simulink model "H175_V3_walk"  (R2025b)
(part 2 of 13)

  ct_L_elbow : nesl_utility/Simulink-PS Converter  PhysicalDomain=network_engine_domain  SubClassName=ps_input  LeftPortType=input  RightPortType=output  PseudoPeriodic=off  Frequencies=[]  NoiseDistribution=none  NoiseParameters=[]  Unit=N*m  AffineConversion=off  FilteringAndDerivatives=provide  SimscapeFilterOrder=1  InputFilterTimeConstant=0.001  UdotUserProvided=0
  ct_L_forearm_twist : nesl_utility/Simulink-PS Converter  PhysicalDomain=network_engine_domain  SubClassName=ps_input  LeftPortType=input  RightPortType=output  PseudoPeriodic=off  Frequencies=[]  NoiseDistribution=none  NoiseParameters=[]  Unit=N*m  AffineConversion=off  FilteringAndDerivatives=provide  SimscapeFilterOrder=1  InputFilterTimeConstant=0.001  UdotUserProvided=0
  ct_L_hip_pitch : nesl_utility/Simulink-PS Converter  PhysicalDomain=network_engine_domain  SubClassName=ps_input  LeftPortType=input  RightPortType=output  PseudoPeriodic=off  Frequencies=[]  NoiseDistribution=none  NoiseParameters=[]  Unit=N*m  AffineConversion=off  FilteringAndDerivatives=provide  SimscapeFilterOrder=1  InputFilterTimeConstant=0.001  UdotUserProvided=0
  ct_L_hip_roll : nesl_utility/Simulink-PS Converter  PhysicalDomain=network_engine_domain  SubClassName=ps_input  LeftPortType=input  RightPortType=output  PseudoPeriodic=off  Frequencies=[]  NoiseDistribution=none  NoiseParameters=[]  Unit=N*m  AffineConversion=off  FilteringAndDerivatives=provide  SimscapeFilterOrder=1  InputFilterTimeConstant=0.001  UdotUserProvided=0
  ct_L_hip_yaw : nesl_utility/Simulink-PS Converter  PhysicalDomain=network_engine_domain  SubClassName=ps_input  LeftPortType=input  RightPortType=output  PseudoPeriodic=off  Frequencies=[]  NoiseDistribution=none  NoiseParameters=[]  Unit=N*m  AffineConversion=off  FilteringAndDerivatives=provide  SimscapeFilterOrder=1  InputFilterTimeConstant=0.001  UdotUserProvided=0
  ct_L_index1 : nesl_utility/Simulink-PS Converter  PhysicalDomain=network_engine_domain  SubClassName=ps_input  LeftPortType=input  RightPortType=output  PseudoPeriodic=off  Frequencies=[]  NoiseDistribution=none  NoiseParameters=[]  Unit=N*m  AffineConversion=off  FilteringAndDerivatives=provide  SimscapeFilterOrder=1  InputFilterTimeConstant=0.001  UdotUserProvided=0
  ct_L_index2 : nesl_utility/Simulink-PS Converter  PhysicalDomain=network_engine_domain  SubClassName=ps_input  LeftPortType=input  RightPortType=output  PseudoPeriodic=off  Frequencies=[]  NoiseDistribution=none  NoiseParameters=[]  Unit=N*m  AffineConversion=off  FilteringAndDerivatives=provide  SimscapeFilterOrder=1  InputFilterTimeConstant=0.001  UdotUserProvided=0
  ct_L_index3 : nesl_utility/Simulink-PS Converter  PhysicalDomain=network_engine_domain  SubClassName=ps_input  LeftPortType=input  RightPortType=output  PseudoPeriodic=off  Frequencies=[]  NoiseDistribution=none  NoiseParameters=[]  Unit=N*m  AffineConversion=off  FilteringAndDerivatives=provide  SimscapeFilterOrder=1  InputFilterTimeConstant=0.001  UdotUserProvided=0
  ct_L_knee : nesl_utility/Simulink-PS Converter  PhysicalDomain=network_engine_domain  SubClassName=ps_input  LeftPortType=input  RightPortType=output  PseudoPeriodic=off  Frequencies=[]  NoiseDistribution=none  NoiseParameters=[]  Unit=N*m  AffineConversion=off  FilteringAndDerivatives=provide  SimscapeFilterOrder=1  InputFilterTimeConstant=0.001  UdotUserProvided=0
  ct_L_little1 : nesl_utility/Simulink-PS Converter  PhysicalDomain=network_engine_domain  SubClassName=ps_input  LeftPortType=input  RightPortType=output  PseudoPeriodic=off  Frequencies=[]  NoiseDistribution=none  NoiseParameters=[]  Unit=N*m  AffineConversion=off  FilteringAndDerivatives=provide  SimscapeFilterOrder=1  InputFilterTimeConstant=0.001  UdotUserProvided=0
  ct_L_little2 : nesl_utility/Simulink-PS Converter  PhysicalDomain=network_engine_domain  SubClassName=ps_input  LeftPortType=input  RightPortType=output  PseudoPeriodic=off  Frequencies=[]  NoiseDistribution=none  NoiseParameters=[]  Unit=N*m  AffineConversion=off  FilteringAndDerivatives=provide  SimscapeFilterOrder=1  InputFilterTimeConstant=0.001  UdotUserProvided=0
  ct_L_little3 : nesl_utility/Simulink-PS Converter  PhysicalDomain=network_engine_domain  SubClassName=ps_input  LeftPortType=input  RightPortType=output  PseudoPeriodic=off  Frequencies=[]  NoiseDistribution=none  NoiseParameters=[]  Unit=N*m  AffineConversion=off  FilteringAndDerivatives=provide  SimscapeFilterOrder=1  InputFilterTimeConstant=0.001  UdotUserProvided=0
  ct_L_middle1 : nesl_utility/Simulink-PS Converter  PhysicalDomain=network_engine_domain  SubClassName=ps_input  LeftPortType=input  RightPortType=output  PseudoPeriodic=off  Frequencies=[]  NoiseDistribution=none  NoiseParameters=[]  Unit=N*m  AffineConversion=off  FilteringAndDerivatives=provide  SimscapeFilterOrder=1  InputFilterTimeConstant=0.001  UdotUserProvided=0
  ct_L_middle2 : nesl_utility/Simulink-PS Converter  PhysicalDomain=network_engine_domain  SubClassName=ps_input  LeftPortType=input  RightPortType=output  PseudoPeriodic=off  Frequencies=[]  NoiseDistribution=none  NoiseParameters=[]  Unit=N*m  AffineConversion=off  FilteringAndDerivatives=provide  SimscapeFilterOrder=1  InputFilterTimeConstant=0.001  UdotUserProvided=0
  ct_L_middle3 : nesl_utility/Simulink-PS Converter  PhysicalDomain=network_engine_domain  SubClassName=ps_input  LeftPortType=input  RightPortType=output  PseudoPeriodic=off  Frequencies=[]  NoiseDistribution=none  NoiseParameters=[]  Unit=N*m  AffineConversion=off  FilteringAndDerivatives=provide  SimscapeFilterOrder=1  InputFilterTimeConstant=0.001  UdotUserProvided=0
  ct_L_ring1 : nesl_utility/Simulink-PS Converter  PhysicalDomain=network_engine_domain  SubClassName=ps_input  LeftPortType=input  RightPortType=output  PseudoPeriodic=off  Frequencies=[]  NoiseDistribution=none  NoiseParameters=[]  Unit=N*m  AffineConversion=off  FilteringAndDerivatives=provide  SimscapeFilterOrder=1  InputFilterTimeConstant=0.001  UdotUserProvided=0
  ct_L_ring2 : nesl_utility/Simulink-PS Converter  PhysicalDomain=network_engine_domain  SubClassName=ps_input  LeftPortType=input  RightPortType=output  PseudoPeriodic=off  Frequencies=[]  NoiseDistribution=none  NoiseParameters=[]  Unit=N*m  AffineConversion=off  FilteringAndDerivatives=provide  SimscapeFilterOrder=1  InputFilterTimeConstant=0.001  UdotUserProvided=0
  ct_L_ring3 : nesl_utility/Simulink-PS Converter  PhysicalDomain=network_engine_domain  SubClassName=ps_input  LeftPortType=input  RightPortType=output  PseudoPeriodic=off  Frequencies=[]  NoiseDistribution=none  NoiseParameters=[]  Unit=N*m  AffineConversion=off  FilteringAndDerivatives=provide  SimscapeFilterOrder=1  InputFilterTimeConstant=0.001  UdotUserProvided=0
  ct_L_scapula : nesl_utility/Simulink-PS Converter  PhysicalDomain=network_engine_domain  SubClassName=ps_input  LeftPortType=input  RightPortType=output  PseudoPeriodic=off  Frequencies=[]  NoiseDistribution=none  NoiseParameters=[]  Unit=N*m  AffineConversion=off  FilteringAndDerivatives=provide  SimscapeFilterOrder=1  InputFilterTimeConstant=0.001  UdotUserProvided=0
  ct_L_shoulder_pitch : nesl_utility/Simulink-PS Converter  PhysicalDomain=network_engine_domain  SubClassName=ps_input  LeftPortType=input  RightPortType=output  PseudoPeriodic=off  Frequencies=[]  NoiseDistribution=none  NoiseParameters=[]  Unit=N*m  AffineConversion=off  FilteringAndDerivatives=provide  SimscapeFilterOrder=1  InputFilterTimeConstant=0.001  UdotUserProvided=0
  ct_L_shoulder_roll : nesl_utility/Simulink-PS Converter  PhysicalDomain=network_engine_domain  SubClassName=ps_input  LeftPortType=input  RightPortType=output  PseudoPeriodic=off  Frequencies=[]  NoiseDistribution=none  NoiseParameters=[]  Unit=N*m  AffineConversion=off  FilteringAndDerivatives=provide  SimscapeFilterOrder=1  InputFilterTimeConstant=0.001  UdotUserProvided=0
  ct_L_shoulder_yaw : nesl_utility/Simulink-PS Converter  PhysicalDomain=network_engine_domain  SubClassName=ps_input  LeftPortType=input  RightPortType=output  PseudoPeriodic=off  Frequencies=[]  NoiseDistribution=none  NoiseParameters=[]  Unit=N*m  AffineConversion=off  FilteringAndDerivatives=provide  SimscapeFilterOrder=1  InputFilterTimeConstant=0.001  UdotUserProvided=0
  ct_L_thumb1 : nesl_utility/Simulink-PS Converter  PhysicalDomain=network_engine_domain  SubClassName=ps_input  LeftPortType=input  RightPortType=output  PseudoPeriodic=off  Frequencies=[]  NoiseDistribution=none  NoiseParameters=[]  Unit=N*m  AffineConversion=off  FilteringAndDerivatives=provide  SimscapeFilterOrder=1  InputFilterTimeConstant=0.001  UdotUserProvided=0
  ct_L_thumb2 : nesl_utility/Simulink-PS Converter  PhysicalDomain=network_engine_domain  SubClassName=ps_input  LeftPortType=input  RightPortType=output  PseudoPeriodic=off  Frequencies=[]  NoiseDistribution=none  NoiseParameters=[]  Unit=N*m  AffineConversion=off  FilteringAndDerivatives=provide  SimscapeFilterOrder=1  InputFilterTimeConstant=0.001  UdotUserProvided=0
  ct_L_thumb3 : nesl_utility/Simulink-PS Converter  PhysicalDomain=network_engine_domain  SubClassName=ps_input  LeftPortType=input  RightPortType=output  PseudoPeriodic=off  Frequencies=[]  NoiseDistribution=none  NoiseParameters=[]  Unit=N*m  AffineConversion=off  FilteringAndDerivatives=provide  SimscapeFilterOrder=1  InputFilterTimeConstant=0.001  UdotUserProvided=0
  ct_L_toe : nesl_utility/Simulink-PS Converter  PhysicalDomain=network_engine_domain  SubClassName=ps_input  LeftPortType=input  RightPortType=output  PseudoPeriodic=off  Frequencies=[]  NoiseDistribution=none  NoiseParameters=[]  Unit=N*m  AffineConversion=off  FilteringAndDerivatives=provide  SimscapeFilterOrder=1  InputFilterTimeConstant=0.001  UdotUserProvided=0
  ct_L_wrist_pitch : nesl_utility/Simulink-PS Converter  PhysicalDomain=network_engine_domain  SubClassName=ps_input  LeftPortType=input  RightPortType=output  PseudoPeriodic=off  Frequencies=[]  NoiseDistribution=none  NoiseParameters=[]  Unit=N*m  AffineConversion=off  FilteringAndDerivatives=provide  SimscapeFilterOrder=1  InputFilterTimeConstant=0.001  UdotUserProvided=0
  ct_L_wrist_roll : nesl_utility/Simulink-PS Converter  PhysicalDomain=network_engine_domain  SubClassName=ps_input  LeftPortType=input  RightPortType=output  PseudoPeriodic=off  Frequencies=[]  NoiseDistribution=none  NoiseParameters=[]  Unit=N*m  AffineConversion=off  FilteringAndDerivatives=provide  SimscapeFilterOrder=1  InputFilterTimeConstant=0.001  UdotUserProvided=0
  ct_L_wrist_yaw : nesl_utility/Simulink-PS Converter  PhysicalDomain=network_engine_domain  SubClassName=ps_input  LeftPortType=input  RightPortType=output  PseudoPeriodic=off  Frequencies=[]  NoiseDistribution=none  NoiseParameters=[]  Unit=N*m  AffineConversion=off  FilteringAndDerivatives=provide  SimscapeFilterOrder=1  InputFilterTimeConstant=0.001  UdotUserProvided=0
  ct_R_ankle_pitch : nesl_utility/Simulink-PS Converter  PhysicalDomain=network_engine_domain  SubClassName=ps_input  LeftPortType=input  RightPortType=output  PseudoPeriodic=off  Frequencies=[]  NoiseDistribution=none  NoiseParameters=[]  Unit=N*m  AffineConversion=off  FilteringAndDerivatives=provide  SimscapeFilterOrder=1  InputFilterTimeConstant=0.001  UdotUserProvided=0
  ct_R_ankle_roll : nesl_utility/Simulink-PS Converter  PhysicalDomain=network_engine_domain  SubClassName=ps_input  LeftPortType=input  RightPortType=output  PseudoPeriodic=off  Frequencies=[]  NoiseDistribution=none  NoiseParameters=[]  Unit=N*m  AffineConversion=off  FilteringAndDerivatives=provide  SimscapeFilterOrder=1  InputFilterTimeConstant=0.001  UdotUserProvided=0
  ct_R_clavicle : nesl_utility/Simulink-PS Converter  PhysicalDomain=network_engine_domain  SubClassName=ps_input  LeftPortType=input  RightPortType=output  PseudoPeriodic=off  Frequencies=[]  NoiseDistribution=none  NoiseParameters=[]  Unit=N*m  AffineConversion=off  FilteringAndDerivatives=provide  SimscapeFilterOrder=1  InputFilterTimeConstant=0.001  UdotUserProvided=0
  ct_R_elbow : nesl_utility/Simulink-PS Converter  PhysicalDomain=network_engine_domain  SubClassName=ps_input  LeftPortType=input  RightPortType=output  PseudoPeriodic=off  Frequencies=[]  NoiseDistribution=none  NoiseParameters=[]  Unit=N*m  AffineConversion=off  FilteringAndDerivatives=provide  SimscapeFilterOrder=1  InputFilterTimeConstant=0.001  UdotUserProvided=0
  ct_R_forearm_twist : nesl_utility/Simulink-PS Converter  PhysicalDomain=network_engine_domain  SubClassName=ps_input  LeftPortType=input  RightPortType=output  PseudoPeriodic=off  Frequencies=[]  NoiseDistribution=none  NoiseParameters=[]  Unit=N*m  AffineConversion=off  FilteringAndDerivatives=provide  SimscapeFilterOrder=1  InputFilterTimeConstant=0.001  UdotUserProvided=0
  ct_R_hip_pitch : nesl_utility/Simulink-PS Converter  PhysicalDomain=network_engine_domain  SubClassName=ps_input  LeftPortType=input  RightPortType=output  PseudoPeriodic=off  Frequencies=[]  NoiseDistribution=none  NoiseParameters=[]  Unit=N*m  AffineConversion=off  FilteringAndDerivatives=provide  SimscapeFilterOrder=1  InputFilterTimeConstant=0.001  UdotUserProvided=0
  ct_R_hip_roll : nesl_utility/Simulink-PS Converter  PhysicalDomain=network_engine_domain  SubClassName=ps_input  LeftPortType=input  RightPortType=output  PseudoPeriodic=off  Frequencies=[]  NoiseDistribution=none  NoiseParameters=[]  Unit=N*m  AffineConversion=off  FilteringAndDerivatives=provide  SimscapeFilterOrder=1  InputFilterTimeConstant=0.001  UdotUserProvided=0
  ct_R_hip_yaw : nesl_utility/Simulink-PS Converter  PhysicalDomain=network_engine_domain  SubClassName=ps_input  LeftPortType=input  RightPortType=output  PseudoPeriodic=off  Frequencies=[]  NoiseDistribution=none  NoiseParameters=[]  Unit=N*m  AffineConversion=off  FilteringAndDerivatives=provide  SimscapeFilterOrder=1  InputFilterTimeConstant=0.001  UdotUserProvided=0
  ct_R_index1 : nesl_utility/Simulink-PS Converter  PhysicalDomain=network_engine_domain  SubClassName=ps_input  LeftPortType=input  RightPortType=output  PseudoPeriodic=off  Frequencies=[]  NoiseDistribution=none  NoiseParameters=[]  Unit=N*m  AffineConversion=off  FilteringAndDerivatives=provide  SimscapeFilterOrder=1  InputFilterTimeConstant=0.001  UdotUserProvided=0
  ct_R_index2 : nesl_utility/Simulink-PS Converter  PhysicalDomain=network_engine_domain  SubClassName=ps_input  LeftPortType=input  RightPortType=output  PseudoPeriodic=off  Frequencies=[]  NoiseDistribution=none  NoiseParameters=[]  Unit=N*m  AffineConversion=off  FilteringAndDerivatives=provide  SimscapeFilterOrder=1  InputFilterTimeConstant=0.001  UdotUserProvided=0
  ct_R_index3 : nesl_utility/Simulink-PS Converter  PhysicalDomain=network_engine_domain  SubClassName=ps_input  LeftPortType=input  RightPortType=output  PseudoPeriodic=off  Frequencies=[]  NoiseDistribution=none  NoiseParameters=[]  Unit=N*m  AffineConversion=off  FilteringAndDerivatives=provide  SimscapeFilterOrder=1  InputFilterTimeConstant=0.001  UdotUserProvided=0
  ct_R_knee : nesl_utility/Simulink-PS Converter  PhysicalDomain=network_engine_domain  SubClassName=ps_input  LeftPortType=input  RightPortType=output  PseudoPeriodic=off  Frequencies=[]  NoiseDistribution=none  NoiseParameters=[]  Unit=N*m  AffineConversion=off  FilteringAndDerivatives=provide  SimscapeFilterOrder=1  InputFilterTimeConstant=0.001  UdotUserProvided=0
  ct_R_little1 : nesl_utility/Simulink-PS Converter  PhysicalDomain=network_engine_domain  SubClassName=ps_input  LeftPortType=input  RightPortType=output  PseudoPeriodic=off  Frequencies=[]  NoiseDistribution=none  NoiseParameters=[]  Unit=N*m  AffineConversion=off  FilteringAndDerivatives=provide  SimscapeFilterOrder=1  InputFilterTimeConstant=0.001  UdotUserProvided=0
  ct_R_little2 : nesl_utility/Simulink-PS Converter  PhysicalDomain=network_engine_domain  SubClassName=ps_input  LeftPortType=input  RightPortType=output  PseudoPeriodic=off  Frequencies=[]  NoiseDistribution=none  NoiseParameters=[]  Unit=N*m  AffineConversion=off  FilteringAndDerivatives=provide  SimscapeFilterOrder=1  InputFilterTimeConstant=0.001  UdotUserProvided=0
  ct_R_little3 : nesl_utility/Simulink-PS Converter  PhysicalDomain=network_engine_domain  SubClassName=ps_input  LeftPortType=input  RightPortType=output  PseudoPeriodic=off  Frequencies=[]  NoiseDistribution=none  NoiseParameters=[]  Unit=N*m  AffineConversion=off  FilteringAndDerivatives=provide  SimscapeFilterOrder=1  InputFilterTimeConstant=0.001  UdotUserProvided=0
  ct_R_middle1 : nesl_utility/Simulink-PS Converter  PhysicalDomain=network_engine_domain  SubClassName=ps_input  LeftPortType=input  RightPortType=output  PseudoPeriodic=off  Frequencies=[]  NoiseDistribution=none  NoiseParameters=[]  Unit=N*m  AffineConversion=off  FilteringAndDerivatives=provide  SimscapeFilterOrder=1  InputFilterTimeConstant=0.001  UdotUserProvided=0
  ct_R_middle2 : nesl_utility/Simulink-PS Converter  PhysicalDomain=network_engine_domain  SubClassName=ps_input  LeftPortType=input  RightPortType=output  PseudoPeriodic=off  Frequencies=[]  NoiseDistribution=none  NoiseParameters=[]  Unit=N*m  AffineConversion=off  FilteringAndDerivatives=provide  SimscapeFilterOrder=1  InputFilterTimeConstant=0.001  UdotUserProvided=0
  ct_R_middle3 : nesl_utility/Simulink-PS Converter  PhysicalDomain=network_engine_domain  SubClassName=ps_input  LeftPortType=input  RightPortType=output  PseudoPeriodic=off  Frequencies=[]  NoiseDistribution=none  NoiseParameters=[]  Unit=N*m  AffineConversion=off  FilteringAndDerivatives=provide  SimscapeFilterOrder=1  InputFilterTimeConstant=0.001  UdotUserProvided=0
  ct_R_ring1 : nesl_utility/Simulink-PS Converter  PhysicalDomain=network_engine_domain  SubClassName=ps_input  LeftPortType=input  RightPortType=output  PseudoPeriodic=off  Frequencies=[]  NoiseDistribution=none  NoiseParameters=[]  Unit=N*m  AffineConversion=off  FilteringAndDerivatives=provide  SimscapeFilterOrder=1  InputFilterTimeConstant=0.001  UdotUserProvided=0
  ct_R_ring2 : nesl_utility/Simulink-PS Converter  PhysicalDomain=network_engine_domain  SubClassName=ps_input  LeftPortType=input  RightPortType=output  PseudoPeriodic=off  Frequencies=[]  NoiseDistribution=none  NoiseParameters=[]  Unit=N*m  AffineConversion=off  FilteringAndDerivatives=provide  SimscapeFilterOrder=1  InputFilterTimeConstant=0.001  UdotUserProvided=0
  ct_R_ring3 : nesl_utility/Simulink-PS Converter  PhysicalDomain=network_engine_domain  SubClassName=ps_input  LeftPortType=input  RightPortType=output  PseudoPeriodic=off  Frequencies=[]  NoiseDistribution=none  NoiseParameters=[]  Unit=N*m  AffineConversion=off  FilteringAndDerivatives=provide  SimscapeFilterOrder=1  InputFilterTimeConstant=0.001  UdotUserProvided=0
  ct_R_scapula : nesl_utility/Simulink-PS Converter  PhysicalDomain=network_engine_domain  SubClassName=ps_input  LeftPortType=input  RightPortType=output  PseudoPeriodic=off  Frequencies=[]  NoiseDistribution=none  NoiseParameters=[]  Unit=N*m  AffineConversion=off  FilteringAndDerivatives=provide  SimscapeFilterOrder=1  InputFilterTimeConstant=0.001  UdotUserProvided=0
  ct_R_shoulder_pitch : nesl_utility/Simulink-PS Converter  PhysicalDomain=network_engine_domain  SubClassName=ps_input  LeftPortType=input  RightPortType=output  PseudoPeriodic=off  Frequencies=[]  NoiseDistribution=none  NoiseParameters=[]  Unit=N*m  AffineConversion=off  FilteringAndDerivatives=provide  SimscapeFilterOrder=1  InputFilterTimeConstant=0.001  UdotUserProvided=0
  ct_R_shoulder_roll : nesl_utility/Simulink-PS Converter  PhysicalDomain=network_engine_domain  SubClassName=ps_input  LeftPortType=input  RightPortType=output  PseudoPeriodic=off  Frequencies=[]  NoiseDistribution=none  NoiseParameters=[]  Unit=N*m  AffineConversion=off  FilteringAndDerivatives=provide  SimscapeFilterOrder=1  InputFilterTimeConstant=0.001  UdotUserProvided=0
  ct_R_shoulder_yaw : nesl_utility/Simulink-PS Converter  PhysicalDomain=network_engine_domain  SubClassName=ps_input  LeftPortType=input  RightPortType=output  PseudoPeriodic=off  Frequencies=[]  NoiseDistribution=none  NoiseParameters=[]  Unit=N*m  AffineConversion=off  FilteringAndDerivatives=provide  SimscapeFilterOrder=1  InputFilterTimeConstant=0.001  UdotUserProvided=0
  ct_R_thumb1 : nesl_utility/Simulink-PS Converter  PhysicalDomain=network_engine_domain  SubClassName=ps_input  LeftPortType=input  RightPortType=output  PseudoPeriodic=off  Frequencies=[]  NoiseDistribution=none  NoiseParameters=[]  Unit=N*m  AffineConversion=off  FilteringAndDerivatives=provide  SimscapeFilterOrder=1  InputFilterTimeConstant=0.001  UdotUserProvided=0
  ct_R_thumb2 : nesl_utility/Simulink-PS Converter  PhysicalDomain=network_engine_domain  SubClassName=ps_input  LeftPortType=input  RightPortType=output  PseudoPeriodic=off  Frequencies=[]  NoiseDistribution=none  NoiseParameters=[]  Unit=N*m  AffineConversion=off  FilteringAndDerivatives=provide  SimscapeFilterOrder=1  InputFilterTimeConstant=0.001  UdotUserProvided=0
  ct_R_thumb3 : nesl_utility/Simulink-PS Converter  PhysicalDomain=network_engine_domain  SubClassName=ps_input  LeftPortType=input  RightPortType=output  PseudoPeriodic=off  Frequencies=[]  NoiseDistribution=none  NoiseParameters=[]  Unit=N*m  AffineConversion=off  FilteringAndDerivatives=provide  SimscapeFilterOrder=1  InputFilterTimeConstant=0.001  UdotUserProvided=0
  ct_R_toe : nesl_utility/Simulink-PS Converter  PhysicalDomain=network_engine_domain  SubClassName=ps_input  LeftPortType=input  RightPortType=output  PseudoPeriodic=off  Frequencies=[]  NoiseDistribution=none  NoiseParameters=[]  Unit=N*m  AffineConversion=off  FilteringAndDerivatives=provide  SimscapeFilterOrder=1  InputFilterTimeConstant=0.001  UdotUserProvided=0
  ct_R_wrist_pitch : nesl_utility/Simulink-PS Converter  PhysicalDomain=network_engine_domain  SubClassName=ps_input  LeftPortType=input  RightPortType=output  PseudoPeriodic=off  Frequencies=[]  NoiseDistribution=none  NoiseParameters=[]  Unit=N*m  AffineConversion=off  FilteringAndDerivatives=provide  SimscapeFilterOrder=1  InputFilterTimeConstant=0.001  UdotUserProvided=0
  ct_R_wrist_roll : nesl_utility/Simulink-PS Converter  PhysicalDomain=network_engine_domain  SubClassName=ps_input  LeftPortType=input  RightPortType=output  PseudoPeriodic=off  Frequencies=[]  NoiseDistribution=none  NoiseParameters=[]  Unit=N*m  AffineConversion=off  FilteringAndDerivatives=provide  SimscapeFilterOrder=1  InputFilterTimeConstant=0.001  UdotUserProvided=0
  ct_R_wrist_yaw : nesl_utility/Simulink-PS Converter  PhysicalDomain=network_engine_domain  SubClassName=ps_input  LeftPortType=input  RightPortType=output  PseudoPeriodic=off  Frequencies=[]  NoiseDistribution=none  NoiseParameters=[]  Unit=N*m  AffineConversion=off  FilteringAndDerivatives=provide  SimscapeFilterOrder=1  InputFilterTimeConstant=0.001  UdotUserProvided=0
  ct_neck_pitch : nesl_utility/Simulink-PS Converter  PhysicalDomain=network_engine_domain  SubClassName=ps_input  LeftPortType=input  RightPortType=output  PseudoPeriodic=off  Frequencies=[]  NoiseDistribution=none  NoiseParameters=[]  Unit=N*m  AffineConversion=off  FilteringAndDerivatives=provide  SimscapeFilterOrder=1  InputFilterTimeConstant=0.001  UdotUserProvided=0
  ct_neck_roll : nesl_utility/Simulink-PS Converter  PhysicalDomain=network_engine_domain  SubClassName=ps_input  LeftPortType=input  RightPortType=output  PseudoPeriodic=off  Frequencies=[]  NoiseDistribution=none  NoiseParameters=[]  Unit=N*m  AffineConversion=off  FilteringAndDerivatives=provide  SimscapeFilterOrder=1  InputFilterTimeConstant=0.001  UdotUserProvided=0
  ct_neck_yaw : nesl_utility/Simulink-PS Converter  PhysicalDomain=network_engine_domain  SubClassName=ps_input  LeftPortType=input  RightPortType=output  PseudoPeriodic=off  Frequencies=[]  NoiseDistribution=none  NoiseParameters=[]  Unit=N*m  AffineConversion=off  FilteringAndDerivatives=provide  SimscapeFilterOrder=1  InputFilterTimeConstant=0.001  UdotUserProvided=0
  ct_rot_L{1..4} (4 alike) : sm_lib/Frames and Transforms/Rigid Transform  RotationMethod=ArbitraryAxis  FollAlignAxisA=+X  BaseAlignAxisA=+Y  FollAlignAxisB=+Y  BaseAlignAxisB=+Z  RotationStandardAxis=+Z  RotationAngle=-1.5708  RotationAngleUnits=rad  RotationArbitraryAxis=[-0, 1, 0]  RotationSequenceAxes=FollowerAxes  RotationSequence=XYX  RotationSequenceAngles=[0 0 0]  RotationSequenceAnglesUnits=deg  RotationMatrix=[1 0 0;0 1 0;0 0 1]  Quaternion=[1 0 0 0]  TranslationMethod=None  TranslationCartesianOffset=[0 0 0]  TranslationCartesianOffsetUnits=m  TranslationStandardAxis=+Z  TranslationStandardOffset=0  TranslationStandardOffsetUnits=m  TranslationROffset=0  TranslationROffsetUnits=m  TranslationThetaOffset=0  TranslationThetaOffsetUnits=deg  TranslationZOffset=0  TranslationZOffsetUnits=m
  ct_rot_R{1..4} (4 alike) : sm_lib/Frames and Transforms/Rigid Transform  RotationMethod=ArbitraryAxis  FollAlignAxisA=+X  BaseAlignAxisA=+Y  FollAlignAxisB=+Y  BaseAlignAxisB=+Z  RotationStandardAxis=+Z  RotationAngle=-1.5708  RotationAngleUnits=rad  RotationArbitraryAxis=[-0, 1, 0]  RotationSequenceAxes=FollowerAxes  RotationSequence=XYX  RotationSequenceAngles=[0 0 0]  RotationSequenceAnglesUnits=deg  RotationMatrix=[1 0 0;0 1 0;0 0 1]  Quaternion=[1 0 0 0]  TranslationMethod=None  TranslationCartesianOffset=[0 0 0]  TranslationCartesianOffsetUnits=m  TranslationStandardAxis=+Z  TranslationStandardOffset=0  TranslationStandardOffsetUnits=m  TranslationROffset=0  TranslationROffsetUnits=m  TranslationThetaOffset=0  TranslationThetaOffsetUnits=deg  TranslationZOffset=0  TranslationZOffsetUnits=m
  ct_sph_L{1..4} (4 alike) : sm_lib/Body Elements/Spherical Solid  SphereRadius=0.006  SphereRadiusUnits=m  ExportEntireGeometry=on  InertiaType=CalculateFromGeometry  BasedOnType=Density  Density=1000  DensityUnits=kg/m^3  Mass=1  MassUnits=kg  CenterOfMass=[0 0 0]  CenterOfMassUnits=m  MomentsOfInertia=[1 1 1]  MomentsOfInertiaUnits=kg*m^2  ProductsOfInertia=[0 0 0]  ProductsOfInertiaUnits=kg*m^2  GraphicType=FromGeometry  MarkerShape=Sphere  MarkerSize=10  GraphicVisPropType=SimpleVisualProperties  GraphicDiffuseColor=[0.9 0.2 0.2]  GraphicOpacity=1  GraphicSpecularColor=[0.5 0.5 0.5 1.0]  GraphicAmbientColor=[0.15 0.15 0.15 1.0]  GraphicEmissiveColor=[0.0 0.0 0.0 1.0]  GraphicShininess=75  DoExposeReferenceFrame=on  SerializedFrames=<Frames/>
  ct_sph_R{1..4} (4 alike) : sm_lib/Body Elements/Spherical Solid  SphereRadius=0.006  SphereRadiusUnits=m  ExportEntireGeometry=on  InertiaType=CalculateFromGeometry  BasedOnType=Density  Density=1000  DensityUnits=kg/m^3  Mass=1  MassUnits=kg  CenterOfMass=[0 0 0]  CenterOfMassUnits=m  MomentsOfInertia=[1 1 1]  MomentsOfInertiaUnits=kg*m^2  ProductsOfInertia=[0 0 0]  ProductsOfInertiaUnits=kg*m^2  GraphicType=FromGeometry  MarkerShape=Sphere  MarkerSize=10  GraphicVisPropType=SimpleVisualProperties  GraphicDiffuseColor=[0.9 0.2 0.2]  GraphicOpacity=1  GraphicSpecularColor=[0.5 0.5 0.5 1.0]  GraphicAmbientColor=[0.15 0.15 0.15 1.0]  GraphicEmissiveColor=[0.0 0.0 0.0 1.0]  GraphicShininess=75  DoExposeReferenceFrame=on  SerializedFrames=<Frames/>
  ct_tf_L1 : sm_lib/Frames and Transforms/Rigid Transform  RotationMethod=None  FollAlignAxisA=+X  BaseAlignAxisA=+Y  FollAlignAxisB=+Y  BaseAlignAxisB=+Z  RotationStandardAxis=+Z  RotationAngle=0  RotationAngleUnits=deg  RotationArbitraryAxis=[0 0 1]  RotationSequenceAxes=FollowerAxes  RotationSequence=XYX  RotationSequenceAngles=[0 0 0]  RotationSequenceAnglesUnits=deg  RotationMatrix=[1 0 0;0 1 0;0 0 1]  Quaternion=[1 0 0 0]  TranslationMethod=Cartesian  TranslationCartesianOffset=[-0.07 0.05 -0.074]  TranslationCartesianOffsetUnits=m  TranslationStandardAxis=+Z  TranslationStandardOffset=0  TranslationStandardOffsetUnits=m  TranslationROffset=0  TranslationROffsetUnits=m  TranslationThetaOffset=0  TranslationThetaOffsetUnits=deg  TranslationZOffset=0  TranslationZOffsetUnits=m
  ct_tf_L2 : sm_lib/Frames and Transforms/Rigid Transform  RotationMethod=None  FollAlignAxisA=+X  BaseAlignAxisA=+Y  FollAlignAxisB=+Y  BaseAlignAxisB=+Z  RotationStandardAxis=+Z  RotationAngle=0  RotationAngleUnits=deg  RotationArbitraryAxis=[0 0 1]  RotationSequenceAxes=FollowerAxes  RotationSequence=XYX  RotationSequenceAngles=[0 0 0]  RotationSequenceAnglesUnits=deg  RotationMatrix=[1 0 0;0 1 0;0 0 1]  Quaternion=[1 0 0 0]  TranslationMethod=Cartesian  TranslationCartesianOffset=[-0.07 -0.05 -0.074]  TranslationCartesianOffsetUnits=m  TranslationStandardAxis=+Z  TranslationStandardOffset=0  TranslationStandardOffsetUnits=m  TranslationROffset=0  TranslationROffsetUnits=m  TranslationThetaOffset=0  TranslationThetaOffsetUnits=deg  TranslationZOffset=0  TranslationZOffsetUnits=m
  ct_tf_L3 : sm_lib/Frames and Transforms/Rigid Transform  RotationMethod=None  FollAlignAxisA=+X  BaseAlignAxisA=+Y  FollAlignAxisB=+Y  BaseAlignAxisB=+Z  RotationStandardAxis=+Z  RotationAngle=0  RotationAngleUnits=deg  RotationArbitraryAxis=[0 0 1]  RotationSequenceAxes=FollowerAxes  RotationSequence=XYX  RotationSequenceAngles=[0 0 0]  RotationSequenceAnglesUnits=deg  RotationMatrix=[1 0 0;0 1 0;0 0 1]  Quaternion=[1 0 0 0]  TranslationMethod=Cartesian  TranslationCartesianOffset=[0.11 0.05 -0.074]  TranslationCartesianOffsetUnits=m  TranslationStandardAxis=+Z  TranslationStandardOffset=0  TranslationStandardOffsetUnits=m  TranslationROffset=0  TranslationROffsetUnits=m  TranslationThetaOffset=0  TranslationThetaOffsetUnits=deg  TranslationZOffset=0  TranslationZOffsetUnits=m
  ct_tf_L4 : sm_lib/Frames and Transforms/Rigid Transform  RotationMethod=None  FollAlignAxisA=+X  BaseAlignAxisA=+Y  FollAlignAxisB=+Y  BaseAlignAxisB=+Z  RotationStandardAxis=+Z  RotationAngle=0  RotationAngleUnits=deg  RotationArbitraryAxis=[0 0 1]  RotationSequenceAxes=FollowerAxes  RotationSequence=XYX  RotationSequenceAngles=[0 0 0]  RotationSequenceAnglesUnits=deg  RotationMatrix=[1 0 0;0 1 0;0 0 1]  Quaternion=[1 0 0 0]  TranslationMethod=Cartesian  TranslationCartesianOffset=[0.11 -0.05 -0.074]  TranslationCartesianOffsetUnits=m  TranslationStandardAxis=+Z  TranslationStandardOffset=0  TranslationStandardOffsetUnits=m  TranslationROffset=0  TranslationROffsetUnits=m  TranslationThetaOffset=0  TranslationThetaOffsetUnits=deg  TranslationZOffset=0  TranslationZOffsetUnits=m
  ct_tf_R1 : sm_lib/Frames and Transforms/Rigid Transform  RotationMethod=None  FollAlignAxisA=+X  BaseAlignAxisA=+Y  FollAlignAxisB=+Y  BaseAlignAxisB=+Z  RotationStandardAxis=+Z  RotationAngle=0  RotationAngleUnits=deg  RotationArbitraryAxis=[0 0 1]  RotationSequenceAxes=FollowerAxes  RotationSequence=XYX  RotationSequenceAngles=[0 0 0]  RotationSequenceAnglesUnits=deg  RotationMatrix=[1 0 0;0 1 0;0 0 1]  Quaternion=[1 0 0 0]  TranslationMethod=Cartesian  TranslationCartesianOffset=[-0.07 0.05 -0.074]  TranslationCartesianOffsetUnits=m  TranslationStandardAxis=+Z  TranslationStandardOffset=0  TranslationStandardOffsetUnits=m  TranslationROffset=0  TranslationROffsetUnits=m  TranslationThetaOffset=0  TranslationThetaOffsetUnits=deg  TranslationZOffset=0  TranslationZOffsetUnits=m
  ct_tf_R2 : sm_lib/Frames and Transforms/Rigid Transform  RotationMethod=None  FollAlignAxisA=+X  BaseAlignAxisA=+Y  FollAlignAxisB=+Y  BaseAlignAxisB=+Z  RotationStandardAxis=+Z  RotationAngle=0  RotationAngleUnits=deg  RotationArbitraryAxis=[0 0 1]  RotationSequenceAxes=FollowerAxes  RotationSequence=XYX  RotationSequenceAngles=[0 0 0]  RotationSequenceAnglesUnits=deg  RotationMatrix=[1 0 0;0 1 0;0 0 1]  Quaternion=[1 0 0 0]  TranslationMethod=Cartesian  TranslationCartesianOffset=[-0.07 -0.05 -0.074]  TranslationCartesianOffsetUnits=m  TranslationStandardAxis=+Z  TranslationStandardOffset=0  TranslationStandardOffsetUnits=m  TranslationROffset=0  TranslationROffsetUnits=m  TranslationThetaOffset=0  TranslationThetaOffsetUnits=deg  TranslationZOffset=0  TranslationZOffsetUnits=m
  ct_tf_R3 : sm_lib/Frames and Transforms/Rigid Transform  RotationMethod=None  FollAlignAxisA=+X  BaseAlignAxisA=+Y  FollAlignAxisB=+Y  BaseAlignAxisB=+Z  RotationStandardAxis=+Z  RotationAngle=0  RotationAngleUnits=deg  RotationArbitraryAxis=[0 0 1]  RotationSequenceAxes=FollowerAxes  RotationSequence=XYX  RotationSequenceAngles=[0 0 0]  RotationSequenceAnglesUnits=deg  RotationMatrix=[1 0 0;0 1 0;0 0 1]  Quaternion=[1 0 0 0]  TranslationMethod=Cartesian  TranslationCartesianOffset=[0.11 0.05 -0.074]  TranslationCartesianOffsetUnits=m  TranslationStandardAxis=+Z  TranslationStandardOffset=0  TranslationStandardOffsetUnits=m  TranslationROffset=0  TranslationROffsetUnits=m  TranslationThetaOffset=0  TranslationThetaOffsetUnits=deg  TranslationZOffset=0  TranslationZOffsetUnits=m
  ct_tf_R4 : sm_lib/Frames and Transforms/Rigid Transform  RotationMethod=None  FollAlignAxisA=+X  BaseAlignAxisA=+Y  FollAlignAxisB=+Y  BaseAlignAxisB=+Z  RotationStandardAxis=+Z  RotationAngle=0  RotationAngleUnits=deg  RotationArbitraryAxis=[0 0 1]  RotationSequenceAxes=FollowerAxes  RotationSequence=XYX  RotationSequenceAngles=[0 0 0]  RotationSequenceAnglesUnits=deg  RotationMatrix=[1 0 0;0 1 0;0 0 1]  Quaternion=[1 0 0 0]  TranslationMethod=Cartesian  TranslationCartesianOffset=[0.11 -0.05 -0.074]  TranslationCartesianOffsetUnits=m  TranslationStandardAxis=+Z  TranslationStandardOffset=0  TranslationStandardOffsetUnits=m  TranslationROffset=0  TranslationROffsetUnits=m  TranslationThetaOffset=0  TranslationThetaOffsetUnits=deg  TranslationZOffset=0  TranslationZOffsetUnits=m
  ct_waist_pitch : nesl_utility/Simulink-PS Converter  PhysicalDomain=network_engine_domain  SubClassName=ps_input  LeftPortType=input  RightPortType=output  PseudoPeriodic=off  Frequencies=[]  NoiseDistribution=none  NoiseParameters=[]  Unit=N*m  AffineConversion=off  FilteringAndDerivatives=provide  SimscapeFilterOrder=1  InputFilterTimeConstant=0.001  UdotUserProvided=0
  ct_waist_roll : nesl_utility/Simulink-PS Converter  PhysicalDomain=network_engine_domain  SubClassName=ps_input  LeftPortType=input  RightPortType=output  PseudoPeriodic=off  Frequencies=[]  NoiseDistribution=none  NoiseParameters=[]  Unit=N*m  AffineConversion=off  FilteringAndDerivatives=provide  SimscapeFilterOrder=1  InputFilterTimeConstant=0.001  UdotUserProvided=0
  ct_waist_yaw : nesl_utility/Simulink-PS Converter  PhysicalDomain=network_engine_domain  SubClassName=ps_input  LeftPortType=input  RightPortType=output  PseudoPeriodic=off  Frequencies=[]  NoiseDistribution=none  NoiseParameters=[]  Unit=N*m  AffineConversion=off  FilteringAndDerivatives=provide  SimscapeFilterOrder=1  InputFilterTimeConstant=0.001  UdotUserProvided=0
  cw_L_ankle_pitch : nesl_utility/PS-Simulink Converter  PhysicalDomain=network_engine_domain  SubClassName=ps_output  LeftPortType=input  RightPortType=output  PseudoPeriodic=off  Frequencies=[]  VectorFormat=inherit  Unit=rad/s  AffineConversion=off
  cw_L_ankle_roll : nesl_utility/PS-Simulink Converter  PhysicalDomain=network_engine_domain  SubClassName=ps_output  LeftPortType=input  RightPortType=output  PseudoPeriodic=off  Frequencies=[]  VectorFormat=inherit  Unit=rad/s  AffineConversion=off
  cw_L_clavicle : nesl_utility/PS-Simulink Converter  PhysicalDomain=network_engine_domain  SubClassName=ps_output  LeftPortType=input  RightPortType=output  PseudoPeriodic=off  Frequencies=[]  VectorFormat=inherit  Unit=rad/s  AffineConversion=off
  cw_L_elbow : nesl_utility/PS-Simulink Converter  PhysicalDomain=network_engine_domain  SubClassName=ps_output  LeftPortType=input  RightPortType=output  PseudoPeriodic=off  Frequencies=[]  VectorFormat=inherit  Unit=rad/s  AffineConversion=off
  cw_L_forearm_twist : nesl_utility/PS-Simulink Converter  PhysicalDomain=network_engine_domain  SubClassName=ps_output  LeftPortType=input  RightPortType=output  PseudoPeriodic=off  Frequencies=[]  VectorFormat=inherit  Unit=rad/s  AffineConversion=off
  cw_L_hip_pitch : nesl_utility/PS-Simulink Converter  PhysicalDomain=network_engine_domain  SubClassName=ps_output  LeftPortType=input  RightPortType=output  PseudoPeriodic=off  Frequencies=[]  VectorFormat=inherit  Unit=rad/s  AffineConversion=off
  cw_L_hip_roll : nesl_utility/PS-Simulink Converter  PhysicalDomain=network_engine_domain  SubClassName=ps_output  LeftPortType=input  RightPortType=output  PseudoPeriodic=off  Frequencies=[]  VectorFormat=inherit  Unit=rad/s  AffineConversion=off
  cw_L_hip_yaw : nesl_utility/PS-Simulink Converter  PhysicalDomain=network_engine_domain  SubClassName=ps_output  LeftPortType=input  RightPortType=output  PseudoPeriodic=off  Frequencies=[]  VectorFormat=inherit  Unit=rad/s  AffineConversion=off
  cw_L_index1 : nesl_utility/PS-Simulink Converter  PhysicalDomain=network_engine_domain  SubClassName=ps_output  LeftPortType=input  RightPortType=output  PseudoPeriodic=off  Frequencies=[]  VectorFormat=inherit  Unit=rad/s  AffineConversion=off
  cw_L_index2 : nesl_utility/PS-Simulink Converter  PhysicalDomain=network_engine_domain  SubClassName=ps_output  LeftPortType=input  RightPortType=output  PseudoPeriodic=off  Frequencies=[]  VectorFormat=inherit  Unit=rad/s  AffineConversion=off
  cw_L_index3 : nesl_utility/PS-Simulink Converter  PhysicalDomain=network_engine_domain  SubClassName=ps_output  LeftPortType=input  RightPortType=output  PseudoPeriodic=off  Frequencies=[]  VectorFormat=inherit  Unit=rad/s  AffineConversion=off
  cw_L_knee : nesl_utility/PS-Simulink Converter  PhysicalDomain=network_engine_domain  SubClassName=ps_output  LeftPortType=input  RightPortType=output  PseudoPeriodic=off  Frequencies=[]  VectorFormat=inherit  Unit=rad/s  AffineConversion=off
  cw_L_little1 : nesl_utility/PS-Simulink Converter  PhysicalDomain=network_engine_domain  SubClassName=ps_output  LeftPortType=input  RightPortType=output  PseudoPeriodic=off  Frequencies=[]  VectorFormat=inherit  Unit=rad/s  AffineConversion=off
  cw_L_little2 : nesl_utility/PS-Simulink Converter  PhysicalDomain=network_engine_domain  SubClassName=ps_output  LeftPortType=input  RightPortType=output  PseudoPeriodic=off  Frequencies=[]  VectorFormat=inherit  Unit=rad/s  AffineConversion=off
  cw_L_little3 : nesl_utility/PS-Simulink Converter  PhysicalDomain=network_engine_domain  SubClassName=ps_output  LeftPortType=input  RightPortType=output  PseudoPeriodic=off  Frequencies=[]  VectorFormat=inherit  Unit=rad/s  AffineConversion=off
  cw_L_middle1 : nesl_utility/PS-Simulink Converter  PhysicalDomain=network_engine_domain  SubClassName=ps_output  LeftPortType=input  RightPortType=output  PseudoPeriodic=off  Frequencies=[]  VectorFormat=inherit  Unit=rad/s  AffineConversion=off
  cw_L_middle2 : nesl_utility/PS-Simulink Converter  PhysicalDomain=network_engine_domain  SubClassName=ps_output  LeftPortType=input  RightPortType=output  PseudoPeriodic=off  Frequencies=[]  VectorFormat=inherit  Unit=rad/s  AffineConversion=off
  cw_L_middle3 : nesl_utility/PS-Simulink Converter  PhysicalDomain=network_engine_domain  SubClassName=ps_output  LeftPortType=input  RightPortType=output  PseudoPeriodic=off  Frequencies=[]  VectorFormat=inherit  Unit=rad/s  AffineConversion=off
  cw_L_ring1 : nesl_utility/PS-Simulink Converter  PhysicalDomain=network_engine_domain  SubClassName=ps_output  LeftPortType=input  RightPortType=output  PseudoPeriodic=off  Frequencies=[]  VectorFormat=inherit  Unit=rad/s  AffineConversion=off
  cw_L_ring2 : nesl_utility/PS-Simulink Converter  PhysicalDomain=network_engine_domain  SubClassName=ps_output  LeftPortType=input  RightPortType=output  PseudoPeriodic=off  Frequencies=[]  VectorFormat=inherit  Unit=rad/s  AffineConversion=off
  cw_L_ring3 : nesl_utility/PS-Simulink Converter  PhysicalDomain=network_engine_domain  SubClassName=ps_output  LeftPortType=input  RightPortType=output  PseudoPeriodic=off  Frequencies=[]  VectorFormat=inherit  Unit=rad/s  AffineConversion=off
  cw_L_scapula : nesl_utility/PS-Simulink Converter  PhysicalDomain=network_engine_domain  SubClassName=ps_output  LeftPortType=input  RightPortType=output  PseudoPeriodic=off  Frequencies=[]  VectorFormat=inherit  Unit=rad/s  AffineConversion=off
  cw_L_shoulder_pitch : nesl_utility/PS-Simulink Converter  PhysicalDomain=network_engine_domain  SubClassName=ps_output  LeftPortType=input  RightPortType=output  PseudoPeriodic=off  Frequencies=[]  VectorFormat=inherit  Unit=rad/s  AffineConversion=off
  cw_L_shoulder_roll : nesl_utility/PS-Simulink Converter  PhysicalDomain=network_engine_domain  SubClassName=ps_output  LeftPortType=input  RightPortType=output  PseudoPeriodic=off  Frequencies=[]  VectorFormat=inherit  Unit=rad/s  AffineConversion=off
  cw_L_shoulder_yaw : nesl_utility/PS-Simulink Converter  PhysicalDomain=network_engine_domain  SubClassName=ps_output  LeftPortType=input  RightPortType=output  PseudoPeriodic=off  Frequencies=[]  VectorFormat=inherit  Unit=rad/s  AffineConversion=off
  cw_L_thumb1 : nesl_utility/PS-Simulink Converter  PhysicalDomain=network_engine_domain  SubClassName=ps_output  LeftPortType=input  RightPortType=output  PseudoPeriodic=off  Frequencies=[]  VectorFormat=inherit  Unit=rad/s  AffineConversion=off
  cw_L_thumb2 : nesl_utility/PS-Simulink Converter  PhysicalDomain=network_engine_domain  SubClassName=ps_output  LeftPortType=input  RightPortType=output  PseudoPeriodic=off  Frequencies=[]  VectorFormat=inherit  Unit=rad/s  AffineConversion=off
  cw_L_thumb3 : nesl_utility/PS-Simulink Converter  PhysicalDomain=network_engine_domain  SubClassName=ps_output  LeftPortType=input  RightPortType=output  PseudoPeriodic=off  Frequencies=[]  VectorFormat=inherit  Unit=rad/s  AffineConversion=off
  cw_L_toe : nesl_utility/PS-Simulink Converter  PhysicalDomain=network_engine_domain  SubClassName=ps_output  LeftPortType=input  RightPortType=output  PseudoPeriodic=off  Frequencies=[]  VectorFormat=inherit  Unit=rad/s  AffineConversion=off
  cw_L_wrist_pitch : nesl_utility/PS-Simulink Converter  PhysicalDomain=network_engine_domain  SubClassName=ps_output  LeftPortType=input  RightPortType=output  PseudoPeriodic=off  Frequencies=[]  VectorFormat=inherit  Unit=rad/s  AffineConversion=off
  cw_L_wrist_roll : nesl_utility/PS-Simulink Converter  PhysicalDomain=network_engine_domain  SubClassName=ps_output  LeftPortType=input  RightPortType=output  PseudoPeriodic=off  Frequencies=[]  VectorFormat=inherit  Unit=rad/s  AffineConversion=off
  cw_L_wrist_yaw : nesl_utility/PS-Simulink Converter  PhysicalDomain=network_engine_domain  SubClassName=ps_output  LeftPortType=input  RightPortType=output  PseudoPeriodic=off  Frequencies=[]  VectorFormat=inherit  Unit=rad/s  AffineConversion=off
  cw_R_ankle_pitch : nesl_utility/PS-Simulink Converter  PhysicalDomain=network_engine_domain  SubClassName=ps_output  LeftPortType=input  RightPortType=output  PseudoPeriodic=off  Frequencies=[]  VectorFormat=inherit  Unit=rad/s  AffineConversion=off
  cw_R_ankle_roll : nesl_utility/PS-Simulink Converter  PhysicalDomain=network_engine_domain  SubClassName=ps_output  LeftPortType=input  RightPortType=output  PseudoPeriodic=off  Frequencies=[]  VectorFormat=inherit  Unit=rad/s  AffineConversion=off
  cw_R_clavicle : nesl_utility/PS-Simulink Converter  PhysicalDomain=network_engine_domain  SubClassName=ps_output  LeftPortType=input  RightPortType=output  PseudoPeriodic=off  Frequencies=[]  VectorFormat=inherit  Unit=rad/s  AffineConversion=off
  cw_R_elbow : nesl_utility/PS-Simulink Converter  PhysicalDomain=network_engine_domain  SubClassName=ps_output  LeftPortType=input  RightPortType=output  PseudoPeriodic=off  Frequencies=[]  VectorFormat=inherit  Unit=rad/s  AffineConversion=off
  cw_R_forearm_twist : nesl_utility/PS-Simulink Converter  PhysicalDomain=network_engine_domain  SubClassName=ps_output  LeftPortType=input  RightPortType=output  PseudoPeriodic=off  Frequencies=[]  VectorFormat=inherit  Unit=rad/s  AffineConversion=off
  cw_R_hip_pitch : nesl_utility/PS-Simulink Converter  PhysicalDomain=network_engine_domain  SubClassName=ps_output  LeftPortType=input  RightPortType=output  PseudoPeriodic=off  Frequencies=[]  VectorFormat=inherit  Unit=rad/s  AffineConversion=off
  cw_R_hip_roll : nesl_utility/PS-Simulink Converter  PhysicalDomain=network_engine_domain  SubClassName=ps_output  LeftPortType=input  RightPortType=output  PseudoPeriodic=off  Frequencies=[]  VectorFormat=inherit  Unit=rad/s  AffineConversion=off
  cw_R_hip_yaw : nesl_utility/PS-Simulink Converter  PhysicalDomain=network_engine_domain  SubClassName=ps_output  LeftPortType=input  RightPortType=output  PseudoPeriodic=off  Frequencies=[]  VectorFormat=inherit  Unit=rad/s  AffineConversion=off
  cw_R_index1 : nesl_utility/PS-Simulink Converter  PhysicalDomain=network_engine_domain  SubClassName=ps_output  LeftPortType=input  RightPortType=output  PseudoPeriodic=off  Frequencies=[]  VectorFormat=inherit  Unit=rad/s  AffineConversion=off
  cw_R_index2 : nesl_utility/PS-Simulink Converter  PhysicalDomain=network_engine_domain  SubClassName=ps_output  LeftPortType=input  RightPortType=output  PseudoPeriodic=off  Frequencies=[]  VectorFormat=inherit  Unit=rad/s  AffineConversion=off
  cw_R_index3 : nesl_utility/PS-Simulink Converter  PhysicalDomain=network_engine_domain  SubClassName=ps_output  LeftPortType=input  RightPortType=output  PseudoPeriodic=off  Frequencies=[]  VectorFormat=inherit  Unit=rad/s  AffineConversion=off
  cw_R_knee : nesl_utility/PS-Simulink Converter  PhysicalDomain=network_engine_domain  SubClassName=ps_output  LeftPortType=input  RightPortType=output  PseudoPeriodic=off  Frequencies=[]  VectorFormat=inherit  Unit=rad/s  AffineConversion=off
  cw_R_little1 : nesl_utility/PS-Simulink Converter  PhysicalDomain=network_engine_domain  SubClassName=ps_output  LeftPortType=input  RightPortType=output  PseudoPeriodic=off  Frequencies=[]  VectorFormat=inherit  Unit=rad/s  AffineConversion=off
  cw_R_little2 : nesl_utility/PS-Simulink Converter  PhysicalDomain=network_engine_domain  SubClassName=ps_output  LeftPortType=input  RightPortType=output  PseudoPeriodic=off  Frequencies=[]  VectorFormat=inherit  Unit=rad/s  AffineConversion=off
  cw_R_little3 : nesl_utility/PS-Simulink Converter  PhysicalDomain=network_engine_domain  SubClassName=ps_output  LeftPortType=input  RightPortType=output  PseudoPeriodic=off  Frequencies=[]  VectorFormat=inherit  Unit=rad/s  AffineConversion=off
  cw_R_middle1 : nesl_utility/PS-Simulink Converter  PhysicalDomain=network_engine_domain  SubClassName=ps_output  LeftPortType=input  RightPortType=output  PseudoPeriodic=off  Frequencies=[]  VectorFormat=inherit  Unit=rad/s  AffineConversion=off
  cw_R_middle2 : nesl_utility/PS-Simulink Converter  PhysicalDomain=network_engine_domain  SubClassName=ps_output  LeftPortType=input  RightPortType=output  PseudoPeriodic=off  Frequencies=[]  VectorFormat=inherit  Unit=rad/s  AffineConversion=off
  cw_R_middle3 : nesl_utility/PS-Simulink Converter  PhysicalDomain=network_engine_domain  SubClassName=ps_output  LeftPortType=input  RightPortType=output  PseudoPeriodic=off  Frequencies=[]  VectorFormat=inherit  Unit=rad/s  AffineConversion=off
  cw_R_ring1 : nesl_utility/PS-Simulink Converter  PhysicalDomain=network_engine_domain  SubClassName=ps_output  LeftPortType=input  RightPortType=output  PseudoPeriodic=off  Frequencies=[]  VectorFormat=inherit  Unit=rad/s  AffineConversion=off
  cw_R_ring2 : nesl_utility/PS-Simulink Converter  PhysicalDomain=network_engine_domain  SubClassName=ps_output  LeftPortType=input  RightPortType=output  PseudoPeriodic=off  Frequencies=[]  VectorFormat=inherit  Unit=rad/s  AffineConversion=off
  cw_R_ring3 : nesl_utility/PS-Simulink Converter  PhysicalDomain=network_engine_domain  SubClassName=ps_output  LeftPortType=input  RightPortType=output  PseudoPeriodic=off  Frequencies=[]  VectorFormat=inherit  Unit=rad/s  AffineConversion=off
  cw_R_scapula : nesl_utility/PS-Simulink Converter  PhysicalDomain=network_engine_domain  SubClassName=ps_output  LeftPortType=input  RightPortType=output  PseudoPeriodic=off  Frequencies=[]  VectorFormat=inherit  Unit=rad/s  AffineConversion=off
  cw_R_shoulder_pitch : nesl_utility/PS-Simulink Converter  PhysicalDomain=network_engine_domain  SubClassName=ps_output  LeftPortType=input  RightPortType=output  PseudoPeriodic=off  Frequencies=[]  VectorFormat=inherit  Unit=rad/s  AffineConversion=off
  cw_R_shoulder_roll : nesl_utility/PS-Simulink Converter  PhysicalDomain=network_engine_domain  SubClassName=ps_output  LeftPortType=input  RightPortType=output  PseudoPeriodic=off  Frequencies=[]  VectorFormat=inherit  Unit=rad/s  AffineConversion=off
  cw_R_shoulder_yaw : nesl_utility/PS-Simulink Converter  PhysicalDomain=network_engine_domain  SubClassName=ps_output  LeftPortType=input  RightPortType=output  PseudoPeriodic=off  Frequencies=[]  VectorFormat=inherit  Unit=rad/s  AffineConversion=off
  cw_R_thumb1 : nesl_utility/PS-Simulink Converter  PhysicalDomain=network_engine_domain  SubClassName=ps_output  LeftPortType=input  RightPortType=output  PseudoPeriodic=off  Frequencies=[]  VectorFormat=inherit  Unit=rad/s  AffineConversion=off
  cw_R_thumb2 : nesl_utility/PS-Simulink Converter  PhysicalDomain=network_engine_domain  SubClassName=ps_output  LeftPortType=input  RightPortType=output  PseudoPeriodic=off  Frequencies=[]  VectorFormat=inherit  Unit=rad/s  AffineConversion=off
  cw_R_thumb3 : nesl_utility/PS-Simulink Converter  PhysicalDomain=network_engine_domain  SubClassName=ps_output  LeftPortType=input  RightPortType=output  PseudoPeriodic=off  Frequencies=[]  VectorFormat=inherit  Unit=rad/s  AffineConversion=off
  cw_R_toe : nesl_utility/PS-Simulink Converter  PhysicalDomain=network_engine_domain  SubClassName=ps_output  LeftPortType=input  RightPortType=output  PseudoPeriodic=off  Frequencies=[]  VectorFormat=inherit  Unit=rad/s  AffineConversion=off
  cw_R_wrist_pitch : nesl_utility/PS-Simulink Converter  PhysicalDomain=network_engine_domain  SubClassName=ps_output  LeftPortType=input  RightPortType=output  PseudoPeriodic=off  Frequencies=[]  VectorFormat=inherit  Unit=rad/s  AffineConversion=off
  cw_R_wrist_roll : nesl_utility/PS-Simulink Converter  PhysicalDomain=network_engine_domain  SubClassName=ps_output  LeftPortType=input  RightPortType=output  PseudoPeriodic=off  Frequencies=[]  VectorFormat=inherit  Unit=rad/s  AffineConversion=off
  cw_R_wrist_yaw : nesl_utility/PS-Simulink Converter  PhysicalDomain=network_engine_domain  SubClassName=ps_output  LeftPortType=input  RightPortType=output  PseudoPeriodic=off  Frequencies=[]  VectorFormat=inherit  Unit=rad/s  AffineConversion=off
  cw_neck_pitch : nesl_utility/PS-Simulink Converter  PhysicalDomain=network_engine_domain  SubClassName=ps_output  LeftPortType=input  RightPortType=output  PseudoPeriodic=off  Frequencies=[]  VectorFormat=inherit  Unit=rad/s  AffineConversion=off
  cw_neck_roll : nesl_utility/PS-Simulink Converter  PhysicalDomain=network_engine_domain  SubClassName=ps_output  LeftPortType=input  RightPortType=output  PseudoPeriodic=off  Frequencies=[]  VectorFormat=inherit  Unit=rad/s  AffineConversion=off
  cw_neck_yaw : nesl_utility/PS-Simulink Converter  PhysicalDomain=network_engine_domain  SubClassName=ps_output  LeftPortType=input  RightPortType=output  PseudoPeriodic=off  Frequencies=[]  VectorFormat=inherit  Unit=rad/s  AffineConversion=off
  cw_waist_pitch : nesl_utility/PS-Simulink Converter  PhysicalDomain=network_engine_domain  SubClassName=ps_output  LeftPortType=input  RightPortType=output  PseudoPeriodic=off  Frequencies=[]  VectorFormat=inherit  Unit=rad/s  AffineConversion=off
  cw_waist_roll : nesl_utility/PS-Simulink Converter  PhysicalDomain=network_engine_domain  SubClassName=ps_output  LeftPortType=input  RightPortType=output  PseudoPeriodic=off  Frequencies=[]  VectorFormat=inherit  Unit=rad/s  AffineConversion=off
  cw_waist_yaw : nesl_utility/PS-Simulink Converter  PhysicalDomain=network_engine_domain  SubClassName=ps_output  LeftPortType=input  RightPortType=output  PseudoPeriodic=off  Frequencies=[]  VectorFormat=inherit  Unit=rad/s  AffineConversion=off
  err_X : Sum  Inputs=+-
  err_XDot : Sum  Inputs=+-
  err_Y : Sum  Inputs=+-
  err_YDot : Sum  Inputs=+-
  fb_gxd : Gain  Gain=Mtot*9.81*1.1
  fb_gxp : Gain  Gain=Mtot*9.81*3.0
  fb_gyd : Gain  Gain=-Mtot*9.81*0.6
  fb_gyp : Gain  Gain=-Mtot*9.81*2.0
  fb_pm_L1 : Product
  fb_pm_L2 : Product
  fb_pm_R1 : Product
  fb_pm_R2 : Product
  fb_satx : Saturate  UpperLimit=Mtot*9.81*0.08  LowerLimit=-Mtot*9.81*0.08
  fb_saty : Saturate  UpperLimit=Mtot*9.81*0.05  LowerLimit=-Mtot*9.81*0.05
  fb_sx : Sum
  fb_sy : Sum
  gT_L_ankle_pitch : Gain  Gain=Tpk(1)
  gT_L_ankle_roll : Gain  Gain=Tpk(2)
  gT_L_clavicle : Gain  Gain=Tpk(3)
  gT_L_elbow : Gain  Gain=Tpk(4)
  gT_L_forearm_twist : Gain  Gain=Tpk(5)
  gT_L_hip_pitch : Gain  Gain=Tpk(6)
  gT_L_hip_roll : Gain  Gain=Tpk(7)
  gT_L_hip_yaw : Gain  Gain=Tpk(8)
  gT_L_index1 : Gain  Gain=Tpk(9)
  gT_L_index2 : Gain  Gain=Tpk(10)
  gT_L_index3 : Gain  Gain=Tpk(11)
  gT_L_knee : Gain  Gain=Tpk(12)
  gT_L_little1 : Gain  Gain=Tpk(13)
  gT_L_little2 : Gain  Gain=Tpk(14)
  gT_L_little3 : Gain  Gain=Tpk(15)
  gT_L_middle1 : Gain  Gain=Tpk(16)
  gT_L_middle2 : Gain  Gain=Tpk(17)
  gT_L_middle3 : Gain  Gain=Tpk(18)
  gT_L_ring1 : Gain  Gain=Tpk(19)
  gT_L_ring2 : Gain  Gain=Tpk(20)
  gT_L_ring3 : Gain  Gain=Tpk(21)
  gT_L_scapula : Gain  Gain=Tpk(22)
  gT_L_shoulder_pitch : Gain  Gain=Tpk(23)
  gT_L_shoulder_roll : Gain  Gain=Tpk(24)
  gT_L_shoulder_yaw : Gain  Gain=Tpk(25)
  gT_L_thumb1 : Gain  Gain=Tpk(26)
  gT_L_thumb2 : Gain  Gain=Tpk(27)
  gT_L_thumb3 : Gain  Gain=Tpk(28)
  gT_L_toe : Gain  Gain=Tpk(29)
  gT_L_wrist_pitch : Gain  Gain=Tpk(30)
  gT_L_wrist_roll : Gain  Gain=Tpk(31)
  gT_L_wrist_yaw : Gain  Gain=Tpk(32)
  gT_R_ankle_pitch : Gain  Gain=Tpk(33)
  gT_R_ankle_roll : Gain  Gain=Tpk(34)
  gT_R_clavicle : Gain  Gain=Tpk(35)
  gT_R_elbow : Gain  Gain=Tpk(36)
  gT_R_forearm_twist : Gain  Gain=Tpk(37)
  gT_R_hip_pitch : Gain  Gain=Tpk(38)
  gT_R_hip_roll : Gain  Gain=Tpk(39)
  gT_R_hip_yaw : Gain  Gain=Tpk(40)
  gT_R_index1 : Gain  Gain=Tpk(41)
  gT_R_index2 : Gain  Gain=Tpk(42)
  gT_R_index3 : Gain  Gain=Tpk(43)
  gT_R_knee : Gain  Gain=Tpk(44)
  gT_R_little1 : Gain  Gain=Tpk(45)
  gT_R_little2 : Gain  Gain=Tpk(46)
  gT_R_little3 : Gain  Gain=Tpk(47)
  gT_R_middle1 : Gain  Gain=Tpk(48)
  gT_R_middle2 : Gain  Gain=Tpk(49)
  gT_R_middle3 : Gain  Gain=Tpk(50)
  gT_R_ring1 : Gain  Gain=Tpk(51)
  gT_R_ring2 : Gain  Gain=Tpk(52)
  gT_R_ring3 : Gain  Gain=Tpk(53)
  gT_R_scapula : Gain  Gain=Tpk(54)
  gT_R_shoulder_pitch : Gain  Gain=Tpk(55)
  gT_R_shoulder_roll : Gain  Gain=Tpk(56)
  gT_R_shoulder_yaw : Gain  Gain=Tpk(57)
  gT_R_thumb1 : Gain  Gain=Tpk(58)
  gT_R_thumb2 : Gain  Gain=Tpk(59)
  gT_R_thumb3 : Gain  Gain=Tpk(60)
  gT_R_toe : Gain  Gain=Tpk(61)
  gT_R_wrist_pitch : Gain  Gain=Tpk(62)
  gT_R_wrist_roll : Gain  Gain=Tpk(63)
  gT_R_wrist_yaw : Gain  Gain=Tpk(64)
  gT_neck_pitch : Gain  Gain=Tpk(65)
  gT_neck_roll : Gain  Gain=Tpk(66)
  gT_neck_yaw : Gain  Gain=Tpk(67)
  gT_waist_pitch : Gain  Gain=Tpk(68)
  gT_waist_roll : Gain  Gain=Tpk(69)
  gT_waist_yaw : Gain  Gain=Tpk(70)
  gn_L_ankle_pitch : Gain  Gain=-1
  gn_L_ankle_roll : Gain  Gain=-1
  gn_L_clavicle : Gain  Gain=-1
  gn_L_elbow : Gain  Gain=-1
  gn_L_forearm_twist : Gain  Gain=-1
  gn_L_hip_pitch : Gain  Gain=-1
  gn_L_hip_roll : Gain  Gain=-1
  gn_L_hip_yaw : Gain  Gain=-1
  gn_L_index1 : Gain  Gain=-1
  gn_L_index2 : Gain  Gain=-1
  gn_L_index3 : Gain  Gain=-1
  gn_L_knee : Gain  Gain=-1
  gn_L_little1 : Gain  Gain=-1
  gn_L_little2 : Gain  Gain=-1
  gn_L_little3 : Gain  Gain=-1
  gn_L_middle1 : Gain  Gain=-1
  gn_L_middle2 : Gain  Gain=-1
  gn_L_middle3 : Gain  Gain=-1
  gn_L_ring1 : Gain  Gain=-1
  gn_L_ring2 : Gain  Gain=-1
  gn_L_ring3 : Gain  Gain=-1
  gn_L_scapula : Gain  Gain=-1
  gn_L_shoulder_pitch : Gain  Gain=-1
  gn_L_shoulder_roll : Gain  Gain=-1
  gn_L_shoulder_yaw : Gain  Gain=-1
  gn_L_thumb1 : Gain  Gain=-1
  gn_L_thumb2 : Gain  Gain=-1
  gn_L_thumb3 : Gain  Gain=-1
  gn_L_toe : Gain  Gain=-1
  gn_L_wrist_pitch : Gain  Gain=-1
  gn_L_wrist_roll : Gain  Gain=-1
  gn_L_wrist_yaw : Gain  Gain=-1
  gn_R_ankle_pitch : Gain  Gain=-1
  gn_R_ankle_roll : Gain  Gain=-1
  gn_R_clavicle : Gain  Gain=-1
  gn_R_elbow : Gain  Gain=-1
  gn_R_forearm_twist : Gain  Gain=-1
  gn_R_hip_pitch : Gain  Gain=-1
  gn_R_hip_roll : Gain  Gain=-1
  gn_R_hip_yaw : Gain  Gain=-1
  gn_R_index1 : Gain  Gain=-1
  gn_R_index2 : Gain  Gain=-1
  gn_R_index3 : Gain  Gain=-1
  gn_R_knee : Gain  Gain=-1
  gn_R_little1 : Gain  Gain=-1
  gn_R_little2 : Gain  Gain=-1
  gn_R_little3 : Gain  Gain=-1
  gn_R_middle1 : Gain  Gain=-1
  gn_R_middle2 : Gain  Gain=-1
  gn_R_middle3 : Gain  Gain=-1
  gn_R_ring1 : Gain  Gain=-1
  gn_R_ring2 : Gain  Gain=-1
  gn_R_ring3 : Gain  Gain=-1
  gn_R_scapula : Gain  Gain=-1
  gn_R_shoulder_pitch : Gain  Gain=-1
  gn_R_shoulder_roll : Gain  Gain=-1
  gn_R_shoulder_yaw : Gain  Gain=-1
  gn_R_thumb1 : Gain  Gain=-1
  gn_R_thumb2 : Gain  Gain=-1
  gn_R_thumb3 : Gain  Gain=-1
  gn_R_toe : Gain  Gain=-1
  gn_R_wrist_pitch : Gain  Gain=-1
  gn_R_wrist_roll : Gain  Gain=-1
  gn_R_wrist_yaw : Gain  Gain=-1
  gn_neck_pitch : Gain  Gain=-1
  gn_neck_roll : Gain  Gain=-1
  gn_neck_yaw : Gain  Gain=-1
  gn_waist_pitch : Gain  Gain=-1
  gn_waist_roll : Gain  Gain=-1
  gn_waist_yaw : Gain  Gain=-1
  gnd_L{1..4} (4 alike) : sm_lib/Body Elements/Brick Solid  BrickDimensions=[30 6 0.2]  BrickDimensionsUnits=m  ExportEntireGeometry=on  InertiaType=CalculateFromGeometry  BasedOnType=Density  Density=1000  DensityUnits=kg/m^3  Mass=1  MassUnits=kg  CenterOfMass=[0 0 0]  CenterOfMassUnits=m  MomentsOfInertia=[1 1 1]  MomentsOfInertiaUnits=kg*m^2  ProductsOfInertia=[0 0 0]  ProductsOfInertiaUnits=kg*m^2  GraphicType=None  MarkerShape=Sphere  MarkerSize=10  GraphicVisPropType=SimpleVisualProperties  GraphicDiffuseColor=[0.5 0.5 0.5]  GraphicOpacity=1  GraphicSpecularColor=[0.5 0.5 0.5 1.0]  GraphicAmbientColor=[0.15 0.15 0.15 1.0]  GraphicEmissiveColor=[0.0 0.0 0.0 1.0]  GraphicShininess=75  DoExposeReferenceFrame=on  SerializedFrames=<Frames/>
  gnd_R{1..4} (4 alike) : sm_lib/Body Elements/Brick Solid  BrickDimensions=[30 6 0.2]  BrickDimensionsUnits=m  ExportEntireGeometry=on  InertiaType=CalculateFromGeometry  BasedOnType=Density  Density=1000  DensityUnits=kg/m^3  Mass=1  MassUnits=kg  CenterOfMass=[0 0 0]  CenterOfMassUnits=m  MomentsOfInertia=[1 1 1]  MomentsOfInertiaUnits=kg*m^2  ProductsOfInertia=[0 0 0]  ProductsOfInertiaUnits=kg*m^2  GraphicType=None  MarkerShape=Sphere  MarkerSize=10  GraphicVisPropType=SimpleVisualProperties  GraphicDiffuseColor=[0.5 0.5 0.5]  GraphicOpacity=1  GraphicSpecularColor=[0.5 0.5 0.5 1.0]  GraphicAmbientColor=[0.15 0.15 0.15 1.0]  GraphicEmissiveColor=[0.0 0.0 0.0 1.0]  GraphicShininess=75  DoExposeReferenceFrame=on  SerializedFrames=<Frames/>
  gw_L_ankle_pitch : Gain  Gain=-1/Wnl(1)
  gw_L_ankle_roll : Gain  Gain=-1/Wnl(2)
  gw_L_clavicle : Gain  Gain=-1/Wnl(3)
  gw_L_elbow : Gain  Gain=-1/Wnl(4)
  gw_L_forearm_twist : Gain  Gain=-1/Wnl(5)
  gw_L_hip_pitch : Gain  Gain=-1/Wnl(6)
  gw_L_hip_roll : Gain  Gain=-1/Wnl(7)
  gw_L_hip_yaw : Gain  Gain=-1/Wnl(8)
  gw_L_index1 : Gain  Gain=-1/Wnl(9)
  gw_L_index2 : Gain  Gain=-1/Wnl(10)
  gw_L_index3 : Gain  Gain=-1/Wnl(11)
  gw_L_knee : Gain  Gain=-1/Wnl(12)
  gw_L_little1 : Gain  Gain=-1/Wnl(13)
  gw_L_little2 : Gain  Gain=-1/Wnl(14)
  gw_L_little3 : Gain  Gain=-1/Wnl(15)
  gw_L_middle1 : Gain  Gain=-1/Wnl(16)
  gw_L_middle2 : Gain  Gain=-1/Wnl(17)
  gw_L_middle3 : Gain  Gain=-1/Wnl(18)
  gw_L_ring1 : Gain  Gain=-1/Wnl(19)
  gw_L_ring2 : Gain  Gain=-1/Wnl(20)
  gw_L_ring3 : Gain  Gain=-1/Wnl(21)
  gw_L_scapula : Gain  Gain=-1/Wnl(22)
  gw_L_shoulder_pitch : Gain  Gain=-1/Wnl(23)
  gw_L_shoulder_roll : Gain  Gain=-1/Wnl(24)
  gw_L_shoulder_yaw : Gain  Gain=-1/Wnl(25)
  gw_L_thumb1 : Gain  Gain=-1/Wnl(26)
  gw_L_thumb2 : Gain  Gain=-1/Wnl(27)
  gw_L_thumb3 : Gain  Gain=-1/Wnl(28)
  gw_L_toe : Gain  Gain=-1/Wnl(29)
  gw_L_wrist_pitch : Gain  Gain=-1/Wnl(30)
  gw_L_wrist_roll : Gain  Gain=-1/Wnl(31)
  gw_L_wrist_yaw : Gain  Gain=-1/Wnl(32)
  gw_R_ankle_pitch : Gain  Gain=-1/Wnl(33)
  gw_R_ankle_roll : Gain  Gain=-1/Wnl(34)
  gw_R_clavicle : Gain  Gain=-1/Wnl(35)
  gw_R_elbow : Gain  Gain=-1/Wnl(36)
  gw_R_forearm_twist : Gain  Gain=-1/Wnl(37)
  gw_R_hip_pitch : Gain  Gain=-1/Wnl(38)
  gw_R_hip_roll : Gain  Gain=-1/Wnl(39)
  gw_R_hip_yaw : Gain  Gain=-1/Wnl(40)
  gw_R_index1 : Gain  Gain=-1/Wnl(41)
  gw_R_index2 : Gain  Gain=-1/Wnl(42)
  gw_R_index3 : Gain  Gain=-1/Wnl(43)
  gw_R_knee : Gain  Gain=-1/Wnl(44)
  gw_R_little1 : Gain  Gain=-1/Wnl(45)
  gw_R_little2 : Gain  Gain=-1/Wnl(46)
  gw_R_little3 : Gain  Gain=-1/Wnl(47)
  gw_R_middle1 : Gain  Gain=-1/Wnl(48)
  gw_R_middle2 : Gain  Gain=-1/Wnl(49)
  gw_R_middle3 : Gain  Gain=-1/Wnl(50)
  gw_R_ring1 : Gain  Gain=-1/Wnl(51)
  gw_R_ring2 : Gain  Gain=-1/Wnl(52)
  gw_R_ring3 : Gain  Gain=-1/Wnl(53)
  gw_R_scapula : Gain  Gain=-1/Wnl(54)
  gw_R_shoulder_pitch : Gain  Gain=-1/Wnl(55)
  gw_R_shoulder_roll : Gain  Gain=-1/Wnl(56)
  gw_R_shoulder_yaw : Gain  Gain=-1/Wnl(57)
  gw_R_thumb1 : Gain  Gain=-1/Wnl(58)
  gw_R_thumb2 : Gain  Gain=-1/Wnl(59)
  gw_R_thumb3 : Gain  Gain=-1/Wnl(60)
  gw_R_toe : Gain  Gain=-1/Wnl(61)
  gw_R_wrist_pitch : Gain  Gain=-1/Wnl(62)
  gw_R_wrist_roll : Gain  Gain=-1/Wnl(63)
  gw_R_wrist_yaw : Gain  Gain=-1/Wnl(64)
  gw_neck_pitch : Gain  Gain=-1/Wnl(65)
  gw_neck_roll : Gain  Gain=-1/Wnl(66)
  gw_neck_yaw : Gain  Gain=-1/Wnl(67)
  gw_waist_pitch : Gain  Gain=-1/Wnl(68)
  gw_waist_roll : Gain  Gain=-1/Wnl(69)
  gw_waist_yaw : Gain  Gain=-1/Wnl(70)
  head : Subsystem
  lam : FromWorkspace  VariableName=lam  OutputAfterFinalValue=Holding final value
  lam_demux : Demux  Outputs=2
  mn_L_ankle_pitch : MinMax  Inputs=2
  mn_L_ankle_roll : MinMax  Inputs=2
  mn_L_clavicle : MinMax  Inputs=2
  mn_L_elbow : MinMax  Inputs=2
  mn_L_forearm_twist : MinMax  Inputs=2
  mn_L_hip_pitch : MinMax  Inputs=2
  mn_L_hip_roll : MinMax  Inputs=2
  mn_L_hip_yaw : MinMax  Inputs=2
  mn_L_index1 : MinMax  Inputs=2
  mn_L_index2 : MinMax  Inputs=2
  mn_L_index3 : MinMax  Inputs=2
  mn_L_knee : MinMax  Inputs=2
  mn_L_little1 : MinMax  Inputs=2
  mn_L_little2 : MinMax  Inputs=2
  mn_L_little3 : MinMax  Inputs=2
  mn_L_middle1 : MinMax  Inputs=2
  mn_L_middle2 : MinMax  Inputs=2
  mn_L_middle3 : MinMax  Inputs=2
  mn_L_ring1 : MinMax  Inputs=2
  mn_L_ring2 : MinMax  Inputs=2
  mn_L_ring3 : MinMax  Inputs=2
  mn_L_scapula : MinMax  Inputs=2
  mn_L_shoulder_pitch : MinMax  Inputs=2
  mn_L_shoulder_roll : MinMax  Inputs=2
  mn_L_shoulder_yaw : MinMax  Inputs=2
  mn_L_thumb1 : MinMax  Inputs=2
  mn_L_thumb2 : MinMax  Inputs=2
  mn_L_thumb3 : MinMax  Inputs=2
  mn_L_toe : MinMax  Inputs=2
  mn_L_wrist_pitch : MinMax  Inputs=2
  mn_L_wrist_roll : MinMax  Inputs=2
  mn_L_wrist_yaw : MinMax  Inputs=2
  mn_R_ankle_pitch : MinMax  Inputs=2
  mn_R_ankle_roll : MinMax  Inputs=2
  mn_R_clavicle : MinMax  Inputs=2
  mn_R_elbow : MinMax  Inputs=2
  mn_R_forearm_twist : MinMax  Inputs=2
  mn_R_hip_pitch : MinMax  Inputs=2
  mn_R_hip_roll : MinMax  Inputs=2
  mn_R_hip_yaw : MinMax  Inputs=2
  mn_R_index1 : MinMax  Inputs=2
  mn_R_index2 : MinMax  Inputs=2
  mn_R_index3 : MinMax  Inputs=2
  mn_R_knee : MinMax  Inputs=2
  mn_R_little1 : MinMax  Inputs=2
  mn_R_little2 : MinMax  Inputs=2
  mn_R_little3 : MinMax  Inputs=2
  mn_R_middle1 : MinMax  Inputs=2
  mn_R_middle2 : MinMax  Inputs=2
  mn_R_middle3 : MinMax  Inputs=2
  mn_R_ring1 : MinMax  Inputs=2
  mn_R_ring2 : MinMax  Inputs=2
  mn_R_ring3 : MinMax  Inputs=2
  mn_R_scapula : MinMax  Inputs=2
  mn_R_shoulder_pitch : MinMax  Inputs=2
  mn_R_shoulder_roll : MinMax  Inputs=2
  mn_R_shoulder_yaw : MinMax  Inputs=2
  mn_R_thumb1 : MinMax  Inputs=2
  mn_R_thumb2 : MinMax  Inputs=2
  mn_R_thumb3 : MinMax  Inputs=2
  mn_R_toe : MinMax  Inputs=2
  mn_R_wrist_pitch : MinMax  Inputs=2
  mn_R_wrist_roll : MinMax  Inputs=2
  mn_R_wrist_yaw : MinMax  Inputs=2
  mn_neck_pitch : MinMax  Inputs=2
  mn_neck_roll : MinMax  Inputs=2
  mn_neck_yaw : MinMax  Inputs=2
  mn_waist_pitch : MinMax  Inputs=2
  mn_waist_roll : MinMax  Inputs=2
  mn_waist_yaw : MinMax  Inputs=2
  mx_L_ankle_pitch : MinMax  Function=max  Inputs=2
  mx_L_ankle_roll : MinMax  Function=max  Inputs=2
  mx_L_clavicle : MinMax  Function=max  Inputs=2
  mx_L_elbow : MinMax  Function=max  Inputs=2
  mx_L_forearm_twist : MinMax  Function=max  Inputs=2
  mx_L_hip_pitch : MinMax  Function=max  Inputs=2
  mx_L_hip_roll : MinMax  Function=max  Inputs=2
  mx_L_hip_yaw : MinMax  Function=max  Inputs=2
  mx_L_index1 : MinMax  Function=max  Inputs=2
  mx_L_index2 : MinMax  Function=max  Inputs=2
  mx_L_index3 : MinMax  Function=max  Inputs=2
  mx_L_knee : MinMax  Function=max  Inputs=2
  mx_L_little1 : MinMax  Function=max  Inputs=2
  mx_L_little2 : MinMax  Function=max  Inputs=2
  mx_L_little3 : MinMax  Function=max  Inputs=2
  mx_L_middle1 : MinMax  Function=max  Inputs=2
  mx_L_middle2 : MinMax  Function=max  Inputs=2
  mx_L_middle3 : MinMax  Function=max  Inputs=2
  mx_L_ring1 : MinMax  Function=max  Inputs=2
  mx_L_ring2 : MinMax  Function=max  Inputs=2
  mx_L_ring3 : MinMax  Function=max  Inputs=2
  mx_L_scapula : MinMax  Function=max  Inputs=2
  mx_L_shoulder_pitch : MinMax  Function=max  Inputs=2
  mx_L_shoulder_roll : MinMax  Function=max  Inputs=2
  mx_L_shoulder_yaw : MinMax  Function=max  Inputs=2
  mx_L_thumb1 : MinMax  Function=max  Inputs=2
  mx_L_thumb2 : MinMax  Function=max  Inputs=2
  mx_L_thumb3 : MinMax  Function=max  Inputs=2
  mx_L_toe : MinMax  Function=max  Inputs=2
  mx_L_wrist_pitch : MinMax  Function=max  Inputs=2
  mx_L_wrist_roll : MinMax  Function=max  Inputs=2
  mx_L_wrist_yaw : MinMax  Function=max  Inputs=2
  mx_R_ankle_pitch : MinMax  Function=max  Inputs=2
  mx_R_ankle_roll : MinMax  Function=max  Inputs=2
  mx_R_clavicle : MinMax  Function=max  Inputs=2
  mx_R_elbow : MinMax  Function=max  Inputs=2
  mx_R_forearm_twist : MinMax  Function=max  Inputs=2
  mx_R_hip_pitch : MinMax  Function=max  Inputs=2
  mx_R_hip_roll : MinMax  Function=max  Inputs=2
  mx_R_hip_yaw : MinMax  Function=max  Inputs=2
  mx_R_index1 : MinMax  Function=max  Inputs=2
  mx_R_index2 : MinMax  Function=max  Inputs=2
  mx_R_index3 : MinMax  Function=max  Inputs=2
  mx_R_knee : MinMax  Function=max  Inputs=2
  mx_R_little1 : MinMax  Function=max  Inputs=2
  mx_R_little2 : MinMax  Function=max  Inputs=2
  mx_R_little3 : MinMax  Function=max  Inputs=2
  mx_R_middle1 : MinMax  Function=max  Inputs=2
  mx_R_middle2 : MinMax  Function=max  Inputs=2
  mx_R_middle3 : MinMax  Function=max  Inputs=2
  mx_R_ring1 : MinMax  Function=max  Inputs=2
  mx_R_ring2 : MinMax  Function=max  Inputs=2
  mx_R_ring3 : MinMax  Function=max  Inputs=2
  mx_R_scapula : MinMax  Function=max  Inputs=2
  mx_R_shoulder_pitch : MinMax  Function=max  Inputs=2
  mx_R_shoulder_roll : MinMax  Function=max  Inputs=2
  mx_R_shoulder_yaw : MinMax  Function=max  Inputs=2
  mx_R_thumb1 : MinMax  Function=max  Inputs=2
  mx_R_thumb2 : MinMax  Function=max  Inputs=2
  mx_R_thumb3 : MinMax  Function=max  Inputs=2
  mx_R_toe : MinMax  Function=max  Inputs=2
  mx_R_wrist_pitch : MinMax  Function=max  Inputs=2
  mx_R_wrist_roll : MinMax  Function=max  Inputs=2
  mx_R_wrist_yaw : MinMax  Function=max  Inputs=2
  mx_neck_pitch : MinMax  Function=max  Inputs=2
  mx_neck_roll : MinMax  Function=max  Inputs=2
  mx_neck_yaw : MinMax  Function=max  Inputs=2
  mx_waist_pitch : MinMax  Function=max  Inputs=2
  mx_waist_roll : MinMax  Function=max  Inputs=2
  mx_waist_yaw : MinMax  Function=max  Inputs=2
  neck_pitch : sm_lib/Joints/Revolute Joint  JointMode=Normal  CompositeWrenchDir=FollowerOnBase  CompositeWrenchFrame=BaseFrame  SenseConstraintForce=off  SenseConstraintTorque=off  SenseTotalForce=off  SenseTotalTorque=off  PositionTargetSpecify=on  PositionTargetPriority=High  PositionTargetValue=0  PositionTargetValueUnits=rad  VelocityTargetSpecify=off  VelocityTargetPriority=High  VelocityTargetValue=0  VelocityTargetValueUnits=deg/s  EquilibriumPosition=0  EquilibriumPositionUnits=deg  SpringStiffness=0  SpringStiffnessUnits=N*m/deg  DampingCoefficient=0.3  DampingCoefficientUnits=kg*m^2/(rad*s)  LowerLimitSpecify=on  LowerLimitBound=-0.6108652381980153  LowerLimitBoundUnits=rad  LowerLimitStiffness=1e4  LowerLimitStiffnessUnits=N*m/deg  LowerLimitDamping=10  LowerLimitDampingUnits=N*m/(deg/s)  LowerLimitTransitionRegionWidth=0.1  LowerLimitTransitionRegionWidthUnits=deg  UpperLimitSpecify=on  UpperLimitBound=0.6108652381980153  UpperLimitBoundUnits=rad  UpperLimitStiffness=1e4  UpperLimitStiffnessUnits=N*m/deg  UpperLimitDamping=10  UpperLimitDampingUnits=N*m/(deg/s)  UpperLimitTransitionRegionWidth=0.1  UpperLimitTransitionRegionWidthUnits=deg  TorqueActuationMode=InputTorque  MotionActuationMode=ComputedMotion  SensePosition=on  SenseVelocity=on  SenseAcceleration=off  SenseTorqueForce=off  SenseLowerLimitTorqueForce=off  SenseUpperLimitTorqueForce=off
  neck_roll : sm_lib/Joints/Revolute Joint  JointMode=Normal  CompositeWrenchDir=FollowerOnBase  CompositeWrenchFrame=BaseFrame  SenseConstraintForce=off  SenseConstraintTorque=off  SenseTotalForce=off  SenseTotalTorque=off  PositionTargetSpecify=on  PositionTargetPriority=High  PositionTargetValue=0  PositionTargetValueUnits=rad  VelocityTargetSpecify=off  VelocityTargetPriority=High  VelocityTargetValue=0  VelocityTargetValueUnits=deg/s  EquilibriumPosition=0  EquilibriumPositionUnits=deg  SpringStiffness=0  SpringStiffnessUnits=N*m/deg  DampingCoefficient=0.3  DampingCoefficientUnits=kg*m^2/(rad*s)  LowerLimitSpecify=on  LowerLimitBound=-0.3490658503988659  LowerLimitBoundUnits=rad  LowerLimitStiffness=1e4  LowerLimitStiffnessUnits=N*m/deg  LowerLimitDamping=10  LowerLimitDampingUnits=N*m/(deg/s)  LowerLimitTransitionRegionWidth=0.1  LowerLimitTransitionRegionWidthUnits=deg  UpperLimitSpecify=on  UpperLimitBound=0.3490658503988659  UpperLimitBoundUnits=rad  UpperLimitStiffness=1e4  UpperLimitStiffnessUnits=N*m/deg  UpperLimitDamping=10  UpperLimitDampingUnits=N*m/(deg/s)  UpperLimitTransitionRegionWidth=0.1  UpperLimitTransitionRegionWidthUnits=deg  TorqueActuationMode=InputTorque  MotionActuationMode=ComputedMotion  SensePosition=on  SenseVelocity=on  SenseAcceleration=off  SenseTorqueForce=off  SenseLowerLimitTorqueForce=off  SenseUpperLimitTorqueForce=off
  neck_roll1 : Subsystem
  neck_yaw : sm_lib/Joints/Revolute Joint  JointMode=Normal  CompositeWrenchDir=FollowerOnBase  CompositeWrenchFrame=BaseFrame  SenseConstraintForce=off  SenseConstraintTorque=off  SenseTotalForce=off  SenseTotalTorque=off  PositionTargetSpecify=on  PositionTargetPriority=High  PositionTargetValue=0  PositionTargetValueUnits=rad  VelocityTargetSpecify=off  VelocityTargetPriority=High  VelocityTargetValue=0  VelocityTargetValueUnits=deg/s  EquilibriumPosition=0  EquilibriumPositionUnits=deg  SpringStiffness=0  SpringStiffnessUnits=N*m/deg  DampingCoefficient=0.3  DampingCoefficientUnits=kg*m^2/(rad*s)  LowerLimitSpecify=on  LowerLimitBound=-1.48352986419518  LowerLimitBoundUnits=rad  LowerLimitStiffness=1e4  LowerLimitStiffnessUnits=N*m/deg  LowerLimitDamping=10  LowerLimitDampingUnits=N*m/(deg/s)  LowerLimitTransitionRegionWidth=0.1  LowerLimitTransitionRegionWidthUnits=deg  UpperLimitSpecify=on  UpperLimitBound=1.48352986419518  UpperLimitBoundUnits=rad  UpperLimitStiffness=1e4  UpperLimitStiffnessUnits=N*m/deg  UpperLimitDamping=10  UpperLimitDampingUnits=N*m/(deg/s)  UpperLimitTransitionRegionWidth=0.1  UpperLimitTransitionRegionWidthUnits=deg  TorqueActuationMode=InputTorque  MotionActuationMode=ComputedMotion  SensePosition=on  SenseVelocity=on  SenseAcceleration=off  SenseTorqueForce=off  SenseLowerLimitTorqueForce=off  SenseUpperLimitTorqueForce=off
  neck_yaw1 : Subsystem
  pb_L_ankle_pitch : Product
  pb_L_hip_pitch : Product
  pb_L_knee : Product
  pb_R_ankle_pitch : Product
  pb_R_hip_pitch : Product
  pb_R_knee : Product
  pc_X : nesl_utility/PS-Simulink Converter  PhysicalDomain=network_engine_domain  SubClassName=ps_output  LeftPortType=input  RightPortType=output  PseudoPeriodic=off  Frequencies=[]  VectorFormat=inherit  Unit=m  AffineConversion=off
  pc_XDot : nesl_utility/PS-Simulink Converter  PhysicalDomain=network_engine_domain  SubClassName=ps_output  LeftPortType=input  RightPortType=output  PseudoPeriodic=off  Frequencies=[]  VectorFormat=inherit  Unit=m/s  AffineConversion=off
  pc_Y : nesl_utility/PS-Simulink Converter  PhysicalDomain=network_engine_domain  SubClassName=ps_output  LeftPortType=input  RightPortType=output  PseudoPeriodic=off  Frequencies=[]  VectorFormat=inherit  Unit=m  AffineConversion=off
  pc_YDot : nesl_utility/PS-Simulink Converter  PhysicalDomain=network_engine_domain  SubClassName=ps_output  LeftPortType=input  RightPortType=output  PseudoPeriodic=off  Frequencies=[]  VectorFormat=inherit  Unit=m/s  AffineConversion=off
  pelvis : Subsystem
  pk_L_ankle_pitch : Product
  pk_L_hip_pitch : Product
  pk_L_knee : Product
  pk_R_ankle_pitch : Product
  pk_R_hip_pitch : Product
  pk_R_knee : Product
  pref : FromWorkspace  VariableName=pref  OutputAfterFinalValue=Holding final value
  pref_demux : Demux
  ps_X : sm_lib/Frames and Transforms/Transform Sensor  MeasurementFrame=World  RotationSequence=XYX  SenseAngle=off  SenseAxis=off  SenseQ=off  SenseR=off  SenseRotationSequence=off  SenseOmegaX=off  SenseOmegaY=off  SenseOmegaZ=off  SenseOmega=off  SenseQDot=off  SenseRDot=off  SenseRotationSequenceDot=off  SenseAlphaX=off  SenseAlphaY=off  SenseAlphaZ=off  SenseAlpha=off  SenseQDDot=off  SenseRDDot=off  SenseX=on  SenseY=off  SenseZ=off  SenseXYZ=off  SenseRad=off  SenseAzim=off  SenseDist=off  SenseInc=off  SenseXDot=off  SenseYDot=off  SenseZDot=off  SenseXYZDot=off  SenseRadDot=off  SenseAzimDot=off  SenseDistDot=off  SenseIncDot=off  SenseXDDot=off  SenseYDDot=off  SenseZDDot=off  SenseXYZDDot=off  SenseRadDDot=off  SenseAzimDDot=off  SenseDistDDot=off  SenseIncDDot=off
  ps_XDot : sm_lib/Frames and Transforms/Transform Sensor  MeasurementFrame=World  RotationSequence=XYX  SenseAngle=off  SenseAxis=off  SenseQ=off  SenseR=off  SenseRotationSequence=off  SenseOmegaX=off  SenseOmegaY=off  SenseOmegaZ=off  SenseOmega=off  SenseQDot=off  SenseRDot=off  SenseRotationSequenceDot=off  SenseAlphaX=off  SenseAlphaY=off  SenseAlphaZ=off  SenseAlpha=off  SenseQDDot=off  SenseRDDot=off  SenseX=off  SenseY=off  SenseZ=off  SenseXYZ=off  SenseRad=off  SenseAzim=off  SenseDist=off  SenseInc=off  SenseXDot=on  SenseYDot=off  SenseZDot=off  SenseXYZDot=off  SenseRadDot=off  SenseAzimDot=off  SenseDistDot=off  SenseIncDot=off  SenseXDDot=off  SenseYDDot=off  SenseZDDot=off  SenseXYZDDot=off  SenseRadDDot=off  SenseAzimDDot=off  SenseDistDDot=off  SenseIncDDot=off
  ps_Y : sm_lib/Frames and Transforms/Transform Sensor  MeasurementFrame=World  RotationSequence=XYX  SenseAngle=off  SenseAxis=off  SenseQ=off  SenseR=off  SenseRotationSequence=off  SenseOmegaX=off  SenseOmegaY=off  SenseOmegaZ=off  SenseOmega=off  SenseQDot=off  SenseRDot=off  SenseRotationSequenceDot=off  SenseAlphaX=off  SenseAlphaY=off  SenseAlphaZ=off  SenseAlpha=off  SenseQDDot=off  SenseRDDot=off  SenseX=off  SenseY=on  SenseZ=off  SenseXYZ=off  SenseRad=off  SenseAzim=off  SenseDist=off  SenseInc=off  SenseXDot=off  SenseYDot=off  SenseZDot=off  SenseXYZDot=off  SenseRadDot=off  SenseAzimDot=off  SenseDistDot=off  SenseIncDot=off  SenseXDDot=off  SenseYDDot=off  SenseZDDot=off  SenseXYZDDot=off  SenseRadDDot=off  SenseAzimDDot=off  SenseDistDDot=off  SenseIncDDot=off
  ps_YDot : sm_lib/Frames and Transforms/Transform Sensor  MeasurementFrame=World  RotationSequence=XYX  SenseAngle=off  SenseAxis=off  SenseQ=off  SenseR=off  SenseRotationSequence=off  SenseOmegaX=off  SenseOmegaY=off  SenseOmegaZ=off  SenseOmega=off  SenseQDot=off  SenseRDot=off  SenseRotationSequenceDot=off  SenseAlphaX=off  SenseAlphaY=off  SenseAlphaZ=off  SenseAlpha=off  SenseQDDot=off  SenseRDDot=off  SenseX=off  SenseY=off  SenseZ=off  SenseXYZ=off  SenseRad=off  SenseAzim=off  SenseDist=off  SenseInc=off  SenseXDot=off  SenseYDot=on  SenseZDot=off  SenseXYZDot=off  SenseRadDot=off  SenseAzimDot=off  SenseDistDot=off  SenseIncDot=off  SenseXDDot=off  SenseYDDot=off  SenseZDDot=off  SenseXYZDDot=off  SenseRadDDot=off  SenseAzimDDot=off  SenseDistDDot=off  SenseIncDDot=off
  qref : FromWorkspace  VariableName=qref  OutputAfterFinalValue=Holding final value
  qref_demux : Demux  Outputs=70
  sat_L_ankle_pitch : Saturate  UpperLimit=1  LowerLimit=0
  sat_L_ankle_roll : Saturate  UpperLimit=1  LowerLimit=0
  sat_L_clavicle : Saturate  UpperLimit=1  LowerLimit=0
  sat_L_elbow : Saturate  UpperLimit=1  LowerLimit=0
  sat_L_forearm_twist : Saturate  UpperLimit=1  LowerLimit=0
  sat_L_hip_pitch : Saturate  UpperLimit=1  LowerLimit=0
  sat_L_hip_roll : Saturate  UpperLimit=1  LowerLimit=0
  sat_L_hip_yaw : Saturate  UpperLimit=1  LowerLimit=0
  sat_L_index1 : Saturate  UpperLimit=1  LowerLimit=0
  sat_L_index2 : Saturate  UpperLimit=1  LowerLimit=0
  sat_L_index3 : Saturate  UpperLimit=1  LowerLimit=0
  sat_L_knee : Saturate  UpperLimit=1  LowerLimit=0
  sat_L_little1 : Saturate  UpperLimit=1  LowerLimit=0
  sat_L_little2 : Saturate  UpperLimit=1  LowerLimit=0
  sat_L_little3 : Saturate  UpperLimit=1  LowerLimit=0
  sat_L_middle1 : Saturate  UpperLimit=1  LowerLimit=0
  sat_L_middle2 : Saturate  UpperLimit=1  LowerLimit=0
  sat_L_middle3 : Saturate  UpperLimit=1  LowerLimit=0
  sat_L_ring1 : Saturate  UpperLimit=1  LowerLimit=0
  sat_L_ring2 : Saturate  UpperLimit=1  LowerLimit=0
  sat_L_ring3 : Saturate  UpperLimit=1  LowerLimit=0
  sat_L_scapula : Saturate  UpperLimit=1  LowerLimit=0
  sat_L_shoulder_pitch : Saturate  UpperLimit=1  LowerLimit=0
  sat_L_shoulder_roll : Saturate  UpperLimit=1  LowerLimit=0
  sat_L_shoulder_yaw : Saturate  UpperLimit=1  LowerLimit=0
  sat_L_thumb1 : Saturate  UpperLimit=1  LowerLimit=0
  sat_L_thumb2 : Saturate  UpperLimit=1  LowerLimit=0
  sat_L_thumb3 : Saturate  UpperLimit=1  LowerLimit=0
  sat_L_toe : Saturate  UpperLimit=1  LowerLimit=0
  sat_L_wrist_pitch : Saturate  UpperLimit=1  LowerLimit=0
  sat_L_wrist_roll : Saturate  UpperLimit=1  LowerLimit=0
  sat_L_wrist_yaw : Saturate  UpperLimit=1  LowerLimit=0
  sat_R_ankle_pitch : Saturate  UpperLimit=1  LowerLimit=0
  sat_R_ankle_roll : Saturate  UpperLimit=1  LowerLimit=0
  sat_R_clavicle : Saturate  UpperLimit=1  LowerLimit=0
  sat_R_elbow : Saturate  UpperLimit=1  LowerLimit=0
  sat_R_forearm_twist : Saturate  UpperLimit=1  LowerLimit=0
  sat_R_hip_pitch : Saturate  UpperLimit=1  LowerLimit=0
  sat_R_hip_roll : Saturate  UpperLimit=1  LowerLimit=0
  sat_R_hip_yaw : Saturate  UpperLimit=1  LowerLimit=0
  sat_R_index1 : Saturate  UpperLimit=1  LowerLimit=0
  sat_R_index2 : Saturate  UpperLimit=1  LowerLimit=0
  sat_R_index3 : Saturate  UpperLimit=1  LowerLimit=0
  sat_R_knee : Saturate  UpperLimit=1  LowerLimit=0
  sat_R_little1 : Saturate  UpperLimit=1  LowerLimit=0
  sat_R_little2 : Saturate  UpperLimit=1  LowerLimit=0
  sat_R_little3 : Saturate  UpperLimit=1  LowerLimit=0
  sat_R_middle1 : Saturate  UpperLimit=1  LowerLimit=0
  sat_R_middle2 : Saturate  UpperLimit=1  LowerLimit=0
  sat_R_middle3 : Saturate  UpperLimit=1  LowerLimit=0
  sat_R_ring1 : Saturate  UpperLimit=1  LowerLimit=0
  sat_R_ring2 : Saturate  UpperLimit=1  LowerLimit=0
  sat_R_ring3 : Saturate  UpperLimit=1  LowerLimit=0
  sat_R_scapula : Saturate  UpperLimit=1  LowerLimit=0
  sat_R_shoulder_pitch : Saturate  UpperLimit=1  LowerLimit=0
  sat_R_shoulder_roll : Saturate  UpperLimit=1  LowerLimit=0
  sat_R_shoulder_yaw : Saturate  UpperLimit=1  LowerLimit=0
  sat_R_thumb1 : Saturate  UpperLimit=1  LowerLimit=0
  sat_R_thumb2 : Saturate  UpperLimit=1  LowerLimit=0
  sat_R_thumb3 : Saturate  UpperLimit=1  LowerLimit=0
  sat_R_toe : Saturate  UpperLimit=1  LowerLimit=0
  sat_R_wrist_pitch : Saturate  UpperLimit=1  LowerLimit=0
  sat_R_wrist_roll : Saturate  UpperLimit=1  LowerLimit=0
  sat_R_wrist_yaw : Saturate  UpperLimit=1  LowerLimit=0
  sat_neck_pitch : Saturate  UpperLimit=1  LowerLimit=0
  sat_neck_roll : Saturate  UpperLimit=1  LowerLimit=0
  sat_neck_yaw : Saturate  UpperLimit=1  LowerLimit=0
  sat_waist_pitch : Saturate  UpperLimit=1  LowerLimit=0
  sat_waist_roll : Saturate  UpperLimit=1  LowerLimit=0
  sat_waist_yaw : Saturate  UpperLimit=1  LowerLimit=0
  sch_b_L : Bias  Bias=1  SaturateOnIntegerOverflow=off
  sch_b_R : Bias  Bias=1  SaturateOnIntegerOverflow=off
  sch_g_L : Gain  Gain=Ksw-1
  sch_g_R : Gain  Gain=Ksw-1
  st_gv : Gain  Gain=0.3052
  st_k : Gain  Gain=-Kstep/0.72
  st_n_L : Gain  Gain=-1
  st_n_R : Gain  Gain=-1
  st_pm_L : Product
  st_pm_R : Product
  st_sat : Saturate  UpperLimit=0.25  LowerLimit=-0.25
  st_xi : Sum
  swing : FromWorkspace  VariableName=swing  OutputAfterFinalValue=Holding final value
  swing_demux : Demux  Outputs=2
  tau_log : ToWorkspace  VariableName=tau_log  SampleTime=-1
  tau_mux : Mux  Inputs=70
  tauff : FromWorkspace  VariableName=tauff  OutputAfterFinalValue=Holding final value
  tauff_demux : Demux  Outputs=70
  torso : Subsystem
  waist_pitch : sm_lib/Joints/Revolute Joint  JointMode=Normal  CompositeWrenchDir=FollowerOnBase  CompositeWrenchFrame=BaseFrame  SenseConstraintForce=off  SenseConstraintTorque=off  SenseTotalForce=off  SenseTotalTorque=off  PositionTargetSpecify=on  PositionTargetPriority=High  PositionTargetValue=0  PositionTargetValueUnits=rad  VelocityTargetSpecify=off  VelocityTargetPriority=High  VelocityTargetValue=0  VelocityTargetValueUnits=deg/s  EquilibriumPosition=0  EquilibriumPositionUnits=deg  SpringStiffness=0  SpringStiffnessUnits=N*m/deg  DampingCoefficient=0.3  DampingCoefficientUnits=kg*m^2/(rad*s)  LowerLimitSpecify=on  LowerLimitBound=-0.5235987755982988  LowerLimitBoundUnits=rad  LowerLimitStiffness=1e4  LowerLimitStiffnessUnits=N*m/deg  LowerLimitDamping=10  LowerLimitDampingUnits=N*m/(deg/s)  LowerLimitTransitionRegionWidth=0.1  LowerLimitTransitionRegionWidthUnits=deg  UpperLimitSpecify=on  UpperLimitBound=0.7853981633974483  UpperLimitBoundUnits=rad  UpperLimitStiffness=1e4  UpperLimitStiffnessUnits=N*m/deg  UpperLimitDamping=10  UpperLimitDampingUnits=N*m/(deg/s)  UpperLimitTransitionRegionWidth=0.1  UpperLimitTransitionRegionWidthUnits=deg  TorqueActuationMode=InputTorque  MotionActuationMode=ComputedMotion  SensePosition=on  SenseVelocity=on  SenseAcceleration=off  SenseTorqueForce=off  SenseLowerLimitTorqueForce=off  SenseUpperLimitTorqueForce=off
  waist_roll : sm_lib/Joints/Revolute Joint  JointMode=Normal  CompositeWrenchDir=FollowerOnBase  CompositeWrenchFrame=BaseFrame  SenseConstraintForce=off  SenseConstraintTorque=off  SenseTotalForce=off  SenseTotalTorque=off  PositionTargetSpecify=on  PositionTargetPriority=High  PositionTargetValue=0  PositionTargetValueUnits=rad  VelocityTargetSpecify=off  VelocityTargetPriority=High  VelocityTargetValue=0  VelocityTargetValueUnits=deg/s  EquilibriumPosition=0  EquilibriumPositionUnits=deg  SpringStiffness=0  SpringStiffnessUnits=N*m/deg  DampingCoefficient=0.3  DampingCoefficientUnits=kg*m^2/(rad*s)  LowerLimitSpecify=on  LowerLimitBound=-0.3490658503988659  LowerLimitBoundUnits=rad  LowerLimitStiffness=1e4  LowerLimitStiffnessUnits=N*m/deg  LowerLimitDamping=10  LowerLimitDampingUnits=N*m/(deg/s)  LowerLimitTransitionRegionWidth=0.1  LowerLimitTransitionRegionWidthUnits=deg  UpperLimitSpecify=on  UpperLimitBound=0.3490658503988659  UpperLimitBoundUnits=rad  UpperLimitStiffness=1e4  UpperLimitStiffnessUnits=N*m/deg  UpperLimitDamping=10  UpperLimitDampingUnits=N*m/(deg/s)  UpperLimitTransitionRegionWidth=0.1  UpperLimitTransitionRegionWidthUnits=deg  TorqueActuationMode=InputTorque  MotionActuationMode=ComputedMotion  SensePosition=on  SenseVelocity=on  SenseAcceleration=off  SenseTorqueForce=off  SenseLowerLimitTorqueForce=off  SenseUpperLimitTorqueForce=off
  waist_roll1 : Subsystem
  waist_yaw : sm_lib/Joints/Revolute Joint  JointMode=Normal  CompositeWrenchDir=FollowerOnBase  CompositeWrenchFrame=BaseFrame  SenseConstraintForce=off  SenseConstraintTorque=off  SenseTotalForce=off  SenseTotalTorque=off  PositionTargetSpecify=on  PositionTargetPriority=High  PositionTargetValue=0  PositionTargetValueUnits=rad  VelocityTargetSpecify=off  VelocityTargetPriority=High  VelocityTargetValue=0  VelocityTargetValueUnits=deg/s  EquilibriumPosition=0  EquilibriumPositionUnits=deg  SpringStiffness=0  SpringStiffnessUnits=N*m/deg  DampingCoefficient=0.3  DampingCoefficientUnits=kg*m^2/(rad*s)  LowerLimitSpecify=on  LowerLimitBound=-1.047197551196598  LowerLimitBoundUnits=rad  LowerLimitStiffness=1e4  LowerLimitStiffnessUnits=N*m/deg  LowerLimitDamping=10  LowerLimitDampingUnits=N*m/(deg/s)  LowerLimitTransitionRegionWidth=0.1  LowerLimitTransitionRegionWidthUnits=deg  UpperLimitSpecify=on  UpperLimitBound=1.047197551196598  UpperLimitBoundUnits=rad  UpperLimitStiffness=1e4  UpperLimitStiffnessUnits=N*m/deg  UpperLimitDamping=10  UpperLimitDampingUnits=N*m/(deg/s)  UpperLimitTransitionRegionWidth=0.1  UpperLimitTransitionRegionWidthUnits=deg  TorqueActuationMode=InputTorque  MotionActuationMode=ComputedMotion  SensePosition=on  SenseVelocity=on  SenseAcceleration=off  SenseTorqueForce=off  SenseLowerLimitTorqueForce=off  SenseUpperLimitTorqueForce=off
  waist_yaw1 : Subsystem
  wires:
  [qr_L_ankle_pitch] -> S_L_ankle_pitch/1
  cq_L_ankle_pitch/1 -> S_L_ankle_pitch/2
  [dq_L_ankle_pitch] -> S_L_ankle_pitch/3
  S_L_ankle_pitch/1 -> K_L_ankle_pitch/1
  cw_L_ankle_pitch/1 -> B_L_ankle_pitch/1, abs_L_ankle_pitch/1
  K_L_ankle_pitch/1 -> pk_L_ankle_pitch/1
  [sch_L] -> pk_L_ankle_pitch/2
  pk_L_ankle_pitch/1 -> T_L_ankle_pitch/1
  B_L_ankle_pitch/1 -> pb_L_ankle_pitch/1
  [sch_L] -> pb_L_ankle_pitch/2
  pb_L_ankle_pitch/1 -> T_L_ankle_pitch/2
  [tf_L_ankle_pitch] -> T_L_ankle_pitch/3
  [fb_L_ankle_pitch] -> T_L_ankle_pitch/4
  abs_L_ankle_pitch/1 -> gw_L_ankle_pitch/1
  gw_L_ankle_pitch/1 -> bi_L_ankle_pitch/1
  bi_L_ankle_pitch/1 -> sat_L_ankle_pitch/1
  sat_L_ankle_pitch/1 -> gT_L_ankle_pitch/1
  gT_L_ankle_pitch/1 -> gn_L_ankle_pitch/1, mn_L_ankle_pitch/2
  T_L_ankle_pitch/1 -> mn_L_ankle_pitch/1
  mn_L_ankle_pitch/1 -> mx_L_ankle_pitch/1
  gn_L_ankle_pitch/1 -> mx_L_ankle_pitch/2
  mx_L_ankle_pitch/1 -> ct_L_ankle_pitch/1, tau_mux/1
  [qr_L_ankle_roll] -> S_L_ankle_roll/1
  cq_L_ankle_roll/1 -> S_L_ankle_roll/2
  S_L_ankle_roll/1 -> K_L_ankle_roll/1
  cw_L_ankle_roll/1 -> B_L_ankle_roll/1, abs_L_ankle_roll/1
  K_L_ankle_roll/1 -> T_L_ankle_roll/1
  B_L_ankle_roll/1 -> T_L_ankle_roll/2
  [tf_L_ankle_roll] -> T_L_ankle_roll/3
  [fb_L_ankle_roll] -> T_L_ankle_roll/4
  abs_L_ankle_roll/1 -> gw_L_ankle_roll/1
  gw_L_ankle_roll/1 -> bi_L_ankle_roll/1
  bi_L_ankle_roll/1 -> sat_L_ankle_roll/1
  sat_L_ankle_roll/1 -> gT_L_ankle_roll/1
  gT_L_ankle_roll/1 -> gn_L_ankle_roll/1, mn_L_ankle_roll/2
  T_L_ankle_roll/1 -> mn_L_ankle_roll/1
  mn_L_ankle_roll/1 -> mx_L_ankle_roll/1
  gn_L_ankle_roll/1 -> mx_L_ankle_roll/2
  mx_L_ankle_roll/1 -> ct_L_ankle_roll/1, tau_mux/2
  [qr_L_clavicle] -> S_L_clavicle/1
  cq_L_clavicle/1 -> S_L_clavicle/2
  S_L_clavicle/1 -> K_L_clavicle/1
  cw_L_clavicle/1 -> B_L_clavicle/1, abs_L_clavicle/1
  K_L_clavicle/1 -> T_L_clavicle/1
  B_L_clavicle/1 -> T_L_clavicle/2
  [tf_L_clavicle] -> T_L_clavicle/3
  abs_L_clavicle/1 -> gw_L_clavicle/1
  gw_L_clavicle/1 -> bi_L_clavicle/1
  bi_L_clavicle/1 -> sat_L_clavicle/1
  sat_L_clavicle/1 -> gT_L_clavicle/1
  gT_L_clavicle/1 -> gn_L_clavicle/1, mn_L_clavicle/2
  T_L_clavicle/1 -> mn_L_clavicle/1
  mn_L_clavicle/1 -> mx_L_clavicle/1
  gn_L_clavicle/1 -> mx_L_clavicle/2
  mx_L_clavicle/1 -> ct_L_clavicle/1, tau_mux/3
  [qr_L_elbow] -> S_L_elbow/1
  cq_L_elbow/1 -> S_L_elbow/2
  S_L_elbow/1 -> K_L_elbow/1
  cw_L_elbow/1 -> B_L_elbow/1, abs_L_elbow/1
  K_L_elbow/1 -> T_L_elbow/1
  B_L_elbow/1 -> T_L_elbow/2
  [tf_L_elbow] -> T_L_elbow/3
  abs_L_elbow/1 -> gw_L_elbow/1
  gw_L_elbow/1 -> bi_L_elbow/1
  bi_L_elbow/1 -> sat_L_elbow/1
  sat_L_elbow/1 -> gT_L_elbow/1
  gT_L_elbow/1 -> gn_L_elbow/1, mn_L_elbow/2
  T_L_elbow/1 -> mn_L_elbow/1
  mn_L_elbow/1 -> mx_L_elbow/1
  gn_L_elbow/1 -> mx_L_elbow/2
  mx_L_elbow/1 -> ct_L_elbow/1, tau_mux/4
  [qr_L_forearm_twist] -> S_L_forearm_twist/1
  cq_L_forearm_twist/1 -> S_L_forearm_twist/2
  S_L_forearm_twist/1 -> K_L_forearm_twist/1
  cw_L_forearm_twist/1 -> B_L_forearm_twist/1, abs_L_forearm_twist/1
  K_L_forearm_twist/1 -> T_L_forearm_twist/1
  B_L_forearm_twist/1 -> T_L_forearm_twist/2
  [tf_L_forearm_twist] -> T_L_forearm_twist/3
  abs_L_forearm_twist/1 -> gw_L_forearm_twist/1
  gw_L_forearm_twist/1 -> bi_L_forearm_twist/1
  bi_L_forearm_twist/1 -> sat_L_forearm_twist/1
  sat_L_forearm_twist/1 -> gT_L_forearm_twist/1
  gT_L_forearm_twist/1 -> gn_L_forearm_twist/1, mn_L_forearm_twist/2
  T_L_forearm_twist/1 -> mn_L_forearm_twist/1
  mn_L_forearm_twist/1 -> mx_L_forearm_twist/1
  gn_L_forearm_twist/1 -> mx_L_forearm_twist/2
  mx_L_forearm_twist/1 -> ct_L_forearm_twist/1, tau_mux/5
  [qr_L_hip_pitch] -> S_L_hip_pitch/1
  cq_L_hip_pitch/1 -> S_L_hip_pitch/2
  [dq_L_hip_pitch] -> S_L_hip_pitch/3
  S_L_hip_pitch/1 -> K_L_hip_pitch/1
  cw_L_hip_pitch/1 -> B_L_hip_pitch/1, abs_L_hip_pitch/1
  K_L_hip_pitch/1 -> pk_L_hip_pitch/1
  [sch_L] -> pk_L_hip_pitch/2
  pk_L_hip_pitch/1 -> T_L_hip_pitch/1
  B_L_hip_pitch/1 -> pb_L_hip_pitch/1
  [sch_L] -> pb_L_hip_pitch/2
  pb_L_hip_pitch/1 -> T_L_hip_pitch/2
  [tf_L_hip_pitch] -> T_L_hip_pitch/3
  abs_L_hip_pitch/1 -> gw_L_hip_pitch/1
  gw_L_hip_pitch/1 -> bi_L_hip_pitch/1
  bi_L_hip_pitch/1 -> sat_L_hip_pitch/1
  sat_L_hip_pitch/1 -> gT_L_hip_pitch/1
  gT_L_hip_pitch/1 -> gn_L_hip_pitch/1, mn_L_hip_pitch/2
  T_L_hip_pitch/1 -> mn_L_hip_pitch/1
  mn_L_hip_pitch/1 -> mx_L_hip_pitch/1
  gn_L_hip_pitch/1 -> mx_L_hip_pitch/2
  mx_L_hip_pitch/1 -> ct_L_hip_pitch/1, tau_mux/6
  [qr_L_hip_roll] -> S_L_hip_roll/1
  cq_L_hip_roll/1 -> S_L_hip_roll/2
  S_L_hip_roll/1 -> K_L_hip_roll/1
  cw_L_hip_roll/1 -> B_L_hip_roll/1, abs_L_hip_roll/1
  K_L_hip_roll/1 -> T_L_hip_roll/1
  B_L_hip_roll/1 -> T_L_hip_roll/2
  [tf_L_hip_roll] -> T_L_hip_roll/3
  abs_L_hip_roll/1 -> gw_L_hip_roll/1
  gw_L_hip_roll/1 -> bi_L_hip_roll/1
  bi_L_hip_roll/1 -> sat_L_hip_roll/1
  sat_L_hip_roll/1 -> gT_L_hip_roll/1
  gT_L_hip_roll/1 -> gn_L_hip_roll/1, mn_L_hip_roll/2
  T_L_hip_roll/1 -> mn_L_hip_roll/1
  mn_L_hip_roll/1 -> mx_L_hip_roll/1
  gn_L_hip_roll/1 -> mx_L_hip_roll/2
  mx_L_hip_roll/1 -> ct_L_hip_roll/1, tau_mux/7
  [qr_L_hip_yaw] -> S_L_hip_yaw/1
  cq_L_hip_yaw/1 -> S_L_hip_yaw/2
  S_L_hip_yaw/1 -> K_L_hip_yaw/1
  cw_L_hip_yaw/1 -> B_L_hip_yaw/1, abs_L_hip_yaw/1
  K_L_hip_yaw/1 -> T_L_hip_yaw/1
  B_L_hip_yaw/1 -> T_L_hip_yaw/2
  [tf_L_hip_yaw] -> T_L_hip_yaw/3
  abs_L_hip_yaw/1 -> gw_L_hip_yaw/1
  gw_L_hip_yaw/1 -> bi_L_hip_yaw/1
  bi_L_hip_yaw/1 -> sat_L_hip_yaw/1
  sat_L_hip_yaw/1 -> gT_L_hip_yaw/1
  gT_L_hip_yaw/1 -> gn_L_hip_yaw/1, mn_L_hip_yaw/2
  T_L_hip_yaw/1 -> mn_L_hip_yaw/1
  mn_L_hip_yaw/1 -> mx_L_hip_yaw/1
  gn_L_hip_yaw/1 -> mx_L_hip_yaw/2
  mx_L_hip_yaw/1 -> ct_L_hip_yaw/1, tau_mux/8
  [qr_L_index1] -> S_L_index1/1
  cq_L_index1/1 -> S_L_index1/2
  S_L_index1/1 -> K_L_index1/1
  cw_L_index1/1 -> B_L_index1/1, abs_L_index1/1
  K_L_index1/1 -> T_L_index1/1
  B_L_index1/1 -> T_L_index1/2
  [tf_L_index1] -> T_L_index1/3
  abs_L_index1/1 -> gw_L_index1/1
  gw_L_index1/1 -> bi_L_index1/1
  bi_L_index1/1 -> sat_L_index1/1
  sat_L_index1/1 -> gT_L_index1/1
  gT_L_index1/1 -> gn_L_index1/1, mn_L_index1/2
  T_L_index1/1 -> mn_L_index1/1
  mn_L_index1/1 -> mx_L_index1/1
  gn_L_index1/1 -> mx_L_index1/2
  mx_L_index1/1 -> ct_L_index1/1, tau_mux/9
  [qr_L_index2] -> S_L_index2/1
  cq_L_index2/1 -> S_L_index2/2
  S_L_index2/1 -> K_L_index2/1
  cw_L_index2/1 -> B_L_index2/1, abs_L_index2/1
  K_L_index2/1 -> T_L_index2/1
  B_L_index2/1 -> T_L_index2/2
  [tf_L_index2] -> T_L_index2/3
  abs_L_index2/1 -> gw_L_index2/1
  gw_L_index2/1 -> bi_L_index2/1
  bi_L_index2/1 -> sat_L_index2/1
  sat_L_index2/1 -> gT_L_index2/1
  gT_L_index2/1 -> gn_L_index2/1, mn_L_index2/2
  T_L_index2/1 -> mn_L_index2/1
  mn_L_index2/1 -> mx_L_index2/1
  gn_L_index2/1 -> mx_L_index2/2
  mx_L_index2/1 -> ct_L_index2/1, tau_mux/10
  [qr_L_index3] -> S_L_index3/1
  cq_L_index3/1 -> S_L_index3/2
  S_L_index3/1 -> K_L_index3/1
  cw_L_index3/1 -> B_L_index3/1, abs_L_index3/1
  K_L_index3/1 -> T_L_index3/1
  B_L_index3/1 -> T_L_index3/2
  [tf_L_index3] -> T_L_index3/3
  abs_L_index3/1 -> gw_L_index3/1
  gw_L_index3/1 -> bi_L_index3/1
  bi_L_index3/1 -> sat_L_index3/1
  sat_L_index3/1 -> gT_L_index3/1
  gT_L_index3/1 -> gn_L_index3/1, mn_L_index3/2
  T_L_index3/1 -> mn_L_index3/1
  mn_L_index3/1 -> mx_L_index3/1
  gn_L_index3/1 -> mx_L_index3/2
  mx_L_index3/1 -> ct_L_index3/1, tau_mux/11
  [qr_L_knee] -> S_L_knee/1
  cq_L_knee/1 -> S_L_knee/2
  S_L_knee/1 -> K_L_knee/1
  cw_L_knee/1 -> B_L_knee/1, abs_L_knee/1
  K_L_knee/1 -> pk_L_knee/1
  [sch_L] -> pk_L_knee/2
  pk_L_knee/1 -> T_L_knee/1
  B_L_knee/1 -> pb_L_knee/1
  [sch_L] -> pb_L_knee/2
  pb_L_knee/1 -> T_L_knee/2
  [tf_L_knee] -> T_L_knee/3
  abs_L_knee/1 -> gw_L_knee/1
  gw_L_knee/1 -> bi_L_knee/1
  bi_L_knee/1 -> sat_L_knee/1
  sat_L_knee/1 -> gT_L_knee/1
  gT_L_knee/1 -> gn_L_knee/1, mn_L_knee/2
  T_L_knee/1 -> mn_L_knee/1
  mn_L_knee/1 -> mx_L_knee/1
  gn_L_knee/1 -> mx_L_knee/2
  mx_L_knee/1 -> ct_L_knee/1, tau_mux/12
  [qr_L_little1] -> S_L_little1/1
  cq_L_little1/1 -> S_L_little1/2
  S_L_little1/1 -> K_L_little1/1
  cw_L_little1/1 -> B_L_little1/1, abs_L_little1/1
  K_L_little1/1 -> T_L_little1/1
  B_L_little1/1 -> T_L_little1/2
  [tf_L_little1] -> T_L_little1/3
  abs_L_little1/1 -> gw_L_little1/1
  gw_L_little1/1 -> bi_L_little1/1
  bi_L_little1/1 -> sat_L_little1/1
  sat_L_little1/1 -> gT_L_little1/1
  gT_L_little1/1 -> gn_L_little1/1, mn_L_little1/2
  T_L_little1/1 -> mn_L_little1/1
  mn_L_little1/1 -> mx_L_little1/1
  gn_L_little1/1 -> mx_L_little1/2
  mx_L_little1/1 -> ct_L_little1/1, tau_mux/13
  [qr_L_little2] -> S_L_little2/1
  cq_L_little2/1 -> S_L_little2/2
  S_L_little2/1 -> K_L_little2/1
  cw_L_little2/1 -> B_L_little2/1, abs_L_little2/1
  K_L_little2/1 -> T_L_little2/1
  B_L_little2/1 -> T_L_little2/2
  [tf_L_little2] -> T_L_little2/3
  abs_L_little2/1 -> gw_L_little2/1
  gw_L_little2/1 -> bi_L_little2/1
  bi_L_little2/1 -> sat_L_little2/1
  sat_L_little2/1 -> gT_L_little2/1
  gT_L_little2/1 -> gn_L_little2/1, mn_L_little2/2
  T_L_little2/1 -> mn_L_little2/1
  mn_L_little2/1 -> mx_L_little2/1
  gn_L_little2/1 -> mx_L_little2/2
  mx_L_little2/1 -> ct_L_little2/1, tau_mux/14
  [qr_L_little3] -> S_L_little3/1
  cq_L_little3/1 -> S_L_little3/2
  S_L_little3/1 -> K_L_little3/1
  cw_L_little3/1 -> B_L_little3/1, abs_L_little3/1
  K_L_little3/1 -> T_L_little3/1
  B_L_little3/1 -> T_L_little3/2
  [tf_L_little3] -> T_L_little3/3
  abs_L_little3/1 -> gw_L_little3/1
  gw_L_little3/1 -> bi_L_little3/1
  bi_L_little3/1 -> sat_L_little3/1
  sat_L_little3/1 -> gT_L_little3/1
  gT_L_little3/1 -> gn_L_little3/1, mn_L_little3/2
  T_L_little3/1 -> mn_L_little3/1
  mn_L_little3/1 -> mx_L_little3/1
  gn_L_little3/1 -> mx_L_little3/2
  mx_L_little3/1 -> ct_L_little3/1, tau_mux/15
  [qr_L_middle1] -> S_L_middle1/1
  cq_L_middle1/1 -> S_L_middle1/2
  S_L_middle1/1 -> K_L_middle1/1
  cw_L_middle1/1 -> B_L_middle1/1, abs_L_middle1/1
  K_L_middle1/1 -> T_L_middle1/1
  B_L_middle1/1 -> T_L_middle1/2
  [tf_L_middle1] -> T_L_middle1/3
  abs_L_middle1/1 -> gw_L_middle1/1
  gw_L_middle1/1 -> bi_L_middle1/1
  bi_L_middle1/1 -> sat_L_middle1/1
  sat_L_middle1/1 -> gT_L_middle1/1
  gT_L_middle1/1 -> gn_L_middle1/1, mn_L_middle1/2
  T_L_middle1/1 -> mn_L_middle1/1
  mn_L_middle1/1 -> mx_L_middle1/1
  gn_L_middle1/1 -> mx_L_middle1/2
  mx_L_middle1/1 -> ct_L_middle1/1, tau_mux/16
  [qr_L_middle2] -> S_L_middle2/1
  cq_L_middle2/1 -> S_L_middle2/2
  S_L_middle2/1 -> K_L_middle2/1
  cw_L_middle2/1 -> B_L_middle2/1, abs_L_middle2/1
  K_L_middle2/1 -> T_L_middle2/1
  B_L_middle2/1 -> T_L_middle2/2
  [tf_L_middle2] -> T_L_middle2/3
  abs_L_middle2/1 -> gw_L_middle2/1
  gw_L_middle2/1 -> bi_L_middle2/1
  bi_L_middle2/1 -> sat_L_middle2/1
  sat_L_middle2/1 -> gT_L_middle2/1
  gT_L_middle2/1 -> gn_L_middle2/1, mn_L_middle2/2
  T_L_middle2/1 -> mn_L_middle2/1
  mn_L_middle2/1 -> mx_L_middle2/1
  gn_L_middle2/1 -> mx_L_middle2/2
  mx_L_middle2/1 -> ct_L_middle2/1, tau_mux/17
  [qr_L_middle3] -> S_L_middle3/1
  cq_L_middle3/1 -> S_L_middle3/2
  S_L_middle3/1 -> K_L_middle3/1
  cw_L_middle3/1 -> B_L_middle3/1, abs_L_middle3/1
  K_L_middle3/1 -> T_L_middle3/1
  B_L_middle3/1 -> T_L_middle3/2
  [tf_L_middle3] -> T_L_middle3/3
  abs_L_middle3/1 -> gw_L_middle3/1
  gw_L_middle3/1 -> bi_L_middle3/1
  bi_L_middle3/1 -> sat_L_middle3/1
  sat_L_middle3/1 -> gT_L_middle3/1
  gT_L_middle3/1 -> gn_L_middle3/1, mn_L_middle3/2
  T_L_middle3/1 -> mn_L_middle3/1
  mn_L_middle3/1 -> mx_L_middle3/1
  gn_L_middle3/1 -> mx_L_middle3/2
  mx_L_middle3/1 -> ct_L_middle3/1, tau_mux/18
  [qr_L_ring1] -> S_L_ring1/1
  cq_L_ring1/1 -> S_L_ring1/2
  S_L_ring1/1 -> K_L_ring1/1
  cw_L_ring1/1 -> B_L_ring1/1, abs_L_ring1/1
  K_L_ring1/1 -> T_L_ring1/1
  B_L_ring1/1 -> T_L_ring1/2
  [tf_L_ring1] -> T_L_ring1/3
  abs_L_ring1/1 -> gw_L_ring1/1
  gw_L_ring1/1 -> bi_L_ring1/1
  bi_L_ring1/1 -> sat_L_ring1/1
  sat_L_ring1/1 -> gT_L_ring1/1
  gT_L_ring1/1 -> gn_L_ring1/1, mn_L_ring1/2
  T_L_ring1/1 -> mn_L_ring1/1
  mn_L_ring1/1 -> mx_L_ring1/1
  gn_L_ring1/1 -> mx_L_ring1/2
  mx_L_ring1/1 -> ct_L_ring1/1, tau_mux/19
  [qr_L_ring2] -> S_L_ring2/1
  cq_L_ring2/1 -> S_L_ring2/2
  S_L_ring2/1 -> K_L_ring2/1
  cw_L_ring2/1 -> B_L_ring2/1, abs_L_ring2/1
  K_L_ring2/1 -> T_L_ring2/1
  B_L_ring2/1 -> T_L_ring2/2
  [tf_L_ring2] -> T_L_ring2/3
  abs_L_ring2/1 -> gw_L_ring2/1
  gw_L_ring2/1 -> bi_L_ring2/1
  bi_L_ring2/1 -> sat_L_ring2/1
  sat_L_ring2/1 -> gT_L_ring2/1
  gT_L_ring2/1 -> gn_L_ring2/1, mn_L_ring2/2
  T_L_ring2/1 -> mn_L_ring2/1
  mn_L_ring2/1 -> mx_L_ring2/1
  gn_L_ring2/1 -> mx_L_ring2/2
  mx_L_ring2/1 -> ct_L_ring2/1, tau_mux/20
  [qr_L_ring3] -> S_L_ring3/1
  cq_L_ring3/1 -> S_L_ring3/2
  S_L_ring3/1 -> K_L_ring3/1
  cw_L_ring3/1 -> B_L_ring3/1, abs_L_ring3/1
  K_L_ring3/1 -> T_L_ring3/1
  B_L_ring3/1 -> T_L_ring3/2
  [tf_L_ring3] -> T_L_ring3/3
  abs_L_ring3/1 -> gw_L_ring3/1
  gw_L_ring3/1 -> bi_L_ring3/1
  bi_L_ring3/1 -> sat_L_ring3/1
  sat_L_ring3/1 -> gT_L_ring3/1
  gT_L_ring3/1 -> gn_L_ring3/1, mn_L_ring3/2
  T_L_ring3/1 -> mn_L_ring3/1
  mn_L_ring3/1 -> mx_L_ring3/1
  gn_L_ring3/1 -> mx_L_ring3/2
  mx_L_ring3/1 -> ct_L_ring3/1, tau_mux/21
  [qr_L_scapula] -> S_L_scapula/1
  cq_L_scapula/1 -> S_L_scapula/2
  S_L_scapula/1 -> K_L_scapula/1
  cw_L_scapula/1 -> B_L_scapula/1, abs_L_scapula/1
  K_L_scapula/1 -> T_L_scapula/1
  B_L_scapula/1 -> T_L_scapula/2
  [tf_L_scapula] -> T_L_scapula/3
  abs_L_scapula/1 -> gw_L_scapula/1
  gw_L_scapula/1 -> bi_L_scapula/1
  bi_L_scapula/1 -> sat_L_scapula/1
  sat_L_scapula/1 -> gT_L_scapula/1
  gT_L_scapula/1 -> gn_L_scapula/1, mn_L_scapula/2
  T_L_scapula/1 -> mn_L_scapula/1
  mn_L_scapula/1 -> mx_L_scapula/1
  gn_L_scapula/1 -> mx_L_scapula/2
  mx_L_scapula/1 -> ct_L_scapula/1, tau_mux/22
  [qr_L_shoulder_pitch] -> S_L_shoulder_pitch/1
  cq_L_shoulder_pitch/1 -> S_L_shoulder_pitch/2
  S_L_shoulder_pitch/1 -> K_L_shoulder_pitch/1
  cw_L_shoulder_pitch/1 -> B_L_shoulder_pitch/1, abs_L_shoulder_pitch/1
  K_L_shoulder_pitch/1 -> T_L_shoulder_pitch/1
  B_L_shoulder_pitch/1 -> T_L_shoulder_pitch/2
  [tf_L_shoulder_pitch] -> T_L_shoulder_pitch/3
  abs_L_shoulder_pitch/1 -> gw_L_shoulder_pitch/1
  gw_L_shoulder_pitch/1 -> bi_L_shoulder_pitch/1
  bi_L_shoulder_pitch/1 -> sat_L_shoulder_pitch/1
  sat_L_shoulder_pitch/1 -> gT_L_shoulder_pitch/1
  gT_L_shoulder_pitch/1 -> gn_L_shoulder_pitch/1, mn_L_shoulder_pitch/2
  T_L_shoulder_pitch/1 -> mn_L_shoulder_pitch/1
  mn_L_shoulder_pitch/1 -> mx_L_shoulder_pitch/1
  gn_L_shoulder_pitch/1 -> mx_L_shoulder_pitch/2
  mx_L_shoulder_pitch/1 -> ct_L_shoulder_pitch/1, tau_mux/23
  [qr_L_shoulder_roll] -> S_L_shoulder_roll/1
  cq_L_shoulder_roll/1 -> S_L_shoulder_roll/2
  S_L_shoulder_roll/1 -> K_L_shoulder_roll/1
  cw_L_shoulder_roll/1 -> B_L_shoulder_roll/1, abs_L_shoulder_roll/1
  K_L_shoulder_roll/1 -> T_L_shoulder_roll/1
  B_L_shoulder_roll/1 -> T_L_shoulder_roll/2
  [tf_L_shoulder_roll] -> T_L_shoulder_roll/3
  abs_L_shoulder_roll/1 -> gw_L_shoulder_roll/1
  gw_L_shoulder_roll/1 -> bi_L_shoulder_roll/1
  bi_L_shoulder_roll/1 -> sat_L_shoulder_roll/1
  sat_L_shoulder_roll/1 -> gT_L_shoulder_roll/1
  gT_L_shoulder_roll/1 -> gn_L_shoulder_roll/1, mn_L_shoulder_roll/2
  T_L_shoulder_roll/1 -> mn_L_shoulder_roll/1
  mn_L_shoulder_roll/1 -> mx_L_shoulder_roll/1
  gn_L_shoulder_roll/1 -> mx_L_shoulder_roll/2
  mx_L_shoulder_roll/1 -> ct_L_shoulder_roll/1, tau_mux/24
  [qr_L_shoulder_yaw] -> S_L_shoulder_yaw/1
  cq_L_shoulder_yaw/1 -> S_L_shoulder_yaw/2
  S_L_shoulder_yaw/1 -> K_L_shoulder_yaw/1
  cw_L_shoulder_yaw/1 -> B_L_shoulder_yaw/1, abs_L_shoulder_yaw/1
  K_L_shoulder_yaw/1 -> T_L_shoulder_yaw/1
  B_L_shoulder_yaw/1 -> T_L_shoulder_yaw/2
  [tf_L_shoulder_yaw] -> T_L_shoulder_yaw/3
  abs_L_shoulder_yaw/1 -> gw_L_shoulder_yaw/1
  gw_L_shoulder_yaw/1 -> bi_L_shoulder_yaw/1
  bi_L_shoulder_yaw/1 -> sat_L_shoulder_yaw/1
  sat_L_shoulder_yaw/1 -> gT_L_shoulder_yaw/1
  gT_L_shoulder_yaw/1 -> gn_L_shoulder_yaw/1, mn_L_shoulder_yaw/2
  T_L_shoulder_yaw/1 -> mn_L_shoulder_yaw/1
  mn_L_shoulder_yaw/1 -> mx_L_shoulder_yaw/1
  gn_L_shoulder_yaw/1 -> mx_L_shoulder_yaw/2
  mx_L_shoulder_yaw/1 -> ct_L_shoulder_yaw/1, tau_mux/25
  [qr_L_thumb1] -> S_L_thumb1/1
  cq_L_thumb1/1 -> S_L_thumb1/2
  S_L_thumb1/1 -> K_L_thumb1/1
  cw_L_thumb1/1 -> B_L_thumb1/1, abs_L_thumb1/1
  K_L_thumb1/1 -> T_L_thumb1/1
  B_L_thumb1/1 -> T_L_thumb1/2
  [tf_L_thumb1] -> T_L_thumb1/3
  abs_L_thumb1/1 -> gw_L_thumb1/1
  gw_L_thumb1/1 -> bi_L_thumb1/1
  bi_L_thumb1/1 -> sat_L_thumb1/1
  sat_L_thumb1/1 -> gT_L_thumb1/1
  gT_L_thumb1/1 -> gn_L_thumb1/1, mn_L_thumb1/2
  T_L_thumb1/1 -> mn_L_thumb1/1
  mn_L_thumb1/1 -> mx_L_thumb1/1
  gn_L_thumb1/1 -> mx_L_thumb1/2
  mx_L_thumb1/1 -> ct_L_thumb1/1, tau_mux/26
  [qr_L_thumb2] -> S_L_thumb2/1
  cq_L_thumb2/1 -> S_L_thumb2/2
  S_L_thumb2/1 -> K_L_thumb2/1
  cw_L_thumb2/1 -> B_L_thumb2/1, abs_L_thumb2/1
  K_L_thumb2/1 -> T_L_thumb2/1
  B_L_thumb2/1 -> T_L_thumb2/2
  [tf_L_thumb2] -> T_L_thumb2/3
  abs_L_thumb2/1 -> gw_L_thumb2/1
  gw_L_thumb2/1 -> bi_L_thumb2/1
  bi_L_thumb2/1 -> sat_L_thumb2/1
  sat_L_thumb2/1 -> gT_L_thumb2/1
  gT_L_thumb2/1 -> gn_L_thumb2/1, mn_L_thumb2/2
  T_L_thumb2/1 -> mn_L_thumb2/1
  mn_L_thumb2/1 -> mx_L_thumb2/1
  gn_L_thumb2/1 -> mx_L_thumb2/2
  mx_L_thumb2/1 -> ct_L_thumb2/1, tau_mux/27
  [qr_L_thumb3] -> S_L_thumb3/1
  cq_L_thumb3/1 -> S_L_thumb3/2
  S_L_thumb3/1 -> K_L_thumb3/1
  cw_L_thumb3/1 -> B_L_thumb3/1, abs_L_thumb3/1
  K_L_thumb3/1 -> T_L_thumb3/1
  B_L_thumb3/1 -> T_L_thumb3/2
  [tf_L_thumb3] -> T_L_thumb3/3
  abs_L_thumb3/1 -> gw_L_thumb3/1
  gw_L_thumb3/1 -> bi_L_thumb3/1
  bi_L_thumb3/1 -> sat_L_thumb3/1
  sat_L_thumb3/1 -> gT_L_thumb3/1
  gT_L_thumb3/1 -> gn_L_thumb3/1, mn_L_thumb3/2
  T_L_thumb3/1 -> mn_L_thumb3/1
  mn_L_thumb3/1 -> mx_L_thumb3/1
  gn_L_thumb3/1 -> mx_L_thumb3/2
  mx_L_thumb3/1 -> ct_L_thumb3/1, tau_mux/28
  [qr_L_toe] -> S_L_toe/1
  cq_L_toe/1 -> S_L_toe/2
  S_L_toe/1 -> K_L_toe/1
  cw_L_toe/1 -> B_L_toe/1, abs_L_toe/1
  K_L_toe/1 -> T_L_toe/1
  B_L_toe/1 -> T_L_toe/2
  [tf_L_toe] -> T_L_toe/3
  abs_L_toe/1 -> gw_L_toe/1
  gw_L_toe/1 -> bi_L_toe/1
  bi_L_toe/1 -> sat_L_toe/1
  sat_L_toe/1 -> gT_L_toe/1
  gT_L_toe/1 -> gn_L_toe/1, mn_L_toe/2
  T_L_toe/1 -> mn_L_toe/1
  mn_L_toe/1 -> mx_L_toe/1
  gn_L_toe/1 -> mx_L_toe/2
  mx_L_toe/1 -> ct_L_toe/1, tau_mux/29
  [qr_L_wrist_pitch] -> S_L_wrist_pitch/1
  cq_L_wrist_pitch/1 -> S_L_wrist_pitch/2
  S_L_wrist_pitch/1 -> K_L_wrist_pitch/1
  cw_L_wrist_pitch/1 -> B_L_wrist_pitch/1, abs_L_wrist_pitch/1
  K_L_wrist_pitch/1 -> T_L_wrist_pitch/1
  B_L_wrist_pitch/1 -> T_L_wrist_pitch/2
  [tf_L_wrist_pitch] -> T_L_wrist_pitch/3
  abs_L_wrist_pitch/1 -> gw_L_wrist_pitch/1
  gw_L_wrist_pitch/1 -> bi_L_wrist_pitch/1
  bi_L_wrist_pitch/1 -> sat_L_wrist_pitch/1
  sat_L_wrist_pitch/1 -> gT_L_wrist_pitch/1
  gT_L_wrist_pitch/1 -> gn_L_wrist_pitch/1, mn_L_wrist_pitch/2
  T_L_wrist_pitch/1 -> mn_L_wrist_pitch/1
  mn_L_wrist_pitch/1 -> mx_L_wrist_pitch/1
  gn_L_wrist_pitch/1 -> mx_L_wrist_pitch/2
  mx_L_wrist_pitch/1 -> ct_L_wrist_pitch/1, tau_mux/30
  [qr_L_wrist_roll] -> S_L_wrist_roll/1
  cq_L_wrist_roll/1 -> S_L_wrist_roll/2
  S_L_wrist_roll/1 -> K_L_wrist_roll/1
  cw_L_wrist_roll/1 -> B_L_wrist_roll/1, abs_L_wrist_roll/1
  K_L_wrist_roll/1 -> T_L_wrist_roll/1
  B_L_wrist_roll/1 -> T_L_wrist_roll/2
  [tf_L_wrist_roll] -> T_L_wrist_roll/3
  abs_L_wrist_roll/1 -> gw_L_wrist_roll/1
  gw_L_wrist_roll/1 -> bi_L_wrist_roll/1
  bi_L_wrist_roll/1 -> sat_L_wrist_roll/1
  sat_L_wrist_roll/1 -> gT_L_wrist_roll/1
  gT_L_wrist_roll/1 -> gn_L_wrist_roll/1, mn_L_wrist_roll/2
  T_L_wrist_roll/1 -> mn_L_wrist_roll/1
  mn_L_wrist_roll/1 -> mx_L_wrist_roll/1
  gn_L_wrist_roll/1 -> mx_L_wrist_roll/2
  mx_L_wrist_roll/1 -> ct_L_wrist_roll/1, tau_mux/31
  [qr_L_wrist_yaw] -> S_L_wrist_yaw/1
  cq_L_wrist_yaw/1 -> S_L_wrist_yaw/2
  S_L_wrist_yaw/1 -> K_L_wrist_yaw/1
  cw_L_wrist_yaw/1 -> B_L_wrist_yaw/1, abs_L_wrist_yaw/1
  K_L_wrist_yaw/1 -> T_L_wrist_yaw/1
  B_L_wrist_yaw/1 -> T_L_wrist_yaw/2
  [tf_L_wrist_yaw] -> T_L_wrist_yaw/3
  abs_L_wrist_yaw/1 -> gw_L_wrist_yaw/1
  gw_L_wrist_yaw/1 -> bi_L_wrist_yaw/1
  bi_L_wrist_yaw/1 -> sat_L_wrist_yaw/1
  sat_L_wrist_yaw/1 -> gT_L_wrist_yaw/1
  gT_L_wrist_yaw/1 -> gn_L_wrist_yaw/1, mn_L_wrist_yaw/2
  T_L_wrist_yaw/1 -> mn_L_wrist_yaw/1
  mn_L_wrist_yaw/1 -> mx_L_wrist_yaw/1
  gn_L_wrist_yaw/1 -> mx_L_wrist_yaw/2
  mx_L_wrist_yaw/1 -> ct_L_wrist_yaw/1, tau_mux/32
  [qr_R_ankle_pitch] -> S_R_ankle_pitch/1
  cq_R_ankle_pitch/1 -> S_R_ankle_pitch/2
  [dq_R_ankle_pitch] -> S_R_ankle_pitch/3
  S_R_ankle_pitch/1 -> K_R_ankle_pitch/1
  cw_R_ankle_pitch/1 -> B_R_ankle_pitch/1, abs_R_ankle_pitch/1
  K_R_ankle_pitch/1 -> pk_R_ankle_pitch/1
  [sch_R] -> pk_R_ankle_pitch/2
  pk_R_ankle_pitch/1 -> T_R_ankle_pitch/1
  B_R_ankle_pitch/1 -> pb_R_ankle_pitch/1
  [sch_R] -> pb_R_ankle_pitch/2
  pb_R_ankle_pitch/1 -> T_R_ankle_pitch/2
  [tf_R_ankle_pitch] -> T_R_ankle_pitch/3
  [fb_R_ankle_pitch] -> T_R_ankle_pitch/4
  abs_R_ankle_pitch/1 -> gw_R_ankle_pitch/1
  gw_R_ankle_pitch/1 -> bi_R_ankle_pitch/1
  bi_R_ankle_pitch/1 -> sat_R_ankle_pitch/1
  sat_R_ankle_pitch/1 -> gT_R_ankle_pitch/1
  gT_R_ankle_pitch/1 -> gn_R_ankle_pitch/1, mn_R_ankle_pitch/2
  T_R_ankle_pitch/1 -> mn_R_ankle_pitch/1
  mn_R_ankle_pitch/1 -> mx_R_ankle_pitch/1
  gn_R_ankle_pitch/1 -> mx_R_ankle_pitch/2
  mx_R_ankle_pitch/1 -> ct_R_ankle_pitch/1, tau_mux/33
  [qr_R_ankle_roll] -> S_R_ankle_roll/1
  cq_R_ankle_roll/1 -> S_R_ankle_roll/2
  S_R_ankle_roll/1 -> K_R_ankle_roll/1
  cw_R_ankle_roll/1 -> B_R_ankle_roll/1, abs_R_ankle_roll/1
  K_R_ankle_roll/1 -> T_R_ankle_roll/1
  B_R_ankle_roll/1 -> T_R_ankle_roll/2
  [tf_R_ankle_roll] -> T_R_ankle_roll/3
  [fb_R_ankle_roll] -> T_R_ankle_roll/4
  abs_R_ankle_roll/1 -> gw_R_ankle_roll/1
  gw_R_ankle_roll/1 -> bi_R_ankle_roll/1
  bi_R_ankle_roll/1 -> sat_R_ankle_roll/1
  sat_R_ankle_roll/1 -> gT_R_ankle_roll/1
  gT_R_ankle_roll/1 -> gn_R_ankle_roll/1, mn_R_ankle_roll/2
  T_R_ankle_roll/1 -> mn_R_ankle_roll/1
  mn_R_ankle_roll/1 -> mx_R_ankle_roll/1
  gn_R_ankle_roll/1 -> mx_R_ankle_roll/2
  mx_R_ankle_roll/1 -> ct_R_ankle_roll/1, tau_mux/34
  [qr_R_clavicle] -> S_R_clavicle/1
  cq_R_clavicle/1 -> S_R_clavicle/2
  S_R_clavicle/1 -> K_R_clavicle/1
  cw_R_clavicle/1 -> B_R_clavicle/1, abs_R_clavicle/1
  K_R_clavicle/1 -> T_R_clavicle/1
  B_R_clavicle/1 -> T_R_clavicle/2
  [tf_R_clavicle] -> T_R_clavicle/3
  abs_R_clavicle/1 -> gw_R_clavicle/1
  gw_R_clavicle/1 -> bi_R_clavicle/1
  bi_R_clavicle/1 -> sat_R_clavicle/1
  sat_R_clavicle/1 -> gT_R_clavicle/1
  gT_R_clavicle/1 -> gn_R_clavicle/1, mn_R_clavicle/2
  T_R_clavicle/1 -> mn_R_clavicle/1
  mn_R_clavicle/1 -> mx_R_clavicle/1
  gn_R_clavicle/1 -> mx_R_clavicle/2
  mx_R_clavicle/1 -> ct_R_clavicle/1, tau_mux/35
  [qr_R_elbow] -> S_R_elbow/1
  cq_R_elbow/1 -> S_R_elbow/2
  S_R_elbow/1 -> K_R_elbow/1
  cw_R_elbow/1 -> B_R_elbow/1, abs_R_elbow/1
  K_R_elbow/1 -> T_R_elbow/1
  B_R_elbow/1 -> T_R_elbow/2
  [tf_R_elbow] -> T_R_elbow/3
  abs_R_elbow/1 -> gw_R_elbow/1
  gw_R_elbow/1 -> bi_R_elbow/1
  bi_R_elbow/1 -> sat_R_elbow/1
  sat_R_elbow/1 -> gT_R_elbow/1
  gT_R_elbow/1 -> gn_R_elbow/1, mn_R_elbow/2
  T_R_elbow/1 -> mn_R_elbow/1
  mn_R_elbow/1 -> mx_R_elbow/1
  gn_R_elbow/1 -> mx_R_elbow/2
  mx_R_elbow/1 -> ct_R_elbow/1, tau_mux/36
  [qr_R_forearm_twist] -> S_R_forearm_twist/1
  cq_R_forearm_twist/1 -> S_R_forearm_twist/2
  S_R_forearm_twist/1 -> K_R_forearm_twist/1
  cw_R_forearm_twist/1 -> B_R_forearm_twist/1, abs_R_forearm_twist/1
  K_R_forearm_twist/1 -> T_R_forearm_twist/1
  B_R_forearm_twist/1 -> T_R_forearm_twist/2
  [tf_R_forearm_twist] -> T_R_forearm_twist/3
  abs_R_forearm_twist/1 -> gw_R_forearm_twist/1
  gw_R_forearm_twist/1 -> bi_R_forearm_twist/1
  bi_R_forearm_twist/1 -> sat_R_forearm_twist/1
  sat_R_forearm_twist/1 -> gT_R_forearm_twist/1
  gT_R_forearm_twist/1 -> gn_R_forearm_twist/1, mn_R_forearm_twist/2
  T_R_forearm_twist/1 -> mn_R_forearm_twist/1
  mn_R_forearm_twist/1 -> mx_R_forearm_twist/1
  gn_R_forearm_twist/1 -> mx_R_forearm_twist/2
  mx_R_forearm_twist/1 -> ct_R_forearm_twist/1, tau_mux/37
  [qr_R_hip_pitch] -> S_R_hip_pitch/1
  cq_R_hip_pitch/1 -> S_R_hip_pitch/2
  [dq_R_hip_pitch] -> S_R_hip_pitch/3
  S_R_hip_pitch/1 -> K_R_hip_pitch/1
  cw_R_hip_pitch/1 -> B_R_hip_pitch/1, abs_R_hip_pitch/1
  K_R_hip_pitch/1 -> pk_R_hip_pitch/1
  [sch_R] -> pk_R_hip_pitch/2
  pk_R_hip_pitch/1 -> T_R_hip_pitch/1
  B_R_hip_pitch/1 -> pb_R_hip_pitch/1
  [sch_R] -> pb_R_hip_pitch/2
  pb_R_hip_pitch/1 -> T_R_hip_pitch/2
  [tf_R_hip_pitch] -> T_R_hip_pitch/3
  abs_R_hip_pitch/1 -> gw_R_hip_pitch/1
  gw_R_hip_pitch/1 -> bi_R_hip_pitch/1
  bi_R_hip_pitch/1 -> sat_R_hip_pitch/1
  sat_R_hip_pitch/1 -> gT_R_hip_pitch/1
  gT_R_hip_pitch/1 -> gn_R_hip_pitch/1, mn_R_hip_pitch/2
  T_R_hip_pitch/1 -> mn_R_hip_pitch/1
  mn_R_hip_pitch/1 -> mx_R_hip_pitch/1
  gn_R_hip_pitch/1 -> mx_R_hip_pitch/2
  mx_R_hip_pitch/1 -> ct_R_hip_pitch/1, tau_mux/38
  [qr_R_hip_roll] -> S_R_hip_roll/1
  cq_R_hip_roll/1 -> S_R_hip_roll/2
  S_R_hip_roll/1 -> K_R_hip_roll/1
  cw_R_hip_roll/1 -> B_R_hip_roll/1, abs_R_hip_roll/1
  K_R_hip_roll/1 -> T_R_hip_roll/1
  B_R_hip_roll/1 -> T_R_hip_roll/2
  [tf_R_hip_roll] -> T_R_hip_roll/3
  abs_R_hip_roll/1 -> gw_R_hip_roll/1
  gw_R_hip_roll/1 -> bi_R_hip_roll/1
  bi_R_hip_roll/1 -> sat_R_hip_roll/1
  sat_R_hip_roll/1 -> gT_R_hip_roll/1
  gT_R_hip_roll/1 -> gn_R_hip_roll/1, mn_R_hip_roll/2
  T_R_hip_roll/1 -> mn_R_hip_roll/1
  mn_R_hip_roll/1 -> mx_R_hip_roll/1
  gn_R_hip_roll/1 -> mx_R_hip_roll/2
  mx_R_hip_roll/1 -> ct_R_hip_roll/1, tau_mux/39
  [qr_R_hip_yaw] -> S_R_hip_yaw/1
  cq_R_hip_yaw/1 -> S_R_hip_yaw/2
  S_R_hip_yaw/1 -> K_R_hip_yaw/1
  cw_R_hip_yaw/1 -> B_R_hip_yaw/1, abs_R_hip_yaw/1
  K_R_hip_yaw/1 -> T_R_hip_yaw/1
  B_R_hip_yaw/1 -> T_R_hip_yaw/2
  [tf_R_hip_yaw] -> T_R_hip_yaw/3
  abs_R_hip_yaw/1 -> gw_R_hip_yaw/1
  gw_R_hip_yaw/1 -> bi_R_hip_yaw/1
  bi_R_hip_yaw/1 -> sat_R_hip_yaw/1
  sat_R_hip_yaw/1 -> gT_R_hip_yaw/1
  gT_R_hip_yaw/1 -> gn_R_hip_yaw/1, mn_R_hip_yaw/2
  T_R_hip_yaw/1 -> mn_R_hip_yaw/1
  mn_R_hip_yaw/1 -> mx_R_hip_yaw/1
  gn_R_hip_yaw/1 -> mx_R_hip_yaw/2
  mx_R_hip_yaw/1 -> ct_R_hip_yaw/1, tau_mux/40
  [qr_R_index1] -> S_R_index1/1
  cq_R_index1/1 -> S_R_index1/2
  S_R_index1/1 -> K_R_index1/1
  cw_R_index1/1 -> B_R_index1/1, abs_R_index1/1
  K_R_index1/1 -> T_R_index1/1
  B_R_index1/1 -> T_R_index1/2
  [tf_R_index1] -> T_R_index1/3
  abs_R_index1/1 -> gw_R_index1/1
  gw_R_index1/1 -> bi_R_index1/1
  bi_R_index1/1 -> sat_R_index1/1
  sat_R_index1/1 -> gT_R_index1/1
  gT_R_index1/1 -> gn_R_index1/1, mn_R_index1/2
  T_R_index1/1 -> mn_R_index1/1
  mn_R_index1/1 -> mx_R_index1/1
  gn_R_index1/1 -> mx_R_index1/2
  mx_R_index1/1 -> ct_R_index1/1, tau_mux/41
  [qr_R_index2] -> S_R_index2/1
  cq_R_index2/1 -> S_R_index2/2
  S_R_index2/1 -> K_R_index2/1
  cw_R_index2/1 -> B_R_index2/1, abs_R_index2/1
  K_R_index2/1 -> T_R_index2/1
  B_R_index2/1 -> T_R_index2/2
  [tf_R_index2] -> T_R_index2/3
  abs_R_index2/1 -> gw_R_index2/1
  gw_R_index2/1 -> bi_R_index2/1
  bi_R_index2/1 -> sat_R_index2/1
  sat_R_index2/1 -> gT_R_index2/1
  gT_R_index2/1 -> gn_R_index2/1, mn_R_index2/2
  T_R_index2/1 -> mn_R_index2/1
  mn_R_index2/1 -> mx_R_index2/1
  gn_R_index2/1 -> mx_R_index2/2
  mx_R_index2/1 -> ct_R_index2/1, tau_mux/42
  [qr_R_index3] -> S_R_index3/1
  cq_R_index3/1 -> S_R_index3/2
  S_R_index3/1 -> K_R_index3/1
  cw_R_index3/1 -> B_R_index3/1, abs_R_index3/1
  K_R_index3/1 -> T_R_index3/1
  B_R_index3/1 -> T_R_index3/2
  [tf_R_index3] -> T_R_index3/3
  abs_R_index3/1 -> gw_R_index3/1
  gw_R_index3/1 -> bi_R_index3/1
  bi_R_index3/1 -> sat_R_index3/1
  sat_R_index3/1 -> gT_R_index3/1
  gT_R_index3/1 -> gn_R_index3/1, mn_R_index3/2
  T_R_index3/1 -> mn_R_index3/1
  mn_R_index3/1 -> mx_R_index3/1
  gn_R_index3/1 -> mx_R_index3/2
  mx_R_index3/1 -> ct_R_index3/1, tau_mux/43
  [qr_R_knee] -> S_R_knee/1
  cq_R_knee/1 -> S_R_knee/2
  S_R_knee/1 -> K_R_knee/1
  cw_R_knee/1 -> B_R_knee/1, abs_R_knee/1
  K_R_knee/1 -> pk_R_knee/1
  [sch_R] -> pk_R_knee/2
  pk_R_knee/1 -> T_R_knee/1
  B_R_knee/1 -> pb_R_knee/1
  [sch_R] -> pb_R_knee/2
  pb_R_knee/1 -> T_R_knee/2
  [tf_R_knee] -> T_R_knee/3
  abs_R_knee/1 -> gw_R_knee/1
  gw_R_knee/1 -> bi_R_knee/1
  bi_R_knee/1 -> sat_R_knee/1
  sat_R_knee/1 -> gT_R_knee/1
  gT_R_knee/1 -> gn_R_knee/1, mn_R_knee/2
  T_R_knee/1 -> mn_R_knee/1
  mn_R_knee/1 -> mx_R_knee/1
  gn_R_knee/1 -> mx_R_knee/2
  mx_R_knee/1 -> ct_R_knee/1, tau_mux/44
  [qr_R_little1] -> S_R_little1/1
  cq_R_little1/1 -> S_R_little1/2
  S_R_little1/1 -> K_R_little1/1
  cw_R_little1/1 -> B_R_little1/1, abs_R_little1/1
  K_R_little1/1 -> T_R_little1/1
  B_R_little1/1 -> T_R_little1/2
  [tf_R_little1] -> T_R_little1/3
  abs_R_little1/1 -> gw_R_little1/1
  gw_R_little1/1 -> bi_R_little1/1
  bi_R_little1/1 -> sat_R_little1/1
  sat_R_little1/1 -> gT_R_little1/1
  gT_R_little1/1 -> gn_R_little1/1, mn_R_little1/2
  T_R_little1/1 -> mn_R_little1/1
  mn_R_little1/1 -> mx_R_little1/1
  gn_R_little1/1 -> mx_R_little1/2
  mx_R_little1/1 -> ct_R_little1/1, tau_mux/45
  [qr_R_little2] -> S_R_little2/1
  cq_R_little2/1 -> S_R_little2/2
  S_R_little2/1 -> K_R_little2/1
  cw_R_little2/1 -> B_R_little2/1, abs_R_little2/1
  K_R_little2/1 -> T_R_little2/1
  B_R_little2/1 -> T_R_little2/2
  [tf_R_little2] -> T_R_little2/3
  abs_R_little2/1 -> gw_R_little2/1
  gw_R_little2/1 -> bi_R_little2/1
  bi_R_little2/1 -> sat_R_little2/1
  sat_R_little2/1 -> gT_R_little2/1
  gT_R_little2/1 -> gn_R_little2/1, mn_R_little2/2
  T_R_little2/1 -> mn_R_little2/1
  mn_R_little2/1 -> mx_R_little2/1
  gn_R_little2/1 -> mx_R_little2/2
  mx_R_little2/1 -> ct_R_little2/1, tau_mux/46
  [qr_R_little3] -> S_R_little3/1
  cq_R_little3/1 -> S_R_little3/2
  S_R_little3/1 -> K_R_little3/1
  cw_R_little3/1 -> B_R_little3/1, abs_R_little3/1
  K_R_little3/1 -> T_R_little3/1
  B_R_little3/1 -> T_R_little3/2
  [tf_R_little3] -> T_R_little3/3
  abs_R_little3/1 -> gw_R_little3/1
  gw_R_little3/1 -> bi_R_little3/1
  bi_R_little3/1 -> sat_R_little3/1
  sat_R_little3/1 -> gT_R_little3/1
  gT_R_little3/1 -> gn_R_little3/1, mn_R_little3/2
  T_R_little3/1 -> mn_R_little3/1
  mn_R_little3/1 -> mx_R_little3/1
  gn_R_little3/1 -> mx_R_little3/2
  mx_R_little3/1 -> ct_R_little3/1, tau_mux/47
  [qr_R_middle1] -> S_R_middle1/1
  cq_R_middle1/1 -> S_R_middle1/2
  S_R_middle1/1 -> K_R_middle1/1
  cw_R_middle1/1 -> B_R_middle1/1, abs_R_middle1/1
  K_R_middle1/1 -> T_R_middle1/1
  B_R_middle1/1 -> T_R_middle1/2
  [tf_R_middle1] -> T_R_middle1/3
  abs_R_middle1/1 -> gw_R_middle1/1
  gw_R_middle1/1 -> bi_R_middle1/1
  bi_R_middle1/1 -> sat_R_middle1/1
  sat_R_middle1/1 -> gT_R_middle1/1
  gT_R_middle1/1 -> gn_R_middle1/1, mn_R_middle1/2
  T_R_middle1/1 -> mn_R_middle1/1
  mn_R_middle1/1 -> mx_R_middle1/1
  gn_R_middle1/1 -> mx_R_middle1/2
  mx_R_middle1/1 -> ct_R_middle1/1, tau_mux/48
  [qr_R_middle2] -> S_R_middle2/1
  cq_R_middle2/1 -> S_R_middle2/2
  S_R_middle2/1 -> K_R_middle2/1
  cw_R_middle2/1 -> B_R_middle2/1, abs_R_middle2/1
  K_R_middle2/1 -> T_R_middle2/1
  B_R_middle2/1 -> T_R_middle2/2
  [tf_R_middle2] -> T_R_middle2/3
  abs_R_middle2/1 -> gw_R_middle2/1
  gw_R_middle2/1 -> bi_R_middle2/1
  bi_R_middle2/1 -> sat_R_middle2/1
  sat_R_middle2/1 -> gT_R_middle2/1
  gT_R_middle2/1 -> gn_R_middle2/1, mn_R_middle2/2
  T_R_middle2/1 -> mn_R_middle2/1
  mn_R_middle2/1 -> mx_R_middle2/1
  gn_R_middle2/1 -> mx_R_middle2/2
  mx_R_middle2/1 -> ct_R_middle2/1, tau_mux/49
  [qr_R_middle3] -> S_R_middle3/1
  cq_R_middle3/1 -> S_R_middle3/2
  S_R_middle3/1 -> K_R_middle3/1
  cw_R_middle3/1 -> B_R_middle3/1, abs_R_middle3/1
  K_R_middle3/1 -> T_R_middle3/1
  B_R_middle3/1 -> T_R_middle3/2
  [tf_R_middle3] -> T_R_middle3/3
  abs_R_middle3/1 -> gw_R_middle3/1
  gw_R_middle3/1 -> bi_R_middle3/1
  bi_R_middle3/1 -> sat_R_middle3/1
  sat_R_middle3/1 -> gT_R_middle3/1
  gT_R_middle3/1 -> gn_R_middle3/1, mn_R_middle3/2
  T_R_middle3/1 -> mn_R_middle3/1
  mn_R_middle3/1 -> mx_R_middle3/1
  gn_R_middle3/1 -> mx_R_middle3/2
  mx_R_middle3/1 -> ct_R_middle3/1, tau_mux/50
  [qr_R_ring1] -> S_R_ring1/1
  cq_R_ring1/1 -> S_R_ring1/2
  S_R_ring1/1 -> K_R_ring1/1
  cw_R_ring1/1 -> B_R_ring1/1, abs_R_ring1/1
  K_R_ring1/1 -> T_R_ring1/1
  B_R_ring1/1 -> T_R_ring1/2
  [tf_R_ring1] -> T_R_ring1/3
  abs_R_ring1/1 -> gw_R_ring1/1
  gw_R_ring1/1 -> bi_R_ring1/1
  bi_R_ring1/1 -> sat_R_ring1/1
  sat_R_ring1/1 -> gT_R_ring1/1
  gT_R_ring1/1 -> gn_R_ring1/1, mn_R_ring1/2
  T_R_ring1/1 -> mn_R_ring1/1
  mn_R_ring1/1 -> mx_R_ring1/1
  gn_R_ring1/1 -> mx_R_ring1/2
  mx_R_ring1/1 -> ct_R_ring1/1, tau_mux/51
  [qr_R_ring2] -> S_R_ring2/1
  cq_R_ring2/1 -> S_R_ring2/2
  S_R_ring2/1 -> K_R_ring2/1
  cw_R_ring2/1 -> B_R_ring2/1, abs_R_ring2/1
  K_R_ring2/1 -> T_R_ring2/1
  B_R_ring2/1 -> T_R_ring2/2
  [tf_R_ring2] -> T_R_ring2/3
  abs_R_ring2/1 -> gw_R_ring2/1
  gw_R_ring2/1 -> bi_R_ring2/1
  bi_R_ring2/1 -> sat_R_ring2/1
  sat_R_ring2/1 -> gT_R_ring2/1
  gT_R_ring2/1 -> gn_R_ring2/1, mn_R_ring2/2
  T_R_ring2/1 -> mn_R_ring2/1
  mn_R_ring2/1 -> mx_R_ring2/1
  gn_R_ring2/1 -> mx_R_ring2/2
  mx_R_ring2/1 -> ct_R_ring2/1, tau_mux/52
  [qr_R_ring3] -> S_R_ring3/1
  cq_R_ring3/1 -> S_R_ring3/2
  S_R_ring3/1 -> K_R_ring3/1
  cw_R_ring3/1 -> B_R_ring3/1, abs_R_ring3/1
  K_R_ring3/1 -> T_R_ring3/1
  B_R_ring3/1 -> T_R_ring3/2
  [tf_R_ring3] -> T_R_ring3/3
  abs_R_ring3/1 -> gw_R_ring3/1
  gw_R_ring3/1 -> bi_R_ring3/1
  bi_R_ring3/1 -> sat_R_ring3/1
  sat_R_ring3/1 -> gT_R_ring3/1
  gT_R_ring3/1 -> gn_R_ring3/1, mn_R_ring3/2
  T_R_ring3/1 -> mn_R_ring3/1
  mn_R_ring3/1 -> mx_R_ring3/1
  gn_R_ring3/1 -> mx_R_ring3/2
  mx_R_ring3/1 -> ct_R_ring3/1, tau_mux/53
  [qr_R_scapula] -> S_R_scapula/1
  cq_R_scapula/1 -> S_R_scapula/2
  S_R_scapula/1 -> K_R_scapula/1
  cw_R_scapula/1 -> B_R_scapula/1, abs_R_scapula/1
  K_R_scapula/1 -> T_R_scapula/1
  B_R_scapula/1 -> T_R_scapula/2
  [tf_R_scapula] -> T_R_scapula/3
  abs_R_scapula/1 -> gw_R_scapula/1
  gw_R_scapula/1 -> bi_R_scapula/1
  bi_R_scapula/1 -> sat_R_scapula/1
  sat_R_scapula/1 -> gT_R_scapula/1
  gT_R_scapula/1 -> gn_R_scapula/1, mn_R_scapula/2
  T_R_scapula/1 -> mn_R_scapula/1
  mn_R_scapula/1 -> mx_R_scapula/1
  gn_R_scapula/1 -> mx_R_scapula/2
  mx_R_scapula/1 -> ct_R_scapula/1, tau_mux/54
  [qr_R_shoulder_pitch] -> S_R_shoulder_pitch/1
  cq_R_shoulder_pitch/1 -> S_R_shoulder_pitch/2
  S_R_shoulder_pitch/1 -> K_R_shoulder_pitch/1
  cw_R_shoulder_pitch/1 -> B_R_shoulder_pitch/1, abs_R_shoulder_pitch/1
  K_R_shoulder_pitch/1 -> T_R_shoulder_pitch/1
  B_R_shoulder_pitch/1 -> T_R_shoulder_pitch/2
  [tf_R_shoulder_pitch] -> T_R_shoulder_pitch/3
  abs_R_shoulder_pitch/1 -> gw_R_shoulder_pitch/1
  gw_R_shoulder_pitch/1 -> bi_R_shoulder_pitch/1
  bi_R_shoulder_pitch/1 -> sat_R_shoulder_pitch/1
  sat_R_shoulder_pitch/1 -> gT_R_shoulder_pitch/1
  gT_R_shoulder_pitch/1 -> gn_R_shoulder_pitch/1, mn_R_shoulder_pitch/2
  T_R_shoulder_pitch/1 -> mn_R_shoulder_pitch/1
  mn_R_shoulder_pitch/1 -> mx_R_shoulder_pitch/1
  gn_R_shoulder_pitch/1 -> mx_R_shoulder_pitch/2
  mx_R_shoulder_pitch/1 -> ct_R_shoulder_pitch/1, tau_mux/55
  [qr_R_shoulder_roll] -> S_R_shoulder_roll/1
  cq_R_shoulder_roll/1 -> S_R_shoulder_roll/2
  S_R_shoulder_roll/1 -> K_R_shoulder_roll/1
  cw_R_shoulder_roll/1 -> B_R_shoulder_roll/1, abs_R_shoulder_roll/1
  K_R_shoulder_roll/1 -> T_R_shoulder_roll/1
  B_R_shoulder_roll/1 -> T_R_shoulder_roll/2
  [tf_R_shoulder_roll] -> T_R_shoulder_roll/3
  abs_R_shoulder_roll/1 -> gw_R_shoulder_roll/1
  gw_R_shoulder_roll/1 -> bi_R_shoulder_roll/1
  bi_R_shoulder_roll/1 -> sat_R_shoulder_roll/1
  sat_R_shoulder_roll/1 -> gT_R_shoulder_roll/1
  gT_R_shoulder_roll/1 -> gn_R_shoulder_roll/1, mn_R_shoulder_roll/2
  T_R_shoulder_roll/1 -> mn_R_shoulder_roll/1
  mn_R_shoulder_roll/1 -> mx_R_shoulder_roll/1
  gn_R_shoulder_roll/1 -> mx_R_shoulder_roll/2
  mx_R_shoulder_roll/1 -> ct_R_shoulder_roll/1, tau_mux/56
  [qr_R_shoulder_yaw] -> S_R_shoulder_yaw/1
  cq_R_shoulder_yaw/1 -> S_R_shoulder_yaw/2
  S_R_shoulder_yaw/1 -> K_R_shoulder_yaw/1
  cw_R_shoulder_yaw/1 -> B_R_shoulder_yaw/1, abs_R_shoulder_yaw/1
  K_R_shoulder_yaw/1 -> T_R_shoulder_yaw/1
  B_R_shoulder_yaw/1 -> T_R_shoulder_yaw/2
  [tf_R_shoulder_yaw] -> T_R_shoulder_yaw/3
  abs_R_shoulder_yaw/1 -> gw_R_shoulder_yaw/1
  gw_R_shoulder_yaw/1 -> bi_R_shoulder_yaw/1
  bi_R_shoulder_yaw/1 -> sat_R_shoulder_yaw/1
  sat_R_shoulder_yaw/1 -> gT_R_shoulder_yaw/1
  gT_R_shoulder_yaw/1 -> gn_R_shoulder_yaw/1, mn_R_shoulder_yaw/2
  T_R_shoulder_yaw/1 -> mn_R_shoulder_yaw/1
  mn_R_shoulder_yaw/1 -> mx_R_shoulder_yaw/1
  gn_R_shoulder_yaw/1 -> mx_R_shoulder_yaw/2
  mx_R_shoulder_yaw/1 -> ct_R_shoulder_yaw/1, tau_mux/57
  [qr_R_thumb1] -> S_R_thumb1/1
  cq_R_thumb1/1 -> S_R_thumb1/2
  S_R_thumb1/1 -> K_R_thumb1/1
  cw_R_thumb1/1 -> B_R_thumb1/1, abs_R_thumb1/1
  K_R_thumb1/1 -> T_R_thumb1/1
  B_R_thumb1/1 -> T_R_thumb1/2
  [tf_R_thumb1] -> T_R_thumb1/3
  abs_R_thumb1/1 -> gw_R_thumb1/1
  gw_R_thumb1/1 -> bi_R_thumb1/1
  bi_R_thumb1/1 -> sat_R_thumb1/1
  sat_R_thumb1/1 -> gT_R_thumb1/1
  gT_R_thumb1/1 -> gn_R_thumb1/1, mn_R_thumb1/2
  T_R_thumb1/1 -> mn_R_thumb1/1
  mn_R_thumb1/1 -> mx_R_thumb1/1
  gn_R_thumb1/1 -> mx_R_thumb1/2
  mx_R_thumb1/1 -> ct_R_thumb1/1, tau_mux/58
  [qr_R_thumb2] -> S_R_thumb2/1
  cq_R_thumb2/1 -> S_R_thumb2/2
  S_R_thumb2/1 -> K_R_thumb2/1
  cw_R_thumb2/1 -> B_R_thumb2/1, abs_R_thumb2/1
  K_R_thumb2/1 -> T_R_thumb2/1
  B_R_thumb2/1 -> T_R_thumb2/2
  [tf_R_thumb2] -> T_R_thumb2/3
  abs_R_thumb2/1 -> gw_R_thumb2/1
  gw_R_thumb2/1 -> bi_R_thumb2/1
  bi_R_thumb2/1 -> sat_R_thumb2/1
  sat_R_thumb2/1 -> gT_R_thumb2/1
  gT_R_thumb2/1 -> gn_R_thumb2/1, mn_R_thumb2/2
  T_R_thumb2/1 -> mn_R_thumb2/1
  mn_R_thumb2/1 -> mx_R_thumb2/1
  gn_R_thumb2/1 -> mx_R_thumb2/2
  mx_R_thumb2/1 -> ct_R_thumb2/1, tau_mux/59
  [qr_R_thumb3] -> S_R_thumb3/1
  cq_R_thumb3/1 -> S_R_thumb3/2
  S_R_thumb3/1 -> K_R_thumb3/1
  cw_R_thumb3/1 -> B_R_thumb3/1, abs_R_thumb3/1
  K_R_thumb3/1 -> T_R_thumb3/1
  B_R_thumb3/1 -> T_R_thumb3/2
  [tf_R_thumb3] -> T_R_thumb3/3
  abs_R_thumb3/1 -> gw_R_thumb3/1
  gw_R_thumb3/1 -> bi_R_thumb3/1
  bi_R_thumb3/1 -> sat_R_thumb3/1
  sat_R_thumb3/1 -> gT_R_thumb3/1
  gT_R_thumb3/1 -> gn_R_thumb3/1, mn_R_thumb3/2
  T_R_thumb3/1 -> mn_R_thumb3/1
  mn_R_thumb3/1 -> mx_R_thumb3/1
  gn_R_thumb3/1 -> mx_R_thumb3/2
  mx_R_thumb3/1 -> ct_R_thumb3/1, tau_mux/60
  [qr_R_toe] -> S_R_toe/1
  cq_R_toe/1 -> S_R_toe/2
  S_R_toe/1 -> K_R_toe/1
  cw_R_toe/1 -> B_R_toe/1, abs_R_toe/1
  K_R_toe/1 -> T_R_toe/1
  B_R_toe/1 -> T_R_toe/2
  [tf_R_toe] -> T_R_toe/3
  abs_R_toe/1 -> gw_R_toe/1
  gw_R_toe/1 -> bi_R_toe/1
  bi_R_toe/1 -> sat_R_toe/1
  sat_R_toe/1 -> gT_R_toe/1
  gT_R_toe/1 -> gn_R_toe/1, mn_R_toe/2
  T_R_toe/1 -> mn_R_toe/1
  mn_R_toe/1 -> mx_R_toe/1
  gn_R_toe/1 -> mx_R_toe/2
  mx_R_toe/1 -> ct_R_toe/1, tau_mux/61
  [qr_R_wrist_pitch] -> S_R_wrist_pitch/1
  cq_R_wrist_pitch/1 -> S_R_wrist_pitch/2
  S_R_wrist_pitch/1 -> K_R_wrist_pitch/1
  cw_R_wrist_pitch/1 -> B_R_wrist_pitch/1, abs_R_wrist_pitch/1
  K_R_wrist_pitch/1 -> T_R_wrist_pitch/1
  B_R_wrist_pitch/1 -> T_R_wrist_pitch/2
  [tf_R_wrist_pitch] -> T_R_wrist_pitch/3
  abs_R_wrist_pitch/1 -> gw_R_wrist_pitch/1
  gw_R_wrist_pitch/1 -> bi_R_wrist_pitch/1
  bi_R_wrist_pitch/1 -> sat_R_wrist_pitch/1
  sat_R_wrist_pitch/1 -> gT_R_wrist_pitch/1
  gT_R_wrist_pitch/1 -> gn_R_wrist_pitch/1, mn_R_wrist_pitch/2
  T_R_wrist_pitch/1 -> mn_R_wrist_pitch/1
  mn_R_wrist_pitch/1 -> mx_R_wrist_pitch/1
  gn_R_wrist_pitch/1 -> mx_R_wrist_pitch/2
  mx_R_wrist_pitch/1 -> ct_R_wrist_pitch/1, tau_mux/62
  [qr_R_wrist_roll] -> S_R_wrist_roll/1
  cq_R_wrist_roll/1 -> S_R_wrist_roll/2
  S_R_wrist_roll/1 -> K_R_wrist_roll/1
  cw_R_wrist_roll/1 -> B_R_wrist_roll/1, abs_R_wrist_roll/1
  K_R_wrist_roll/1 -> T_R_wrist_roll/1
  B_R_wrist_roll/1 -> T_R_wrist_roll/2
  [tf_R_wrist_roll] -> T_R_wrist_roll/3
  abs_R_wrist_roll/1 -> gw_R_wrist_roll/1
  gw_R_wrist_roll/1 -> bi_R_wrist_roll/1
  bi_R_wrist_roll/1 -> sat_R_wrist_roll/1
  sat_R_wrist_roll/1 -> gT_R_wrist_roll/1
  gT_R_wrist_roll/1 -> gn_R_wrist_roll/1, mn_R_wrist_roll/2
  T_R_wrist_roll/1 -> mn_R_wrist_roll/1
  mn_R_wrist_roll/1 -> mx_R_wrist_roll/1
  gn_R_wrist_roll/1 -> mx_R_wrist_roll/2
  mx_R_wrist_roll/1 -> ct_R_wrist_roll/1, tau_mux/63
  [qr_R_wrist_yaw] -> S_R_wrist_yaw/1
  cq_R_wrist_yaw/1 -> S_R_wrist_yaw/2
  S_R_wrist_yaw/1 -> K_R_wrist_yaw/1
  cw_R_wrist_yaw/1 -> B_R_wrist_yaw/1, abs_R_wrist_yaw/1
  K_R_wrist_yaw/1 -> T_R_wrist_yaw/1
  B_R_wrist_yaw/1 -> T_R_wrist_yaw/2
  [tf_R_wrist_yaw] -> T_R_wrist_yaw/3
  abs_R_wrist_yaw/1 -> gw_R_wrist_yaw/1
  gw_R_wrist_yaw/1 -> bi_R_wrist_yaw/1
  bi_R_wrist_yaw/1 -> sat_R_wrist_yaw/1
  sat_R_wrist_yaw/1 -> gT_R_wrist_yaw/1
  gT_R_wrist_yaw/1 -> gn_R_wrist_yaw/1, mn_R_wrist_yaw/2
  T_R_wrist_yaw/1 -> mn_R_wrist_yaw/1
  mn_R_wrist_yaw/1 -> mx_R_wrist_yaw/1
  gn_R_wrist_yaw/1 -> mx_R_wrist_yaw/2
  mx_R_wrist_yaw/1 -> ct_R_wrist_yaw/1, tau_mux/64
  [qr_neck_pitch] -> S_neck_pitch/1
  cq_neck_pitch/1 -> S_neck_pitch/2
  S_neck_pitch/1 -> K_neck_pitch/1
  cw_neck_pitch/1 -> B_neck_pitch/1, abs_neck_pitch/1
  K_neck_pitch/1 -> T_neck_pitch/1
  B_neck_pitch/1 -> T_neck_pitch/2
  [tf_neck_pitch] -> T_neck_pitch/3
  abs_neck_pitch/1 -> gw_neck_pitch/1
  gw_neck_pitch/1 -> bi_neck_pitch/1
  bi_neck_pitch/1 -> sat_neck_pitch/1
  sat_neck_pitch/1 -> gT_neck_pitch/1
  gT_neck_pitch/1 -> gn_neck_pitch/1, mn_neck_pitch/2
  T_neck_pitch/1 -> mn_neck_pitch/1
  mn_neck_pitch/1 -> mx_neck_pitch/1
  gn_neck_pitch/1 -> mx_neck_pitch/2
  mx_neck_pitch/1 -> ct_neck_pitch/1, tau_mux/65
  [qr_neck_roll] -> S_neck_roll/1
  cq_neck_roll/1 -> S_neck_roll/2
  S_neck_roll/1 -> K_neck_roll/1
  cw_neck_roll/1 -> B_neck_roll/1, abs_neck_roll/1
  K_neck_roll/1 -> T_neck_roll/1
  B_neck_roll/1 -> T_neck_roll/2
  [tf_neck_roll] -> T_neck_roll/3
  abs_neck_roll/1 -> gw_neck_roll/1
  gw_neck_roll/1 -> bi_neck_roll/1
  bi_neck_roll/1 -> sat_neck_roll/1
  sat_neck_roll/1 -> gT_neck_roll/1
  gT_neck_roll/1 -> gn_neck_roll/1, mn_neck_roll/2
  T_neck_roll/1 -> mn_neck_roll/1
  mn_neck_roll/1 -> mx_neck_roll/1
  gn_neck_roll/1 -> mx_neck_roll/2
  mx_neck_roll/1 -> ct_neck_roll/1, tau_mux/66
  [qr_neck_yaw] -> S_neck_yaw/1
  cq_neck_yaw/1 -> S_neck_yaw/2
  S_neck_yaw/1 -> K_neck_yaw/1
  cw_neck_yaw/1 -> B_neck_yaw/1, abs_neck_yaw/1
  K_neck_yaw/1 -> T_neck_yaw/1
  B_neck_yaw/1 -> T_neck_yaw/2
  [tf_neck_yaw] -> T_neck_yaw/3
  abs_neck_yaw/1 -> gw_neck_yaw/1
  gw_neck_yaw/1 -> bi_neck_yaw/1
  bi_neck_yaw/1 -> sat_neck_yaw/1
  sat_neck_yaw/1 -> gT_neck_yaw/1
  gT_neck_yaw/1 -> gn_neck_yaw/1, mn_neck_yaw/2
  T_neck_yaw/1 -> mn_neck_yaw/1
  mn_neck_yaw/1 -> mx_neck_yaw/1
  gn_neck_yaw/1 -> mx_neck_yaw/2
  mx_neck_yaw/1 -> ct_neck_yaw/1, tau_mux/67
  [qr_waist_pitch] -> S_waist_pitch/1
  cq_waist_pitch/1 -> S_waist_pitch/2
  S_waist_pitch/1 -> K_waist_pitch/1
  cw_waist_pitch/1 -> B_waist_pitch/1, abs_waist_pitch/1
  K_waist_pitch/1 -> T_waist_pitch/1
  B_waist_pitch/1 -> T_waist_pitch/2
  [tf_waist_pitch] -> T_waist_pitch/3
  abs_waist_pitch/1 -> gw_waist_pitch/1
  gw_waist_pitch/1 -> bi_waist_pitch/1
  bi_waist_pitch/1 -> sat_waist_pitch/1
  sat_waist_pitch/1 -> gT_waist_pitch/1
  gT_waist_pitch/1 -> gn_waist_pitch/1, mn_waist_pitch/2
  T_waist_pitch/1 -> mn_waist_pitch/1
  mn_waist_pitch/1 -> mx_waist_pitch/1
  gn_waist_pitch/1 -> mx_waist_pitch/2
  mx_waist_pitch/1 -> ct_waist_pitch/1, tau_mux/68
  [qr_waist_roll] -> S_waist_roll/1
  cq_waist_roll/1 -> S_waist_roll/2
  S_waist_roll/1 -> K_waist_roll/1
  cw_waist_roll/1 -> B_waist_roll/1, abs_waist_roll/1
  K_waist_roll/1 -> T_waist_roll/1
  B_waist_roll/1 -> T_waist_roll/2
  [tf_waist_roll] -> T_waist_roll/3
  abs_waist_roll/1 -> gw_waist_roll/1
  gw_waist_roll/1 -> bi_waist_roll/1
  bi_waist_roll/1 -> sat_waist_roll/1
  sat_waist_roll/1 -> gT_waist_roll/1
  gT_waist_roll/1 -> gn_waist_roll/1, mn_waist_roll/2
  T_waist_roll/1 -> mn_waist_roll/1
  mn_waist_roll/1 -> mx_waist_roll/1
  gn_waist_roll/1 -> mx_waist_roll/2
  mx_waist_roll/1 -> ct_waist_roll/1, tau_mux/69
  [qr_waist_yaw] -> S_waist_yaw/1
  cq_waist_yaw/1 -> S_waist_yaw/2
  S_waist_yaw/1 -> K_waist_yaw/1
  cw_waist_yaw/1 -> B_waist_yaw/1, abs_waist_yaw/1
  K_waist_yaw/1 -> T_waist_yaw/1
  B_waist_yaw/1 -> T_waist_yaw/2
  [tf_waist_yaw] -> T_waist_yaw/3
  abs_waist_yaw/1 -> gw_waist_yaw/1
  gw_waist_yaw/1 -> bi_waist_yaw/1
  bi_waist_yaw/1 -> sat_waist_yaw/1
  sat_waist_yaw/1 -> gT_waist_yaw/1
  gT_waist_yaw/1 -> gn_waist_yaw/1, mn_waist_yaw/2
  T_waist_yaw/1 -> mn_waist_yaw/1
  mn_waist_yaw/1 -> mx_waist_yaw/1
  gn_waist_yaw/1 -> mx_waist_yaw/2
  mx_waist_yaw/1 -> ct_waist_yaw/1, tau_mux/70
  pref/1 -> pref_demux/1
  lam/1 -> lam_demux/1
  pc_X/1 -> err_X/1
  pref_demux/1 -> err_X/2
  pc_Y/1 -> err_Y/1
  pref_demux/2 -> err_Y/2
  pc_XDot/1 -> err_XDot/1
  pref_demux/3 -> err_XDot/2
  pc_YDot/1 -> err_YDot/1
  pref_demux/4 -> err_YDot/2
  err_X/1 -> fb_gxp/1, st_xi/1
  err_XDot/1 -> fb_gxd/1, st_gv/1
  err_Y/1 -> fb_gyp/1
  err_YDot/1 -> fb_gyd/1
  fb_gxp/1 -> fb_sx/1
  fb_gxd/1 -> fb_sx/2
  fb_gyp/1 -> fb_sy/1
  fb_gyd/1 -> fb_sy/2
  fb_sx/1 -> fb_satx/1
  fb_sy/1 -> fb_saty/1
  fb_satx/1 -> fb_pm_L1/1, fb_pm_R1/1
  lam_demux/1 -> fb_pm_L1/2, fb_pm_L2/2
  fb_pm_L1/1 -> [fb_L_ankle_pitch]
  fb_saty/1 -> fb_pm_L2/1, fb_pm_R2/1
  fb_pm_L2/1 -> [fb_L_ankle_roll]
  lam_demux/2 -> fb_pm_R1/2, fb_pm_R2/2
  fb_pm_R1/1 -> [fb_R_ankle_pitch]
  fb_pm_R2/1 -> [fb_R_ankle_roll]
  swing/1 -> swing_demux/1
  swing_demux/1 -> sch_g_L/1, st_pm_L/2
  sch_g_L/1 -> sch_b_L/1
  sch_b_L/1 -> [sch_L]
  swing_demux/2 -> sch_g_R/1, st_pm_R/2
  sch_g_R/1 -> sch_b_R/1
  sch_b_R/1 -> [sch_R]
  st_gv/1 -> st_xi/2
  st_xi/1 -> st_k/1
  st_k/1 -> st_sat/1
  st_sat/1 -> st_pm_L/1, st_pm_R/1
  st_pm_L/1 -> [dq_L_hip_pitch], st_n_L/1
  st_n_L/1 -> [dq_L_ankle_pitch]
  st_pm_R/1 -> [dq_R_hip_pitch], st_n_R/1
  st_n_R/1 -> [dq_R_ankle_pitch]
  qref/1 -> qref_demux/1
  qref_demux/1 -> [qr_L_ankle_pitch]
  qref_demux/2 -> [qr_L_ankle_roll]
  qref_demux/3 -> [qr_L_clavicle]
  qref_demux/4 -> [qr_L_elbow]
  qref_demux/5 -> [qr_L_forearm_twist]
  qref_demux/6 -> [qr_L_hip_pitch]
  qref_demux/7 -> [qr_L_hip_roll]
  qref_demux/8 -> [qr_L_hip_yaw]
  qref_demux/9 -> [qr_L_index1]
  qref_demux/10 -> [qr_L_index2]
  qref_demux/11 -> [qr_L_index3]
  qref_demux/12 -> [qr_L_knee]
  qref_demux/13 -> [qr_L_little1]
  qref_demux/14 -> [qr_L_little2]
  qref_demux/15 -> [qr_L_little3]
  qref_demux/16 -> [qr_L_middle1]
  qref_demux/17 -> [qr_L_middle2]
  qref_demux/18 -> [qr_L_middle3]
  qref_demux/19 -> [qr_L_ring1]
  qref_demux/20 -> [qr_L_ring2]
  qref_demux/21 -> [qr_L_ring3]
  qref_demux/22 -> [qr_L_scapula]
  qref_demux/23 -> [qr_L_shoulder_pitch]
  qref_demux/24 -> [qr_L_shoulder_roll]
  qref_demux/25 -> [qr_L_shoulder_yaw]
  qref_demux/26 -> [qr_L_thumb1]
  qref_demux/27 -> [qr_L_thumb2]
  qref_demux/28 -> [qr_L_thumb3]
  qref_demux/29 -> [qr_L_toe]
  qref_demux/30 -> [qr_L_wrist_pitch]
  qref_demux/31 -> [qr_L_wrist_roll]
  qref_demux/32 -> [qr_L_wrist_yaw]
  qref_demux/33 -> [qr_R_ankle_pitch]
  qref_demux/34 -> [qr_R_ankle_roll]
  qref_demux/35 -> [qr_R_clavicle]
  qref_demux/36 -> [qr_R_elbow]
  qref_demux/37 -> [qr_R_forearm_twist]
  qref_demux/38 -> [qr_R_hip_pitch]
  qref_demux/39 -> [qr_R_hip_roll]
  qref_demux/40 -> [qr_R_hip_yaw]
  qref_demux/41 -> [qr_R_index1]
  qref_demux/42 -> [qr_R_index2]
  qref_demux/43 -> [qr_R_index3]
  qref_demux/44 -> [qr_R_knee]
  qref_demux/45 -> [qr_R_little1]
  qref_demux/46 -> [qr_R_little2]
  qref_demux/47 -> [qr_R_little3]
  qref_demux/48 -> [qr_R_middle1]
  qref_demux/49 -> [qr_R_middle2]
  qref_demux/50 -> [qr_R_middle3]
  qref_demux/51 -> [qr_R_ring1]
  qref_demux/52 -> [qr_R_ring2]
  qref_demux/53 -> [qr_R_ring3]
  qref_demux/54 -> [qr_R_scapula]
  qref_demux/55 -> [qr_R_shoulder_pitch]
  qref_demux/56 -> [qr_R_shoulder_roll]
  qref_demux/57 -> [qr_R_shoulder_yaw]
  qref_demux/58 -> [qr_R_thumb1]
  qref_demux/59 -> [qr_R_thumb2]
  qref_demux/60 -> [qr_R_thumb3]
  qref_demux/61 -> [qr_R_toe]
  qref_demux/62 -> [qr_R_wrist_pitch]
  qref_demux/63 -> [qr_R_wrist_roll]
  qref_demux/64 -> [qr_R_wrist_yaw]
  qref_demux/65 -> [qr_neck_pitch]
  qref_demux/66 -> [qr_neck_roll]
  qref_demux/67 -> [qr_neck_yaw]
  qref_demux/68 -> [qr_waist_pitch]
  qref_demux/69 -> [qr_waist_roll]
  qref_demux/70 -> [qr_waist_yaw]
  tauff/1 -> tauff_demux/1
  tauff_demux/1 -> [tf_L_ankle_pitch]
  tauff_demux/2 -> [tf_L_ankle_roll]
  tauff_demux/3 -> [tf_L_clavicle]
  tauff_demux/4 -> [tf_L_elbow]
  tauff_demux/5 -> [tf_L_forearm_twist]
  tauff_demux/6 -> [tf_L_hip_pitch]
  tauff_demux/7 -> [tf_L_hip_roll]
  tauff_demux/8 -> [tf_L_hip_yaw]
  tauff_demux/9 -> [tf_L_index1]
  tauff_demux/10 -> [tf_L_index2]
  tauff_demux/11 -> [tf_L_index3]
  tauff_demux/12 -> [tf_L_knee]
  tauff_demux/13 -> [tf_L_little1]
  tauff_demux/14 -> [tf_L_little2]
  tauff_demux/15 -> [tf_L_little3]
  tauff_demux/16 -> [tf_L_middle1]
  tauff_demux/17 -> [tf_L_middle2]
  tauff_demux/18 -> [tf_L_middle3]
  tauff_demux/19 -> [tf_L_ring1]
  tauff_demux/20 -> [tf_L_ring2]
  tauff_demux/21 -> [tf_L_ring3]
  tauff_demux/22 -> [tf_L_scapula]
  tauff_demux/23 -> [tf_L_shoulder_pitch]
  tauff_demux/24 -> [tf_L_shoulder_roll]
  tauff_demux/25 -> [tf_L_shoulder_yaw]
  tauff_demux/26 -> [tf_L_thumb1]
  tauff_demux/27 -> [tf_L_thumb2]
  tauff_demux/28 -> [tf_L_thumb3]
  tauff_demux/29 -> [tf_L_toe]
  tauff_demux/30 -> [tf_L_wrist_pitch]
  tauff_demux/31 -> [tf_L_wrist_roll]
  tauff_demux/32 -> [tf_L_wrist_yaw]
  tauff_demux/33 -> [tf_R_ankle_pitch]
  tauff_demux/34 -> [tf_R_ankle_roll]
  tauff_demux/35 -> [tf_R_clavicle]
  tauff_demux/36 -> [tf_R_elbow]
  tauff_demux/37 -> [tf_R_forearm_twist]
  tauff_demux/38 -> [tf_R_hip_pitch]
  tauff_demux/39 -> [tf_R_hip_roll]
  tauff_demux/40 -> [tf_R_hip_yaw]
  tauff_demux/41 -> [tf_R_index1]
  tauff_demux/42 -> [tf_R_index2]
  tauff_demux/43 -> [tf_R_index3]
  tauff_demux/44 -> [tf_R_knee]
  tauff_demux/45 -> [tf_R_little1]
  tauff_demux/46 -> [tf_R_little2]
  tauff_demux/47 -> [tf_R_little3]
  tauff_demux/48 -> [tf_R_middle1]
  tauff_demux/49 -> [tf_R_middle2]
  tauff_demux/50 -> [tf_R_middle3]
  tauff_demux/51 -> [tf_R_ring1]
  tauff_demux/52 -> [tf_R_ring2]
  tauff_demux/53 -> [tf_R_ring3]
  tauff_demux/54 -> [tf_R_scapula]
  tauff_demux/55 -> [tf_R_shoulder_pitch]
  tauff_demux/56 -> [tf_R_shoulder_roll]
  tauff_demux/57 -> [tf_R_shoulder_yaw]
  tauff_demux/58 -> [tf_R_thumb1]
  tauff_demux/59 -> [tf_R_thumb2]
  tauff_demux/60 -> [tf_R_thumb3]
  tauff_demux/61 -> [tf_R_toe]
  tauff_demux/62 -> [tf_R_wrist_pitch]
  tauff_demux/63 -> [tf_R_wrist_roll]
  tauff_demux/64 -> [tf_R_wrist_yaw]
  tauff_demux/65 -> [tf_neck_pitch]
  tauff_demux/66 -> [tf_neck_roll]
  tauff_demux/67 -> [tf_neck_yaw]
  tauff_demux/68 -> [tf_waist_pitch]
  tauff_demux/69 -> [tf_waist_roll]
  tauff_demux/70 -> [tf_waist_yaw]
  tau_mux/1 -> tau_log/1
  connections:
  L_ankle_pitch/RConn1 -- L_ankle_pitch1/LConn1
  L_ankle_pitch1/RConn1 -- L_ankle_roll/LConn1
  L_hip_pitch/RConn1 -- L_hip_pitch1/LConn1
  R_scapula/RConn1 -- R_scapula1/LConn1
  R_clavicle/LConn1 -- R_scapula1/RConn1
  R_shoulder_pitch/RConn1 -- R_shoulder_pitch1/LConn1
  R_shoulder_pitch1/RConn1 -- R_shoulder_roll/LConn1
  R_shoulder_roll/RConn1 -- R_shoulder_roll1/LConn1
  R_shoulder_roll1/RConn1 -- R_shoulder_yaw/LConn1
  R_shoulder_yaw/RConn1 -- R_shoulder_yaw1/LConn1
  R_elbow/LConn1 -- R_shoulder_yaw1/RConn1
  R_thumb1/RConn1 -- R_thumb4/LConn1
  R_thumb2/LConn1 -- R_thumb4/RConn1
  L_hip_pitch1/RConn1 -- L_hip_roll/LConn1
  R_thumb2/RConn1 -- R_thumb5/LConn1
  R_thumb3/LConn1 -- R_thumb5/RConn1
  R_thumb3/RConn1 -- R_thumb6/LConn1
  R_toe/RConn1 -- R_toe1/LConn1
  R_wrist_pitch/RConn1 -- R_wrist_pitch1/LConn1
  R_wrist_pitch1/RConn1 -- R_wrist_roll/LConn1
  R_wrist_roll/RConn1 -- R_wrist_roll1/LConn1
  R_wrist_roll1/RConn1 -- R_wrist_yaw/LConn1
  R_wrist_yaw/RConn1 -- R_wrist_yaw1/LConn1
  R_index1/LConn1 -- R_wrist_yaw1/RConn5
  L_hip_roll/RConn1 -- L_hip_roll1/LConn1
  R_little1/LConn1 -- R_wrist_yaw1/RConn4
  R_middle1/LConn1 -- R_wrist_yaw1/RConn3
  R_ring1/LConn1 -- R_wrist_yaw1/RConn2
  R_thumb1/LConn1 -- R_wrist_yaw1/RConn1
  head/LConn1 -- neck_pitch/RConn1
  neck_roll/RConn1 -- neck_roll1/LConn1
  neck_pitch/LConn1 -- neck_roll1/RConn1
  neck_yaw/RConn1 -- neck_yaw1/LConn1
  neck_roll/LConn1 -- neck_yaw1/RConn1
  L_hip_pitch/LConn1 -- pelvis/RConn3
  L_hip_roll1/RConn1 -- L_hip_yaw/LConn1
  R_hip_pitch/LConn1 -- pelvis/RConn2
  pelvis/RConn1 -- waist_yaw/LConn1
  torso/LConn1 -- waist_pitch/RConn1
  L_scapula/LConn1 -- torso/RConn3
  R_scapula/LConn1 -- torso/RConn2
  neck_yaw/LConn1 -- torso/RConn1
  waist_roll/RConn1 -- waist_roll1/LConn1
  waist_pitch/LConn1 -- waist_roll1/RConn1
  waist_yaw/RConn1 -- waist_yaw1/LConn1
  waist_roll/LConn1 -- waist_yaw1/RConn1
  L_hip_yaw/RConn1 -- L_hip_yaw1/LConn1
  L_hip_yaw1/RConn1 -- L_knee/LConn1
  L_index1/RConn1 -- L_index4/LConn1
  L_index2/LConn1 -- L_index4/RConn1
  L_index2/RConn1 -- L_index5/LConn1
  L_index3/LConn1 -- L_index5/RConn1
  L_ankle_roll/RConn1 -- ct_rot_L1/LConn1 -- ct_rot_L2/LConn1 -- ct_rot_L3/LConn1 -- L_ankle_roll1/LConn1 -- ct_rot_L4/LConn1
  L_index3/RConn1 -- L_index6/LConn1
  L_knee/RConn1 -- L_knee1/LConn1
  L_ankle_pitch/LConn1 -- L_knee1/RConn1
  L_little1/RConn1 -- L_little4/LConn1
  L_little2/LConn1 -- L_little4/RConn1
  L_little2/RConn1 -- L_little5/LConn1
  L_little3/LConn1 -- L_little5/RConn1
  L_little3/RConn1 -- L_little6/LConn1
  L_middle1/RConn1 -- L_middle4/LConn1
  L_middle2/LConn1 -- L_middle4/RConn1
  L_ankle_roll1/RConn1 -- L_toe/LConn1
  L_middle2/RConn1 -- L_middle5/LConn1
  L_middle3/LConn1 -- L_middle5/RConn1
  L_middle3/RConn1 -- L_middle6/LConn1
  L_ring1/RConn1 -- L_ring4/LConn1
  L_ring2/LConn1 -- L_ring4/RConn1
  L_ring2/RConn1 -- L_ring5/LConn1
  L_ring3/LConn1 -- L_ring5/RConn1
  L_ring3/RConn1 -- L_ring6/LConn1
  L_scapula/RConn1 -- L_scapula1/LConn1
  L_clavicle/LConn1 -- L_scapula1/RConn1
  L_clavicle/RConn1 -- L_clavicle1/LConn1
  L_shoulder_pitch/RConn1 -- L_shoulder_pitch1/LConn1
  L_shoulder_pitch1/RConn1 -- L_shoulder_roll/LConn1
  L_shoulder_roll/RConn1 -- L_shoulder_roll1/LConn1
  L_shoulder_roll1/RConn1 -- L_shoulder_yaw/LConn1
  L_shoulder_yaw/RConn1 -- L_shoulder_yaw1/LConn1
  L_elbow/LConn1 -- L_shoulder_yaw1/RConn1
  L_thumb1/RConn1 -- L_thumb4/LConn1
  L_thumb2/LConn1 -- L_thumb4/RConn1
  L_thumb2/RConn1 -- L_thumb5/LConn1
  L_thumb3/LConn1 -- L_thumb5/RConn1
  L_clavicle1/RConn1 -- L_shoulder_pitch/LConn1
  L_thumb3/RConn1 -- L_thumb6/LConn1
  L_toe/RConn1 -- L_toe1/LConn1
  L_wrist_pitch/RConn1 -- L_wrist_pitch1/LConn1
  L_wrist_pitch1/RConn1 -- L_wrist_roll/LConn1
  L_wrist_roll/RConn1 -- L_wrist_roll1/LConn1
  L_wrist_roll1/RConn1 -- L_wrist_yaw/LConn1
  L_wrist_yaw/RConn1 -- L_wrist_yaw1/LConn1
  L_index1/LConn1 -- L_wrist_yaw1/RConn5
